simulink model "finalmodel1"  (R2024b)
(part 3 of 9)

Industry ET-P672305WB | ET Solar Industry ET-P672305WBG | ET Solar Industry ET-P672305WW | ET Solar Industry ET-P672305WWG | ET Solar Industry ET-P672310WB | ET Solar Industry ET-P672310WW | ET Solar Industry ET-P672315WB | ET Solar Industry ET-P672315WW | ET Solar Industry ET-M672320WB | ET Solar Industry ET-M672320WW | ET Solar Industry ET-P672320WB | ET Solar Industry ET-P672320WW | ET Solar Industry ET-M672325WB | ET Solar Industry ET-M672325WW | ET Solar Industry ET-P672325WB | ET Solar Industry ET-P672325WW | ET Solar Industry ET-M672330WB | ET Solar Industry ET-M672330WW | ET Solar Industry ET-P672330WB | ET Solar Industry ET-P672330WW | ET Solar Industry ET-M672335WB | ET Solar Industry ET-M672335WW | ET Solar Industry ET-P672335WB | ET Solar Industry ET-P672335WW | ET Solar Industry ET-M672340WB | ET Solar Industry ET-M672340WW | ET Solar Industry ET-M672345WB | ET Solar Industry ET-M672345WW | ET Solar Industry ET-M672350WB | ET Solar Industry ET-M672350WW | ET Solar New Energy ET-M572165WW | ET Solar New Energy ET-M572165WWZ | ET Solar New Energy ET-M572170WW | ET Solar New Energy ET-M572170WWZ | ET Solar New Energy ET-M572175BB | ET Solar New Energy ET-M572175BBZ | ET Solar New Energy ET-M572175WW | ET Solar New Energy ET-M572175WWZ | ET Solar New Energy ET-M572180BB | ET Solar New Energy ET-M572180BBZ | ET Solar New Energy ET-M572180WW | ET Solar New Energy ET-M572180WWZ | ET Solar New Energy ET-M572185BB | ET Solar New Energy ET-M572185BBZ | ET Solar New Energy ET-M572185WW | ET Solar New Energy ET-M572185WWZ | ET Solar New Energy ET-M572190BBZ | ET Solar New Energy ET-M572190WB | ET Solar New Energy ET-M572190WW | ET Solar New Energy ET-M572190WWZ | ET Solar New Energy ET-P654190WB | ET Solar New Energy ET-P654190WW | ET Solar New Energy ET-P654195WB | ET Solar New Energy ET-P654195WW | ET Solar New Energy ET-P654200WB | ET Solar New Energy ET-P654200WW | ET Solar New Energy ET-P654205WB | ET Solar New Energy ET-P654205WW | ET Solar New Energy ET-P654210WB | ET Solar New Energy ET-P654210WW | ET Solar New Energy ET-P660220WB | ET Solar New Energy ET-P660220WBZ | ET Solar New Energy ET-P660220WW | ET Solar New Energy ET-P660220WWZ | ET Solar New Energy ET-A-P660225 | ET Solar New Energy ET-A-P660225B | ET Solar New Energy ET-P660225WB | ET Solar New Energy ET-P660225WBZ | ET Solar New Energy ET-P660225WW | ET Solar New Energy ET-P660225WWZ | ET Solar New Energy ET-A-P660230 | ET Solar New Energy ET-A-P660230B | ET Solar New Energy ET-P660230B | ET Solar New Energy ET-P660230WB | ET Solar New Energy ET-P660230WBZ | ET Solar New Energy ET-P660230WW | ET Solar New Energy ET-P660230WWZ | ET Solar New Energy ET-A-M660235 | ET Solar New Energy ET-A-M660235B | ET Solar New Energy ET-A-P660235 | ET Solar New Energy ET-A-P660235B | ET Solar New Energy ET-P660235B | ET Solar New Energy ET-P660235BB | ET Solar New Energy ET-P660235BBZ | ET Solar New Energy ET-P660235WB | ET Solar New Energy ET-P660235WBZ | ET Solar New Energy ET-P660235WW | ET Solar New Energy ET-P660235WWZ | ET Solar New Energy ET-A-M660240 | ET Solar New Energy ET-A-M660240B | ET Solar New Energy ET-A-P660240 | ET Solar New Energy ET-A-P660240B | ET Solar New Energy ET-M660240BB | ET Solar New Energy ET-M660240WW | ET Solar New Energy ET-P660240B | ET Solar New Energy ET-P660240BB | ET Solar New Energy ET-P660240BBZ | ET Solar New Energy ET-P660240WB | ET Solar New Energy ET-P660240WBZ | ET Solar New Energy ET-P660240WW | ET Solar New Energy ET-P660240WWZ | ET Solar New Energy ET-A-M660245 | ET Solar New Energy ET-A-M660245B | ET Solar New Energy ET-A-P660245 | ET Solar New Energy ET-A-P660245B | ET Solar New Energy ET-M660245BB | ET Solar New Energy ET-M660245WW | ET Solar New Energy ET-P660245B | ET Solar New Energy ET-P660245BAC | ET Solar New Energy ET-P660245BB | ET Solar New Energy ET-P660245BBAC | ET Solar New Energy ET-P660245BBZ | ET Solar New Energy ET-P660245BBZAC | ET Solar New Energy ET-P660245WB | ET Solar New Energy ET-P660245WBZ | ET Solar New Energy ET-P660245WBZAC | ET Solar New Energy ET-P660245WW | ET Solar New Energy ET-P660245WWZ | ET Solar New Energy ET-A-M660250 | ET Solar New Energy ET-A-M660250B | ET Solar New Energy ET-M660250BB | ET Solar New Energy ET-M660250WW | ET Solar New Energy ET-P660250BAC | ET Solar New Energy ET-P660250BB | ET Solar New Energy ET-P660250BBAC | ET Solar New Energy ET-P660250BBZ | ET Solar New Energy ET-P660250BBZAC | ET Solar New Energy ET-P660250WB | ET Solar New Energy ET-P660250WBAC | ET Solar New Energy ET-P660250WBZ | ET Solar New Energy ET-P660250WBZAC | ET Solar New Energy ET-P660250WW | ET Solar New Energy ET-P660250WWZ | ET Solar New Energy ET-P672250 | ET Solar New Energy ET-A-M660255 | ET Solar New Energy ET-A-M660255B | ET Solar New Energy ET-M660255BB | ET Solar New Energy ET-M660255WW | ET Solar New Energy ET-P660255BB | ET Solar New Energy ET-P660255BBAC | ET Solar New Energy ET-P660255BBZ | ET Solar New Energy ET-P660255BBZAC | ET Solar New Energy ET-P660255WB | ET Solar New Energy ET-P660255WBAC | ET Solar New Energy ET-P660255WBZ | ET Solar New Energy ET-P660255WBZAC | ET Solar New Energy ET-P660255WW | ET Solar New Energy ET-P660255WWAC | ET Solar New Energy ET-P660255WWZ | ET Solar New Energy ET-P660255WWZAC | ET Solar New Energy ET-P672255 | ET Solar New Energy ET-A-M660260 | ET Solar New Energy ET-A-M660260B | ET Solar New Energy ET-M660260BB | ET Solar New Energy ET-M660260WW | ET Solar New Energy ET-P660260WB | ET Solar New Energy ET-P660260WBAC | ET Solar New Energy ET-P660260WBZ | ET Solar New Energy ET-P660260WBZAC | ET Solar New Energy ET-P660260WW | ET Solar New Energy ET-P660260WWAC | ET Solar New Energy ET-P660260WWZ | ET Solar New Energy ET-P660260WWZAC | ET Solar New Energy ET-P672260WB | ET Solar New Energy ET-P672260WW | ET Solar New Energy ET-A-M660265 | ET Solar New Energy ET-A-M660265B | ET Solar New Energy ET-M660265BB | ET Solar New Energy ET-M660265WB | ET Solar New Energy ET-M660265WW | ET Solar New Energy ET-P660265WB | ET Solar New Energy ET-P660265WW | ET Solar New Energy ET-P672265WB | ET Solar New Energy ET-P672265WW | ET Solar New Energy ET-M660270BB | ET Solar New Energy ET-M660270WB | ET Solar New Energy ET-M660270WW | ET Solar New Energy ET-P660270WB | ET Solar New Energy ET-P660270WW | ET Solar New Energy ET-P672270WB | ET Solar New Energy ET-P672270WW | ET Solar New Energy ET-A-P672275 | ET Solar New Energy ET-A-P672275B | ET Solar New Energy ET-M660275BB | ET Solar New Energy ET-M660275WB | ET Solar New Energy ET-M660275WW | ET Solar New Energy ET-P660275WB | ET Solar New Energy ET-P660275WW | ET Solar New Energy ET-P672275WB | ET Solar New Energy ET-P672275WW | ET Solar New Energy ET-A-P672280 | ET Solar New Energy ET-A-P672280B | ET Solar New Energy ET-M660280BB | ET Solar New Energy ET-M660280WB | ET Solar New Energy ET-M660280WW | ET Solar New Energy ET-P660280WB | ET Solar New Energy ET-P660280WW | ET Solar New Energy ET-P672280WB | ET Solar New Energy ET-P672280WBG | ET Solar New Energy ET-P672280WW | ET Solar New Energy ET-P672280WWG | ET Solar New Energy ET-A-M672285 | ET Solar New Energy ET-A-M672285B | ET Solar New Energy ET-A-P672285 | ET Solar New Energy ET-A-P672285B | ET Solar New Energy ET-M660285BB | ET Solar New Energy ET-M660285WB | ET Solar New Energy ET-M660285WW | ET Solar New Energy ET-P672285WB | ET Solar New Energy ET-P672285WBG | ET Solar New Energy ET-P672285WW | ET Solar New Energy ET-P672285WWG | ET Solar New Energy ET-A-M672290 | ET Solar New Energy ET-A-M672290B | ET Solar New Energy ET-A-P672290 | ET Solar New Energy ET-A-P672290B | ET Solar New Energy ET-M660290WB | ET Solar New Energy ET-M660290WW | ET Solar New Energy ET-P672290WB | ET Solar New Energy ET-P672290WBG | ET Solar New Energy ET-P672290WW | ET Solar New Energy ET-P672290WWG | ET Solar New Energy ET-A-M672295 | ET Solar New Energy ET-A-M672295B | ET Solar New Energy ET-A-P672295 | ET Solar New Energy ET-A-P672295B | ET Solar New Energy ET-P672295WB | ET Solar New Energy ET-P672295WBG | ET Solar New Energy ET-P672295WW | ET Solar New Energy ET-P672295WWG | ET Solar New Energy ET-A-M672300 | ET Solar New Energy ET-A-M672300B | ET Solar New Energy ET-P672300WB | ET Solar New Energy ET-P672300WBG | ET Solar New Energy ET-P672300WW | ET Solar New Energy ET-P672300WWG | ET Solar New Energy ET-A-M672305 | ET Solar New Energy ET-A-M672305B | ET Solar New Energy ET-P672305WB | ET Solar New Energy ET-P672305WBG | ET Solar New Energy ET-P672305WW | ET Solar New Energy ET-P672305WWG | ET Solar New Energy ET-P672310WB | ET Solar New Energy ET-P672310WW | ET Solar New Energy ET-P672315WB | ET Solar New Energy ET-P672315WW | ET Solar New Energy ET-M672320WB | ET Solar New Energy ET-M672320WW | ET Solar New Energy ET-P672320WB | ET Solar New Energy ET-P672320WW | ET Solar New Energy ET-M672325WB | ET Solar New Energy ET-M672325WW | ET Solar New Energy ET-P672325WB | ET Solar New Energy ET-P672325WW | ET Solar New Energy ET-M672330WB | ET Solar New Energy ET-M672330WW | ET Solar New Energy ET-P672330WB | ET Solar New Energy ET-P672330WW | ET Solar New Energy ET-M672335WB | ET Solar New Energy ET-M672335WW | ET Solar New Energy ET-P672335WB | ET Solar New Energy ET-P672335WW | ET Solar New Energy ET-M672340WB | ET Solar New Energy ET-M672340WW | ET Solar New Energy ET-M672345WB | ET Solar New Energy ET-M672345WW | ET Solar New Energy ET-M672350WB | ET Solar New Energy ET-M672350WW | Eterbright Solar Corp. Cigs-3050E1 | Eterbright Solar Corp. Cigs-3100A1 | Eterbright Solar Corp. Cigs-3100E1 | Eterbright Solar Corp. Cigs-3150A1 | Eterbright Solar Corp. Cigs-3150E1 | Eterbright Solar Corp. Cigs-3200A1 | Eterbright Solar Corp. Cigs-3200E1 | Eterbright Solar Corp. Cigs-3250A1 | Exeltech AM24-1-B-6-0-00 | Exiom Solution EX-175M | Exiom Solution EX-175MB | Exiom Solution EX-180M | Exiom Solution EX-180MB | Exiom Solution EX-185M | Exiom Solution EX-185MB | Exiom Solution EX-185W | Exiom Solution EX-190M | Exiom Solution EX-195M | Exiom Solution EX-220P | Exiom Solution EX-220PB | Exiom Solution EX-225P | Exiom Solution EX-225PB | Exiom Solution EX-230P | Exiom Solution EX-230PB | Exiom Solution EX-230W | Exiom Solution EX-235P | Exiom Solution EX-235PB | Exiom Solution EX-235W | Exiom Solution EX-240P | Exiom Solution EX-240PB | Exiom Solution EX-240W | Exiom Solution EX-270P | Exiom Solution EX-270PB | Exiom Solution EX-275P | Exiom Solution EX-275PB | Exiom Solution EX-280P | Exiom Solution EX-280PB | Exiom Solution EX-285P | Exiom Solution EX-285PB | Exiom Solution EX-290P | Exiom Solution EX-290PB | Fire Energy FE5A-160M | Fire Energy FE6A-160P | Fire Energy FE6A-160PE | Fire Energy FE5A-170M | Fire Energy FE6A-170P | Fire Energy FE6P-170PE | Fire Energy FE5A-180M | Fire Energy FE6A-180P | Fire Energy FE6P-180PE | Fire Energy FE5A-190M | Fire Energy FE6P-190PE | Fire Energy FE6P-200PE | Fire Energy FE6P-210P | Fire Energy FE5P-220M | Fire Energy FE6P-220P | Fire Energy FE5P-230M | Fire Energy FE6P-230P | Fire Energy FE5P-240M | First Solar FS-267 | First Solar FS-367 | First Solar FS-270 | First Solar FS-370 | First Solar FS-272 | First Solar FS-372 | First Solar FS-275 | First Solar FS-375 | First Solar FS-377 | First Solar FS-277 | First Solar FS-280 | First Solar FS-380 | First Solar FS-382 | First Solar FS-385 | First Solar FS-387 | First Solar FS-387-Plus | First Solar FS-390 | First Solar FS-390-Plus | First Solar FS-490 | First Solar FS-490A | First Solar FS-392 | First Solar FS-392-Plus | First Solar FS-492 | First Solar Fs-492A | First Solar FS-395 | First Solar FS-395-Plus | First Solar FS-495 | First Solar FS-495A | First Solar FS-397-Plus | First Solar FS-497 | First Solar FS-497A | First Solar FS-3100-Plus | First Solar FS-4100 | First Solar FS-4100-2 | First Solar FS-4100A | First Solar FS-4100A-2 | First Solar FS-4102 | First Solar FS-4102-2 | First Solar FS-4102A | First Solar FS-4102A-2 | First Solar FS-4105 | First Solar FS-4105-2 | First Solar FS-4105-3 | First Solar FS-4105A | First Solar FS-4105A-2 | First Solar FS-4105A-3 | First Solar FS-4107-2 | First Solar FS-4107-3 | First Solar FS-4107A-2 | First Solar FS-4107A-3 | First Solar FS-4110-2 | First Solar FS-4110-3 | First Solar FS-4110A-2 | First Solar FS-4110A-3 | First Solar FS-4112-2 | First Solar FS-4112-3 | First Solar FS-4112A-2 | First Solar FS-4112A-3 | First Solar FS-4115-2 | First Solar FS-4115-3 | First Solar FS-4115A-2 | First Solar FS-4115A-3 | First Solar FS-4117-2 | First Solar FS-4117-3 | First Solar FS-4117A-2 | First Solar FS-4117A-3 | First Solar FS-4120-3 | First Solar FS-4120A-3 | First Solar FS-4122-3 | First Solar FS-4122A-3 | First Solar TS-295-R11-02 | First Solar TS-295-R12-02 | First Solar TS-295-R13-02 | First Solar TS-300-R11-02 | First Solar TS-300-R12-02 | First Solar TS-300-R13-02 | First Solar TS-305-R11-02 | First Solar TS-305-R12-02 | First Solar TS-305-R13-02 | First Solar TS-310-R11-02 | First Solar TS-310-R12-02 | First Solar TS-310-R13-02 | First Solar TS-315-R11-02 | First Solar TS-315-R12-02 | First Solar TS-315-R13-02 | First Solar TS-355-R11-02 | First Solar TS-355-R12-02 | First Solar TS-355-R13-02 | First Solar TS-360-R11-02 | First Solar TS-360-R12-02 | First Solar TS-360-R13-02 | First Solar TS-365-R11-02 | First Solar TS-365-R12-02 | First Solar TS-365-R13-02 | First Solar TS-370-R11-02 | First Solar TS-370-R12-02 | First Solar TS-370-R13-02 | First Solar TS-375-R11-02 | First Solar TS-375-R12-02 | First Solar TS-375-R13-02 | Flextronics FXS-260BB-MAA1B | Flextronics FXS-260BB-MAA1W | Flextronics FLV-MA-265M60AK | Flextronics FLV-MA-265M60AW | Flextronics FLV-MA-270M60AK | Flextronics FLV-MA-270M60AW | Flextronics FXS-270BB-SAC1B | Flextronics FLV-MA-275M60AK | Flextronics FLV-MA-275M60AW | Flextronics FXS-275BB-SAC1B | Flextronics FXS-285BB-SBC1B | Flextronics FXS-285BB-SBC1W | Flextronics FLV-MA-280M60AK | Flextronics FLV-MA-280M60AW | Flextronics FLV-MA-280P60AB | Flextronics FLV-MA-280P60AK | Flextronics FLV-MA-280P60AW | Flextronics FLV-MA-285M60AK | Flextronics FLV-MA-285M60AW | Flextronics FLV-MA-285P60AB | Flextronics FLV-MA-285P60AK | Flextronics FLV-MA-285P60AW | Flextronics FLV-MA-290P60AB | Flextronics FLV-MA-290P60AK | Flextronics FLV-MA-290P60AW | Flextronics FLV-MA-295P60AB | Flextronics FLV-MA-295P60AK | Flextronics FLV-MA-295P60AW | Flextronics FLV-MA-300P60AB | Flextronics FLV-MA-320M72AK | Flextronics FLV-MA-320M72AW | Flextronics FLV-MA-325M72AK | Flextronics FLV-MA-325M72AW | Flextronics FXS-325BB-MAB1W | Flextronics FXS-325BC-MAB1W | Flextronics FLV-MA-330M72AK | Flextronics FLV-MA-330M72AW | Flextronics FLV-MA-330P72AK | Flextronics FLV-MA-330P72AW | Flextronics FXS-330BB-SAD1W | Flextronics FLV-MA-335M72AK | Flextronics FLV-MA-335M72AW | Flextronics FLV-MA-335P72AK | Flextronics FLV-MA-335P72AW | Flextronics FXS-335BB-SAD1W | Flextronics FLV-MA-340M72AK | Flextronics FLV-MA-340M72AW | Flextronics FLV-MA-340P72AK | Flextronics FLV-MA-340P72AW | Flextronics FXS-350BB-SBD1W | Flextronics FXS-350BC-SBD1W | Flextronics FLV-MA-345P72AK | Flextronics FLV-MA-345P72AW | Fluitecnik FTS210P | Fluitecnik FTS215P | Fluitecnik FTS220P | Fluitecnik FTS225P | Fluitecnik FTS230M | Fluitecnik FTS230P | Fluitecnik FTS235M | Fluitecnik FTS240M | Fluitecnik FTS245M | Fluitecnik FTS250P | Fluitecnik FTS260P | Fluitecnik FTS270P | Fluitecnik FTS280P | Foxconn International FSM185-D4C0 | Foxconn International FSM190-D4C0 | Foxconn International FSM195-D4C0 | Foxconn International FSM205-D3C0 | Foxconn International FSM210-D3C0 | Foxconn International FSM215-D3C0 | Foxconn International FSM220-D3C0 | Foxconn International FSM225-D3C0 | Foxconn International FSM230-D2C0 | Foxconn International FSM235-D2C0 | Foxconn International FSM240-D2C0 | Foxconn International FSM245-D2C0 | Foxconn International FSM250-D2C0 | Foxconn International FSM275-D1E0 | Foxconn International FSM275-D1F0 | Foxconn International FSM280-D1E0 | Foxconn International FSM280-D1F0 | Foxconn International FSM285-D1E0 | Foxconn International FSM285-D1F0 | Foxconn International FSM290-D1E0 | Foxconn International FSM290-D1F0 | Foxconn International FSM295-D1E0 | Foxconn International FSM295-D1F0 | Freevolt SW Premium 275 | Freevolt SW Premium 285 | Freevolt SW Premium 300 | Future Solar Energy FSM572165 | Future Solar Energy FSM572170 | Future Solar Energy FSM572175 | Future Solar Energy FSM572180 | Future Solar Energy FSM572185 | Future Solar Energy FSP654195 | Future Solar Energy FSP654200 | Future Solar Energy FSP654205 | Future Solar Energy FSP654210 | Future Solar Energy FSP672260 | Future Solar Energy FSP672265 | Future Solar Energy FSP672270 | Future Solar Energy FSP672275 | Future Solar Energy FSP672280 | GAF RIAC 1000 | GCL System Integration Technology Co._ Ltd. GCL-P6-36-130 | GCL System Integration Technology Co._ Ltd. GCL-P6-36-135 | GCL System Integration Technology Co._ Ltd. GCL-P6-36-140 | GCL System Integration Technology Co._ Ltd. GCL-P6-42-150 | GCL System Integration Technology Co._ Ltd. GCL-P6-42-155 | GCL System Integration Technology Co._ Ltd. GCL-P6-42-160 | GCL System Integration Technology Co._ Ltd. GCL-P6-42-165 | GCL System Integration Technology Co._ Ltd. GCL-P6-48-170 | GCL System Integration Technology Co._ Ltd. GCL-P6-48-175 | GCL System Integration Technology Co._ Ltd. GCL-M5(L)-72-180 | GCL System Integration Technology Co._ Ltd. GCL-P6-48-180 | GCL System Integration Technology Co._ Ltd. GCL-M5(L)-72-185 | GCL System Integration Technology Co._ Ltd. GCL-P6-48-185 | GCL System Integration Technology Co._ Ltd. GCL-M5(L)-72-190 | GCL System Integration Technology Co._ Ltd. GCL-P6-48-190 | GCL System Integration Technology Co._ Ltd. GCL-M5(L)-72-195 | GCL System Integration Technology Co._ Ltd. GCL-M5(L)-72-200 | GCL System Integration Technology Co._ Ltd. GCL-M6-60-200 | GCL System Integration Technology Co._ Ltd. GCL-P6-54-200 | GCL System Integration Technology Co._ Ltd. GCL-M5(L)-72-205 | GCL System Integration Technology Co._ Ltd. GCL-M6-60-205 | GCL System Integration Technology Co._ Ltd. GCL-P6-54-205 | GCL System Integration Technology Co._ Ltd. GCL-M5(L)-72-210 | GCL System Integration Technology Co._ Ltd. GCL-M6-60-210 | GCL System Integration Technology Co._ Ltd. GCL-P6-54-210 | GCL System Integration Technology Co._ Ltd. GCL-M6-60-215 | GCL System Integration Technology Co._ Ltd. GCL-P6-54-215 | GCL System Integration Technology Co._ Ltd. GCL-P6-60-215 | GCL System Integration Technology Co._ Ltd. GCL-M6-60-220 | GCL System Integration Technology Co._ Ltd. GCL-P6-54-220 | GCL System Integration Technology Co._ Ltd. GCL-P6-60-220 | GCL System Integration Technology Co._ Ltd. GCL-M6-60-225 | GCL System Integration Technology Co._ Ltd. GCL-P6-60-225 | GCL System Integration Technology Co._ Ltd. GCL-M6-60-230 | GCL System Integration Technology Co._ Ltd. GCL-P6-60-230 | GCL System Integration Technology Co._ Ltd. GCL-M6-60-235 | GCL System Integration Technology Co._ Ltd. GCL-P6-60-235 | GCL System Integration Technology Co._ Ltd. GCL-M6-60-240 | GCL System Integration Technology Co._ Ltd. GCL-P6-60-240 | GCL System Integration Technology Co._ Ltd. GCL-P6-60-245 | GCL System Integration Technology Co._ Ltd. GCL-P6-60-250 | GCL System Integration Technology Co._ Ltd. GCL-P6-72-250 | GCL System Integration Technology Co._ Ltd. GCL-P6/60255 | GCL System Integration Technology Co._ Ltd. GCL-P6-72-255 | GCL System Integration Technology Co._ Ltd. GCL-P6/60260 | GCL System Integration Technology Co._ Ltd. GCL-P6-72-260 | GCL System Integration Technology Co._ Ltd. GCL-P6/60265 | GCL System Integration Technology Co._ Ltd. GCL-P6-72-265 | GCL System Integration Technology Co._ Ltd. GCL-P6/60270 | GCL System Integration Technology Co._ Ltd. GCL-P6-72-270 | GCL System Integration Technology Co._ Ltd. GCL-M6/60275 | GCL System Integration Technology Co._ Ltd. GCL-P6/60275 | GCL System Integration Technology Co._ Ltd. GCL-P6-72-275 | GCL System Integration Technology Co._ Ltd. GCL-M6/60280 | GCL System Integration Technology Co._ Ltd. GCL-P6/60280 | GCL System Integration Technology Co._ Ltd. GCL-P6-72-280 | GCL System Integration Technology Co._ Ltd. GCL-M6/60285 | GCL System Integration Technology Co._ Ltd. GCL-P6/60285 | GCL System Integration Technology Co._ Ltd. GCL-P6-72-285 | GCL System Integration Technology Co._ Ltd. GCL-M6/60290 | GCL System Integration Technology Co._ Ltd. GCL-P6/60290 | GCL System Integration Technology Co._ Ltd. GCL-P6-72-290 | GCL System Integration Technology Co._ Ltd. GCL-M6/60295 | GCL System Integration Technology Co._ Ltd. GCL-P6-72-295 | GCL System Integration Technology Co._ Ltd. GCL-M6/60300 | GCL System Integration Technology Co._ Ltd. GCL-P6/72300 | GCL System Integration Technology Co._ Ltd. GCL-M6/60305 | GCL System Integration Technology Co._ Ltd. GCL-P6/72305 | GCL System Integration Technology Co._ Ltd. GCL-M6/60310 | GCL System Integration Technology Co._ Ltd. GCL-P6/72310 | GCL System Integration Technology Co._ Ltd. GCL-M6/60315 | GCL System Integration Technology Co._ Ltd. GCL-P6/72315 | GCL System Integration Technology Co._ Ltd. GCL-M6/60320 | GCL System Integration Technology Co._ Ltd. GCL-P6/72320 | GCL System Integration Technology Co._ Ltd. GCL-M6/72325 | GCL System Integration Technology Co._ Ltd. GCL-P6/72325 | GCL System Integration Technology Co._ Ltd. GCL-M6/72330 | GCL System Integration Technology Co._ Ltd. GCL-M6/72H330 | GCL System Integration Technology Co._ Ltd. GCL-P6/72330 | GCL System Integration Technology Co._ Ltd. GCL-P6/72H330 | GCL System Integration Technology Co._ Ltd. GCL-M6/72335 | GCL System Integration Technology Co._ Ltd. GCL-M6/72H335 | GCL System Integration Technology Co._ Ltd. GCL-P6/72335 | GCL System Integration Technology Co._ Ltd. GCL-P6/72H335 | GCL System Integration Technology Co._ Ltd. GCL-M6/72340 | GCL System Integration Technology Co._ Ltd. GCL-M6/72H340 | GCL System Integration Technology Co._ Ltd. GCL-P6/72340 | GCL System Integration Technology Co._ Ltd. GCL-P6/72H340 | GCL System Integration Technology Co._ Ltd. GCL-M6/72345 | GCL System Integration Technology Co._ Ltd. GCL-M6/72H345 | GCL System Integration Technology Co._ Ltd. GCL-P6/72345 | GCL System Integration Technology Co._ Ltd. GCL-P6/72H345 | GCL System Integration Technology Co._ Ltd. GCL-M6/72350 | GCL System Integration Technology Co._ Ltd. GCL-M6/72H350 | GCL System Integration Technology Co._ Ltd. GCL-P6/72350 | GCL System Integration Technology Co._ Ltd. GCL-P6/72H350 | GCL System Integration Technology Co._ Ltd. GCL-M6/72355 | GCL System Integration Technology Co._ Ltd. GCL-M6/72H355 | GCL System Integration Technology Co._ Ltd. GCL-P6/72355 | GCL System Integration Technology Co._ Ltd. GCL-P6/72H355 | GCL System Integration Technology Co._ Ltd. GCL-M6/72H360 | GCL System Integration Technology Co._ Ltd. GCL-P6/72H360 | GE Energy GEPVp-066-G | GE Energy GE80-NA-B | GE Energy GE85-NA-B | GE Energy GE-CIGS130 | GE Energy GE-CIGS140 | GE Energy GE-CIGS145 | GE Energy GE-CIGS150 | GE Energy GE-CIGS155 | GE Energy GEPVp-200-M | GE Energy GEPVp-205-M | General Energy Solutions 7C00-6A225 | General Energy Solutions 7C00-6A230 | General Energy Solutions 7C00-6A235 | General Energy Solutions 7E00-6A235 | General Energy Solutions 7C00-6A240 | General Energy Solutions 7E00-6A240 | General Energy Solutions 7C00-6A245 | General Energy Solutions 7E00-6A245 | General Energy Solutions 7E00-6A250 | General Energy Solutions BVM6610P-250 | General Energy Solutions 7E00-6A255 | General Energy Solutions BVM6610P-255 | General Energy Solutions 7E00-6A260 | General Energy Solutions BVM6610M-260 | General Energy Solutions BVM6610P-260 | General Energy Solutions 7E00-6A265 | General Energy Solutions BVM6610M-265 | General Energy Solutions BVM6610P-265 | General Energy Solutions BVM6610M-270 | General Energy Solutions BVM6610P-270 | General Energy Solutions 7C00-6C275 | General Energy Solutions BVM6610M-275 | General Energy Solutions 7C00-6C280 | General Energy Solutions BVM6610M-280 | General Energy Solutions 7C00-6C285 | General Energy Solutions 7E00-6C285 | General Energy Solutions 7C00-6C290 | General Energy Solutions 7E00-6C290 | General Energy Solutions 7C00-6C295 | General Energy Solutions 7E00-6C295 | General Energy Solutions 7C00-6C300 | General Energy Solutions 7E00-6C300 | General Energy Solutions BVM6612P-300 | General Energy Solutions 7C00-6C305 | General Energy Solutions 7E00-6C305 | General Energy Solutions BVM6612P-305 | General Energy Solutions 7C00-6C310 | General Energy Solutions 7E00-6C310 | General Energy Solutions BVM6612M-310 | General Energy Solutions BVM6612P-310 | General Energy Solutions 7E00-6C315 | General Energy Solutions BVM6612M-315 | General Energy Solutions BVM6612P-315 | General Energy Solutions BVM6612M-320 | General Energy Solutions BVM6612P-320 | General Energy Solutions BVM6612M-325 | General Energy Solutions BVM6612P-325 | General Energy Solutions BVM6612M-330 | General Energy Solutions BVM6612M-335 | General Solar Power (Yantai) GSC90UR33Y | General Solar Power (Yantai) GSC93UR33Y | General Solar Power (Yantai) GSB94UR33 | General Solar Power (Yantai) GSB97UR33 | General Solar Power (Yantai) GSB100UR33 | GermanSolar USA GSP6-60-245W | GermanSolar USA GSP6-60-250W | GermanSolar USA GSP6-60-255W | GermanSolar USA GSM6-60-260W | GermanSolar USA GSP6-60-260W | GermanSolar USA GSM6-60-265W | GermanSolar USA GSP6-60-265W | GermanSolar USA GSM6-60-270W | GermanSolar USA GSP6-60-270W | GermanSolar USA GSM6-60-275W | GermanSolar USA GSM6-60-280W | GermanSolar USA GSM6-60-285W | GermanSolar USA GSM6-60-290W | GermanSolar USA GSM6-60-295W | GermanSolar USA GSM6-60-300W | GermanSolar USA GSP6-72-300W | GermanSolar USA GSP6-72-305W | GermanSolar USA GSM6-72-310W | GermanSolar USA GSP6-72-310W | GermanSolar USA GSM6-72-315W | GermanSolar USA GSP6-72-315W | GermanSolar USA GSM6-72-320W | GermanSolar USA GSP6-72-320W | GermanSolar USA GSM6-72-325W | GermanSolar USA GSP6-72-325W | GermanSolar USA GSM6-72-330W | GermanSolar USA GSM6-72-335W | GESOLAR GES-M165 | GESOLAR GES-M170 | GESOLAR GES-M175 | GESOLAR GES-M180 | GESOLAR GES-P200 | GESOLAR GES-P210 | GESOLAR GES-P220 | GESOLAR GES-P230 | GESOLAR GES-P250 | GESOLAR GES-P260 | GESOLAR GES-P270 | GESOLAR GES-P280 | Gigawatt GW250PB | Gigawatt GW255PB | Gigawatt GW260PB | Gigawatt GW265PB | Gigawatt GW270MB | Gigawatt GW270MB-M2 | Gigawatt GW270PB | Gigawatt GW275MB | Gigawatt GW275MB-M2 | Gigawatt GW-275MB-USA | Gigawatt GW275PB | Gigawatt GW280MB | Gigawatt GW280MB-M2 | Gigawatt GW-280MB-USA | Gigawatt GW280PB | Gigawatt GW285MB | Gigawatt GW285MB-M2 | Gigawatt GW-285MB-USA | Gigawatt GW290MB | Gigawatt GW290MB-M2 | Gigawatt GW-290MB-USA | Gigawatt GW295MB | Gigawatt GW295MB-M2 | Gigawatt GW-295MB-USA | Gigawatt GW-300MB-USA | Gintech Energy GIN P6-48-200 | Gintech Energy GTE 200M | Gintech Energy GIN P6-48-205 | Gintech Energy GTE 205M | Gintech Energy GIN M6-48-210 | Gintech Energy GIN P6-48-210 | Gintech Energy GTE 210M | Gintech Energy GIN M6-48-215 | Gintech Energy GIN P6-48-215 | Gintech Energy GTE 215M | Gintech Energy GIN M6-48-220 | Gintech Energy GIN P6-48-220 | Gintech Energy GTE 220M | Gintech Energy GIN M6-48-225 | Gintech Energy GTE 225M | Gintech Energy GIN M6-48-230 | Gintech Energy GTE 230M | Gintech Energy GTE 235M | Gintech Energy GTE 240M | Gintech Energy GIN P6-60-250 | Gintech Energy GIN P6-60-255 | Gintech Energy GIN P6-60-260 | Gintech Energy GIN M6-60-265 | Gintech Energy GIN P6-60-265 | Gintech Energy GIN M6-60-270 | Gintech Energy GIN P6-60-270 | Gintech Energy GIN M6-60-275 | Gintech Energy GIN M6-60-280 | Gintech Energy GIN M6-60-285 | Gintech Energy GIN P6-72-290 | Gintech Energy GIN P6-72-295 | Gintech Energy GIN P6-72-300 | Gintech Energy GIN M6-72-305 | Gintech Energy GIN P6-72-305 | Gintech Energy GIN P6F-72-305 | Gintech Energy GIN M6-72-310 | Gintech Energy GIN P6-72-310 | Gintech Energy GIN P6F-72-310 | Gintech Energy GIN M6-72-315 | Gintech Energy GIN P6-72-315 | Gintech Energy GIN P6F-72-315 | Gintech Energy GIN M6-72-320 | Gintech Energy GIN P6-72-320 | Gintech Energy GIN P6F-72-320 | Gintech Energy GIN M6-72-325 | Gintech Energy GIN P6F-72-325 | Gintech Energy GIN M6-72-330 | Gintech Energy GIN P6F-72-330 | Gintech Energy GIN M6-72-335 | Gintung Energy ASEC-120G6M | Gintung Energy ASEC-125G6M | Gintung Energy ASEC-125G6S | Gintung Energy ASEC-130G6M | Gintung Energy ASEC-130G6S | Gintung Energy ASEC-135G6M | Gintung Energy ASEC-135G6S | Gintung Energy ASEC-140G6M | Gintung Energy ASEC-140G6S | Gintung Energy ASEC-145G6M49 | Gintung Energy ASEC-145G6S49 | Gintung Energy ASEC-150G6M49 | Gintung Energy ASEC-150G6S49 | Gintung Energy ASEC-155G6M49 | Gintung Energy ASEC-155G6S49 | Gintung Energy ASEC-175G6M | Gintung Energy ASEC-175G6S | Gintung Energy ASEC-180G6M | Gintung Energy ASEC-180G6S | Gintung Energy ASEC-185G6M | Gintung Energy ASEC-185G6S | Gintung Energy ASEC-190G6M | Gintung Energy ASEC-190G6M68 | Gintung Energy ASEC-190G6S | Gintung Energy ASEC-190G6S68 | Gintung Energy GTEC-190G6M68 | Gintung Energy GTEC-190G6S68 | Gintung Energy ASEC-195G6M | Gintung Energy ASEC-195G6M68 | Gintung Energy ASEC-195G6S | Gintung Energy ASEC-195G6S68 | Gintung Energy GTEC-195G6M68 | Gintung Energy GTEC-195G6S68 | Gintung Energy ASEC-200G6M | Gintung Energy ASEC-200G6M68 | Gintung Energy ASEC-200G6S | Gintung Energy ASEC-200G6S68 | Gintung Energy GTEC-200G6M68 | Gintung Energy GTEC-200G6S68 | Gintung Energy ASEC-205G6M | Gintung Energy ASEC-205G6M68 | Gintung Energy ASEC-205G6S | Gintung Energy ASEC-205G6S68 | Gintung Energy GTEC-205G6M68 | Gintung Energy GTEC-205G6S68 | Gintung Energy ASEC-210G6M | Gintung Energy ASEC-210G6M68 | Gintung Energy ASEC-210G6S | Gintung Energy ASEC-210G6S68 | Gintung Energy GTEC-210G6M68 | Gintung Energy GTEC-210G6S68 | Gintung Energy ASEC-215G6M | Gintung Energy ASEC-215G6M68 | Gintung Energy ASEC-215G6M69 | Gintung Energy ASEC-215G6S | Gintung Energy ASEC-215G6S68 | Gintung Energy ASEC-215G6S69 | Gintung Energy GTEC-215G6M68 | Gintung Energy GTEC-215G6M69 | Gintung Energy GTEC-215G6S68 | Gintung Energy GTEC-215G6S69 | Gintung Energy ASEC-220G6M | Gintung Energy ASEC-220G6M68 | Gintung Energy ASEC-220G6M69 | Gintung Energy ASEC-220G6S | Gintung Energy ASEC-220G6S68 | Gintung Energy ASEC-220G6S69 | Gintung Energy GTEC-220G6M68 | Gintung Energy GTEC-220G6M69 | Gintung Energy GTEC-220G6S68 | Gintung Energy GTEC-220G6S69 | Gintung Energy ASEC-225G6M | Gintung Energy ASEC-225G6M69 | Gintung Energy ASEC-225G6S | Gintung Energy ASEC-225G6S69 | Gintung Energy GTEC-225G6M69 | Gintung Energy GTEC-225G6S69 | Gintung Energy ASEC-230G6M | Gintung Energy ASEC-230G6M69 | Gintung Energy ASEC-230G6S | Gintung Energy ASEC-230G6S69 | Gintung Energy GTEC-230G6M69 | Gintung Energy GTEC-230G6S69 | Gintung Energy ASEC-235G6M | Gintung Energy ASEC-235G6M69 | Gintung Energy ASEC-235G6S | Gintung Energy ASEC-235G6S69 | Gintung Energy GTEC-235G6M69 | Gintung Energy GTEC-235G6S69 | Gintung Energy ASEC-240G6M69 | Gintung Energy ASEC-240G6M6A | Gintung Energy ASEC-240G6S69 | Gintung Energy ASEC-240G6S6A | Gintung Energy GTEC-240G6M69 | Gintung Energy GTEC-240G6M6A | Gintung Energy GTEC-240G6S69 | Gintung Energy GTEC-240G6S6A | Gintung Energy ASEC-245G6M | Gintung Energy ASEC-245G6M69 | Gintung Energy ASEC-245G6M6A | Gintung Energy ASEC-245G6S69 | Gintung Energy ASEC-245G6S6A | Gintung Energy GTEC-245G6M69 | Gintung Energy GTEC-245G6M6A | Gintung Energy GTEC-245G6S69 | Gintung Energy GTEC-245G6S6A | Gintung Energy ASEC-250G6M | Gintung Energy ASEC-250G6M6A | Gintung Energy ASEC-250G6M6B | Gintung Energy ASEC-250G6S6A | Gintung Energy ASEC-250G6S6B | Gintung Energy GTEC-250G6M6A | Gintung Energy GTEC-250G6S6A | Gintung Energy ASEC-255G6M | Gintung Energy ASEC-255G6M6A | Gintung Energy ASEC-255G6M6B | Gintung Energy ASEC-255G6S | Gintung Energy ASEC-255G6S6A | Gintung Energy ASEC-255G6S6B | Gintung Energy GTEC-255G6M6A | Gintung Energy GTEC-255G6S6A | Gintung Energy ASEC-260G6M | Gintung Energy ASEC-260G6M6A | Gintung Energy ASEC-260G6M6B | Gintung Energy ASEC-260G6S | Gintung Energy ASEC-260G6S6A | Gintung Energy ASEC-260G6S6B | Gintung Energy GTEC-260G6M6A | Gintung Energy GTEC-260G6M6B | Gintung Energy GTEC-260G6S6A | Gintung Energy GTEC-260G6S6B | Gintung Energy ASEC-265G6M | Gintung Energy ASEC-265G6M6A | Gintung Energy ASEC-265G6M6B | Gintung Energy ASEC-265G6S | Gintung Energy ASEC-265G6S6A | Gintung Energy ASEC-265G6S6B | Gintung Energy GTEC-265G6M6A | Gintung Energy GTEC-265G6M6B | Gintung Energy GTEC-265G6S6A | Gintung Energy GTEC-265G6S6B | Gintung Energy ASEC-270G6M | Gintung Energy ASEC-270G6M6A | Gintung Energy ASEC-270G6M6B | Gintung Energy ASEC-270G6S | Gintung Energy ASEC-270G6S6A | Gintung Energy ASEC-270G6S6B | Gintung Energy GTEC-270G6M6A | Gintung Energy GTEC-270G6M6B | Gintung Energy GTEC-270G6S6A | Gintung Energy GTEC-270G6S6B | Gintung Energy ASEC-275G6M | Gintung Energy ASEC-275G6M6B | Gintung Energy ASEC-275G6S | Gintung Energy ASEC-275G6S6B | Gintung Energy GTEC-275G6M6B | Gintung Energy GTEC-275G6S6B | Gintung Energy ASEC-280G6M | Gintung Energy ASEC-280G6M6B | Gintung Energy ASEC-280G6S | Gintung Energy ASEC-280G6S6B | Gintung Energy GTEC-280G6M | Gintung Energy GTEC-280G6M6B | Gintung Energy GTEC-280G6S | Gintung Energy GTEC-280G6S6B | Gintung Energy ASEC-285G6M | Gintung Energy ASEC-285G6M6B | Gintung Energy ASEC-285G6S | Gintung Energy ASEC-285G6S6B | Gintung Energy GTEC-285G6M | Gintung Energy GTEC-285G6M6B | Gintung Energy GTEC-285G6S | Gintung Energy GTEC-285G6S6B | Gintung Energy ASEC-290G6M | Gintung Energy ASEC-290G6M6B | Gintung Energy ASEC-290G6S | Gintung Energy ASEC-290G6S6B | Gintung Energy GTEC-290G6M | Gintung Energy GTEC-290G6M6B | Gintung Energy GTEC-290G6S | Gintung Energy GTEC-290G6S6B | Gintung Energy ASEC-295G6M | Gintung Energy ASEC-295G6M6B | Gintung Energy ASEC-295G6S | Gintung Energy ASEC-295G6S6B | Gintung Energy GTEC-295G6M | Gintung Energy GTEC-295G6M6B | Gintung Energy GTEC-295G6S | Gintung Energy GTEC-295G6S6B | Gintung Energy ASEC-300G6M | Gintung Energy ASEC-300G6S | Gintung Energy GTEC-300G6M | Gintung Energy GTEC-300G6S | Gintung Energy ASEC-305G6M | Gintung Energy ASEC-305G6S | Gintung Energy GTEC-305G6M | Gintung Energy GTEC-305G6S | Gintung Energy ASEC-310G6M | Gintung Energy ASEC-310G6S | Gintung Energy GTEC-310G6M | Gintung Energy GTEC-310G6S | Gintung Energy ASEC-315G6M | Gintung Energy ASEC-315G6S | Gintung Energy GTEC-315G6M | Gintung Energy GTEC-315G6S | Gintung Energy ASEC-320G6M | Gintung Energy ASEC-320G6S | Gintung Energy GTEC-320G6M | Gintung Energy GTEC-320G6S | Gintung Energy ASEC-325G6M | Gintung Energy ASEC-325G6S | Gintung Energy GTEC-325G6M | Gintung Energy GTEC-325G6S | Global Solar Energy FG-2BTM-82 | Global Solar Energy FG-2BTN-82 | Global Solar Energy FG-2BTM-90 | Global Solar Energy FG-2BTN-90 | Global Solar Energy FG-2BTM-100 | Global Solar Energy FG-2BTN-100 | Global Solar Energy FG-4BTM-185 | Global Solar Energy FG-4BTN-185 | Global Solar Energy FG-1BTM-225 | Global Solar Energy FG-1BTN-225 | Global Solar Energy FG-1BTM-250 | Global Solar Energy FG-1BTN-250 | Global Solar Energy FG-1BTM-275 | Global Solar Energy FG-1BTN-275 | Global Solar Energy FG-1BTM-300 | Global Solar Energy FG-1BTN-300 | Global Sun P-220GS | Global Sun P-225GS | Global Sun P-230GS | Global Sun P-235GS | Global Sun P-240GS | Gloria Solar GSS5-160A-E1 | Gloria Solar GSS5-165A-E1 | Gloria Solar GSS5-170A-E1 | Gloria Solar GSS5-175A-E1 | Gloria Solar GSS5-180A-E1 | Gloria Solar GSM6-200D-E1 | Gloria Solar GSM6-205D-E1 | Gloria Solar GSM6-210D-E1 | Gloria Solar GSM6-215D-E1 | Gloria Solar GSM6-220D-E1 | Gloria Solar GSM6-225D-E1 | Gloria Solar GSM6-230D-E1 | Gloria Solar GSM6-235D-E1 | Gloria Solar GSM6-240D-E1 | Grape Solar GS-P-120-PDX | Grape Solar GS-P-125-PDX | Grape Solar GS-P-130-PDX | Grape Solar GS-P-135-PDX | Grape Solar GS-P-140-PDX | Grape Solar GS-S-150-SF | Grape Solar GS-S-155-SF | Grape Solar GS-P-160-EUG | Grape Solar GS-S-160-Fab8 | Grape Solar GS-S-160-SF | Grape Solar CS-S-165-DJ | Grape Solar GS-P-165-EUG | Grape Solar GS-S-165-Fab8 | Grape Solar GS-S-165-SF | Grape Solar CS-S-170-DJ | Grape Solar GS-P-170-EUG | Grape Solar GS-S-170-Fab3 | Grape Solar GS-S-170-SF | Grape Solar GS-S-175-Fab8 | Grape Solar CS-S-175-DJ | Grape Solar GS-P-175-EUG | Grape Solar GS-S-175-EUG | Grape Solar GS-S-175-Fab3 | Grape Solar GS-S-175-SF | Grape Solar CS-S-180-DJ | Grape Solar GS-P-180-EUG | Grape Solar GS-S-180-EUG | Grape Solar GS-S-180-Fab3 | Grape Solar GS-S-180-Fab8 | Grape Solar GS-S-180-SF | Grape Solar GS-S-185-Fab3 | Grape Solar GS-S-185-Fab8 | Grape Solar GS-S-185-SF | Grape Solar GS-P-190-EUG | Grape Solar GS-S-190-Fab3 | Grape Solar GS-P-190-SL6-18 | Grape Solar GS-P-195-EUG | Grape Solar GS-S-195-Fab3 | Grape Solar CS-P-200-DJ | Grape Solar GS-P-200-CSPE | Grape Solar GS-P-200-EUG | Grape Solar GS-P-200-Fab1 | Grape Solar GS-P-200-OR | Grape Solar GS-P-200-PDX | Grape Solar GS-P-200-SL6-18 | Grape Solar GS-S-200-Fab1 | Grape Solar GS-P-205-EUG | Grape Solar GS-P-205-Fab1 | Grape Solar GS-P-205-OR | Grape Solar GS-P-205-PDX | Grape Solar GS-P-205-SL6-18 | Grape Solar GS-S-205-Fab1 | Grape Solar CS-P-210-DJ | Grape Solar GS-P-210-Fab1 | Grape Solar GS-P-210-Fab5 | Grape Solar GS-P-210-OR | Grape Solar GS-P-210-PDX | Grape Solar GS-S-210-Fab1 | Grape Solar GS-P-215-Fab1 | Grape Solar GS-P-215-Fab5 | Grape Solar GS-P-215-OR | Grape Solar GS-P-215-PDX | Grape Solar GS-S-215-Fab1 | Grape Solar CS-P-220-DJ | Grape Solar GS-P-220-CS | Grape Solar GS-P-220-EUG | Grape Solar GS-P-220-Fab1 | Grape Solar GS-P-220-Fab5 | Grape Solar GS-P-220-OR | Grape Solar GS-P-220-PDX | Grape Solar GS-P-220-SL6-20 | Grape Solar GS-S-220-CS | Grape Solar GS-S-220-Fab1 | Grape Solar GS-S-220-Fab3 | Grape Solar GS-S-220-Fab8 | Grape Solar GS-P-225-EUG | Grape Solar GS-P-225-Fab1 | Grape Solar GS-P-225-Fab5 | Grape Solar GS-P-225-PDX | Grape Solar GS-P-225-SL6-20 | Grape Solar GS-S-225-Fab1 | Grape Solar GS-S-225-Fab3 | Grape Solar GS-S-225-Fab8 | Grape Solar CS-P-230-DJ | Grape Solar GS-P-230-CS | Grape Solar GS-P-230-EUG | Grape Solar GS-P-230-Fab1 | Grape Solar GS-P-230-Fab5 | Grape Solar GS-P-230-PDX | Grape Solar GS-P-230-SL6-20 | Grape Solar GS-S-230-CS | Grape Solar GS-S-230-Fab1 | Grape Solar GS-S-230-Fab3 | Grape Solar GS-S-230-Fab8 | Grape Solar GS-P-235-Fab1 | Grape Solar GS-P-235-Fab5 | Grape Solar GS-P-235-PDX | Grape Solar GS-S-235-Fab1 | Grape Solar GS-S-235-Fab3 | Grape Solar GS-S-235-Fab8 | Grape Solar GS-P-240-Fab1 | Grape Solar GS-P-240-KR2 | Grape Solar GS-P-240-KR2K | Grape Solar GS-P-240-PDX | Grape Solar GS-S-240-CS | Grape Solar GS-S-240-Fab1 | Grape Solar GS-S-240-Fab3 | Grape Solar GS-S-240-Fab8 | Grape Solar GS-P-245-Fab1 | Grape Solar GS-P-245-KR2 | Grape Solar GS-P-245-KR2K | Grape Solar GS-P-245-PDX | Grape Solar GS-S-245-Fab3 | Grape Solar GS-S-245-Fab8 | Grape Solar CS-P-250-DJ | Grape Solar GS-P-250-EUG | Grape Solar GS-P-250-Fab1 | Grape Solar GS-P-250-KR2 | Grape Solar GS-P-250-KR2K | Grape Solar GS-P-250-PDX | Grape Solar GS-S-250-Fab3 | Grape Solar GS-S-250-Fab5 | Grape Solar GS-S-250-Fab8 | Grape Solar GS-S-250-KR1 | Grape Solar GS-S-250-KR1K | Grape Solar GS-S-250-KR3 | Grape Solar GS-S-250-KR3K | Grape Solar GS-P-255-EUG | Grape Solar GS-P-255-Fab1 | Grape Solar GS-P-255-PDX | Grape Solar GS-P60-255-Fab2 | Grape Solar GS-S-255-Fab3 | Grape Solar GS-S-255-Fab5 | Grape Solar GS-S-255-KR1 | Grape Solar GS-S-255-KR1K | Grape Solar GS-S-255-KR3 | Grape Solar GS-S-255-KR3K | Grape Solar CS-P-260-DJ | Grape Solar GS-P-260-EUG | Grape Solar GS-P-260-Fab1 | Grape Solar GS-P-260-PDX | Grape Solar GS-P60-260-Fab2 | Grape Solar GS-P72-260-Fab2 | Grape Solar GS-S-260-Fab1 | Grape Solar GS-S-260-Fab5 | Grape Solar GS-S-260-KR1 | Grape Solar GS-S-260-KR1K | Grape Solar GS-S-260-KR3 | Grape Solar GS-S-260-KR3K | Grape Solar GS-S60-260-SI | Grape Solar GS-P-265-Fab1 | Grape Solar GS-P-265-PDX | Grape Solar GS-P60-265-Fab2 | Grape Solar GS-P72-265-Fab2 | Grape Solar GS-S-265-Fab1 | Grape Solar GS-S-265-Fab5 | Grape Solar GS-S60-265-SI | Grape Solar CS-P-270-DJ | Grape Solar GS-P-270-EUG | Grape Solar GS-P-270-Fab1 | Grape Solar GS-P-270-PDX | Grape Solar GS-P60-270-Fab2 | Grape Solar GS-P72-270-Fab2 | Grape Solar GS-S-270-Fab1 | Grape Solar GS-S-270-Fab5 | Grape Solar GS-S60-270-SI | Grape Solar GS-P-275-EUG | Grape Solar GS-P-275-Fab1 | Grape Solar GS-P-275-PDX | Grape Solar GS-P60-275-Fab2 | Grape Solar GS-P72-275-Fab2 | Grape Solar GS-S-275-Fab1 | Grape Solar GS-S-275-Fab5 | Grape Solar GS-S60-275-SI | Grape Solar CS-P-280-DJ | Grape Solar GS-P-280-EUG | Grape Solar GS-P-280-Fab1 | Grape Solar GS-P-280-PDX | Grape Solar GS-P72-280-Fab2 | Grape Solar GS-S-280-Fab1 | Grape Solar GS-S-280-Fab5 | Grape Solar GS-S60-280-SI | Grape Solar GS-M60-285-Fab1-USA | Grape Solar GS-P-285-Fab1 | Grape Solar GS-P-285-FAB36 | Grape Solar GS-P-285-PDX | Grape Solar GS-P72-285-Fab2 | Grape Solar GS-S-285-Fab1 | Grape Solar GS-S60LSQ-285-PR | Grape Solar GS-M60-290-Fab1-USA | Grape Solar GS-P-290-Fab1 | Grape Solar GS-P-290-FAB36 | Grape Solar GS-P72-290-Fab2 | Grape Solar GS-S-290-Fab1 | Grape Solar GS-S-290-FAB36 | Grape Solar GS-M60-295-Fab1-USA | Grape Solar GS-P-295-Fab1 | Grape Solar GS-P-295-FAB36 | Grape Solar GS-P72-295-Fab2 | Grape Solar GS-S-295-Fab1 | Grape Solar GS-S-295-FAB36 | Grape Solar GS-M60-300-Fab1-USA | Grape Solar GS-P-300-FAB36 | Grape Solar GS-P72-300-Fab2 | Grape Solar GS-S-300-FAB36 | Grape Solar GS-S-300-KR1 | Grape Solar GS-S-300-KR1K | Grape Solar GS-P72-305-Fab2 | Grape Solar GS-S-305-FAB36 | Grape Solar GS-S-305-KR1 | Grape Solar GS-S-305-KR1K | Grape Solar GS-S72-305-SI | Grape Solar GS-P72-310-Fab2 | Grape Solar GS-S-310-FAB36 | Grape Solar GS-S-310-KR1 | Grape Solar GS-S-310-KR1K | Grape Solar GS-S72-310-SI | Grape Solar GS-P72-315-Fab2 | Grape Solar GS-S72-315-SI | Grape Solar GS-P72-320-Fab2 | Grape Solar GS-S72-320-SI | Grape Solar GS-P72-325-Fab2 | Grape Solar GS-S72-325-SI | Grape Solar GS-P72-330-Fab2 | Grape Solar GS-S72-330-SI | Grape Solar GS-S72-335-SI | Grape Solar GS-M72-340-Fab1-USA | Grape Solar GS-M72-345-Fab1-USA | Grape Solar GS-M72-350-Fab1-USA | Grape Solar GS-M72-355-Fab1-USA | Grape Solar GS-M72-360-Fab1-USA | Grape Solar GS-P-375-KR2 | Grape Solar GS-P-380-KR2 | Grape Solar GS-P-385-KR2 | Grape Solar GS-S-385-TS | Grape Solar GS-P-390-KR2 | Grape Solar GS-S-390-TS | Grape Solar GS-P-395-KR2 | Grape Solar GS-S-395-Platinum | Grape Solar GS-S-400-Platinum | Grape Solar GS-S-405-KR1 | Grape Solar GS-S-405-KR3 | Grape Solar GS-S-405-Platinum | Grape Solar GS-S-410-KR1 | Grape Solar GS-S-410-KR3 | Grape Solar GS-S-410-Platinum | Grape Solar GS-S-415-KR1 | Grape Solar GS-S-415-KR3 | Grape Solar GS-S-420-KR1 | Grape Solar GS-S-420-KR3 | Green Energy Solar & Wind GESW1750 USA-170W | Green Energy Solar & Wind GESW1750 USA-175W | Green Energy Solar & Wind GESW1750 USA-180W | Green Energy Solar & Wind GESW2100 USA-210W | Green Energy Solar & Wind GESW2100 USA-215W | Green Energy Solar & Wind GESW2100 USA-220W | Green Energy Technology GET-085A | Green Energy Technology GET-090A | Green Energy Technology GET-095A-1 | Green Energy Technology GET-095-AT | Green Energy Technology GET-100A-1 | Green Energy Technology GET-100-AT | Green Energy Technology GET-105-AT | Green Energy Technology GET-170A | Green Energy Technology GET-170B | Green Energy Technology GET-180A | Green Energy Technology GET-180B | Green Energy Technology GET-340A | Green Energy Technology GET-360A | Green Power ET-M572165 | Green Power ET-M572170 | Green Power ET-M572175 | Green Power ET-M572175B | Green Power ET-M572180 | Green Power ET-M572180B | Green Power ET-M572185 | Green Power ET-M572185B | Green Power ET-P654190B | Green Power ET-P654195 | Green Power ET-P654195B | Green Power ET-P654200 | Green Power ET-P654200B | Green Power ET-P654205 | Green Power ET-P654205B | Green Power ET-P654210 | Green Power ET-P654210B | Green Power ET-P660220 | Green Power ET-P660220B | Green Power ET-P660225 | Green Power ET-P660225B | Green Power ET-P660230 | Green Power ET-P660230B | Green Power ET-P660235 | Green Power ET-P660235B | Green Power ET-P672260 | Green Power ET-P672260B | Green Power ET-P672265 | Green Power ET-P672265B | Green Power ET-P672270 | Green Power ET-P672270B | Green Power ET-P672275 | Green Power ET-P672275B | Green Power ET-P672280 | Green Power ET-P672280B | Greenbrilliance Energy GB54P6-200 | Greenbrilliance Energy GB60P6-210 | Greenbrilliance Energy GB60P6-215 | Greenbrilliance Energy GB60P6-220 | Greenbrilliance Energy GB60P6-225 | Greenbrilliance Energy GB60P6-230 | Greenbrilliance Energy GB72P6-270 | Greenbrilliance Energy GB72P6-275 | Greenbrilliance Energy GB72P6-280 | Greenlite Solar Canada GLS-200 | Greenlite Solar Canada GLS-220 | Greenlite Solar Canada GLS-270 | GS-Solar (Fujian) GS-46SU | GS-Solar (Fujian) GS-58 | GS-Solar (Fujian) GS-60 | GS-Solar (Fujian) GS-63 | Guangdong Fivestar Solar Energy FS-M125-175W | Guangdong Fivestar Solar Energy FS-P156-210W | Guangdong Fivestar Solar Energy FS-P156-220W | Guangdong Golden Glass Technologies GG160M2-24/1324x992 | Guangdong Golden Glass Technologies GG165M2-24/1324x992 | Guangdong Golden Glass Technologies GG170M2-24/1324x992 | Guangdong Golden Glass Technologies GG175M2-24/1324x992 | Guangdong Golden Glass Technologies GG175S1-36/1589x807 | Guangdong Golden Glass Technologies GG180M2-24/1324x992 | Guangdong Golden Glass Technologies GG180S1-36/1589x807 | Guangdong Golden Glass Technologies GG190M2-27/1482x992 | Guangdong Golden Glass Technologies GG195M2-27/1482x992 | Guangdong Golden Glass Technologies GG200M2-27/1482x992 | Guangdong Golden Glass Technologies GG205M2-27/1482x992 | Guangdong Golden Glass Technologies GG220M2-30/1640x992 | Guangdong Golden Glass Technologies GG225M2-30/1640x992 | Guangdong Golden Glass Technologies GG230M2-30/1640x992 | Guangdong Golden Glass Technologies GG250M2-35/1956x992 | Guangdong Golden Glass Technologies GG255M2-35/1956x992 | Guangdong Golden Glass Technologies GG260M2-35/1956x992 | Guangdong Golden Glass Technologies GG270M2-36/1956x992 | Guangdong Golden Glass Technologies GG275M2-36/1956x992 | Guangdong Golden Glass Technologies GG280M2-36/1956x992 | Guodian Jintech Solar Energy JT5M-175/E | Guodian Jintech Solar Energy JT5M-180/E | Guodian Jintech Solar Energy JT5M-185/E | Guodian Jintech Solar Energy JT6P-215/D | Guodian Jintech Solar Energy JT6P-220/D | Guodian Jintech Solar Energy JT6P-225/D | Guodian Jintech Solar Energy JT6P-230/D | Guodian Jintech Solar Energy JT6P-235/D | Guodian Jintech Solar Energy JT6P-255/E | Guodian Jintech Solar Energy JT6P-260/E | Guodian Jintech Solar Energy JT6P-265/E | Guodian Jintech Solar Energy JT6P-270/E | Guodian Jintech Solar Energy JT6P-275/E | Guodian Jintech Solar Energy JT6P-280/E | Hangzhou AmpleSun Solar Technology ASF100 | Hangzhou Zhejiang University Sunny Energy Science & Technology ZDNY-180C | Hangzhou Zhejiang University Sunny Energy Science & Technology ZDNY-185C | Hangzhou Zhejiang University Sunny Energy Science & Technology ZDNY-190C | Hangzhou Zhejiang University Sunny Energy Science & Technology ZDNY-200P54 | Hangzhou Zhejiang University Sunny Energy Science & Technology ZDNY-210C54 | Hangzhou Zhejiang University Sunny Energy Science & Technology ZDNY-210P54 | Hangzhou Zhejiang University Sunny Energy Science & Technology ZDNY-220C54 | Hangzhou Zhejiang University Sunny Energy Science & Technology ZDNY-220P54 | Hangzhou Zhejiang University Sunny Energy Science & Technology ZDNY-220P60 | Hangzhou Zhejiang University Sunny Energy Science & Technology ZDNY-230C54 | Hangzhou Zhejiang University Sunny Energy Science & Technology ZDNY-230C60 | Hangzhou Zhejiang University Sunny Energy Science & Technology ZDNY-230P60 | Hangzhou Zhejiang University Sunny Energy Science & Technology ZDNY-240C60 | Hangzhou Zhejiang University Sunny Energy Science & Technology ZDNY-240P60 | Hangzhou Zhejiang University Sunny Energy Science & Technology ZDNY-245P60 | Hangzhou Zhejiang University Sunny Energy Science & Technology ZDNY-250C60 | Hangzhou Zhejiang University Sunny Energy Science & Technology ZDNY-250P60 | Hangzhou Zhejiang University Sunny Energy Science & Technology ZDNY-255C60 | Hangzhou Zhejiang University Sunny Energy Science & Technology ZDNY-255P60 | Hangzhou Zhejiang University Sunny Energy Science & Technology ZDNY-260C60 | Hangzhou Zhejiang University Sunny Energy Science & Technology ZDNY-260P60 | Hangzhou Zhejiang University Sunny Energy Science & Technology ZDNY-265C60 | Hangzhou Zhejiang University Sunny Energy Science & Technology ZDNY-265P60 | Hangzhou Zhejiang University Sunny Energy Science & Technology ZDNY-270C60 | Hangzhou Zhejiang University Sunny Energy Science & Technology ZDNY-270P72 | Hangzhou Zhejiang University Sunny Energy Science & Technology ZDNY-275C60 | Hangzhou Zhejiang University Sunny Energy Science & Technology ZDNY-280C72 | Hangzhou Zhejiang University Sunny Energy Science & Technology ZDNY-280P72 | Hangzhou Zhejiang University Sunny Energy Science & Technology ZDNY-290C72 | Hangzhou Zhejiang University Sunny Energy Science & Technology ZDNY-290P72 | Hangzhou Zhejiang University Sunny Energy Science & Technology ZDNY-295P72 | Hangzhou Zhejiang University Sunny Energy Science & Technology ZDNY-300C72 | Hangzhou Zhejiang University Sunny Energy Science & Technology ZDNY-300P72 | Hangzhou Zhejiang University Sunny Energy Science & Technology ZDNY-305C72 | Hangzhou Zhejiang University Sunny Energy Science & Technology ZDNY-305P72 | Hangzhou Zhejiang University Sunny Energy Science & Technology ZDNY-310C72 | Hangzhou Zhejiang University Sunny Energy Science & Technology ZDNY-310P72 | Hangzhou Zhejiang University Sunny Energy Science & Technology ZDNY-315C72 | Hangzhou Zhejiang University Sunny Energy Science & Technology ZDNY-315P72 | Hangzhou Zhejiang University Sunny Energy Science & Technology ZDNY-320C72 | Hangzhou Zhejiang University Sunny Energy Science & Technology ZDNY-320P72 | Hangzhou Zhejiang University Sunny Energy Science & Technology ZDNY-325C72 | Hangzhou Zhejiang University Sunny Energy Science & Technology ZDNY-330C72 | Hangzhou Zhejiang University Sunny Energy Science & Technology ZDNY-335C72 | Hansol Technics Co._ Ltd HS238SB-A | Hansol Technics Co._ Ltd HS238SB-A06 | Hansol Technics Co._ Ltd HS240ME-V01 | Hansol Technics Co._ Ltd HS240SB-A | Hansol Technics Co._ Ltd HS240SB-A06 | Hansol Technics Co._ Ltd HS243SB-A | Hansol Technics Co._ Ltd HS243SB-A06 | Hansol Technics Co._ Ltd HS245ME-V01 | Hansol Technics Co._ Ltd HS245SB-A | Hansol Technics Co._ Ltd HS245SB-A06 | Hansol Technics Co._ Ltd HS248SB-A | Hansol Technics Co._ Ltd HS248SB-A06 | Hansol Technics Co._ Ltd HS250MB-AN3 | Hansol Technics Co._ Ltd HS250ME-V01 | Hansol Technics Co._ Ltd HS250NB-AN3 | Hansol Technics Co._ Ltd HS250SB-A | Hansol Technics Co._ Ltd HS250SB-A06 | Hansol Technics Co._ Ltd HS253SB-A | Hansol Technics Co._ Ltd HS253SB-A06 | Hansol Technics Co._ Ltd HS255MB-AN3 | Hansol Technics Co._ Ltd HS255ME-V01 | Hansol Technics Co._ Ltd HS255NB-AN3 | Hansol Technics Co._ Ltd HS255NB-AN4 | Hansol Technics Co._ Ltd HS255SB-A | Hansol Technics Co._ Ltd HS255SB-A06 | Hansol Technics Co._ Ltd HS255SE-V01 | Hansol Technics Co._ Ltd HS258SB-A | Hansol Technics Co._ Ltd HS258SB-A06 | Hansol Technics Co._ Ltd HS260MB-AN3 | Hansol Technics Co._ Ltd HS260ME-V01 | Hansol Technics Co._ Ltd HS260NB-AN3 | Hansol Technics Co._ Ltd HS260NB-AN4 | Hansol Technics Co._ Ltd HS260PB-AN1 | Hansol Technics Co._ Ltd HS260SB-A | Hansol Technics Co._ Ltd HS260SB-A06 | Hansol Technics Co._ Ltd HS260SE-V01 | Hansol Technics Co._ Ltd HS265MB-AN3 | Hansol Technics Co._ Ltd HS265ME-V01 | Hansol Technics Co._ Ltd HS265NB-AN3 | Hansol Technics Co._ Ltd HS265NB-AN4 | Hansol Technics Co._ Ltd HS265PB-AN1 | Hansol Technics Co._ Ltd HS265SE-V01 | Hansol Technics Co._ Ltd HS270MB-AN3 | Hansol Technics Co._ Ltd HS270ME-V01 | Hansol Technics Co._ Ltd HS270NB-AN3 | Hansol Technics Co._ Ltd HS270NB-AN4 | Hansol Technics Co._ Ltd HS270PB-AN1 | Hansol Technics Co._ Ltd HS270SE-V01 | Hansol Technics Co._ Ltd HS275NB-AN4 | Hansol Technics Co._ Ltd HS275PB-AN1 | Hansol Technics Co._ Ltd HS275SE-V01 | Hansol Technics Co._ Ltd HS275TB-AN3 | Hansol Technics Co._ Ltd HS280PB-AN1 | Hansol Technics Co._ Ltd HS280SE-V01 | Hansol Technics Co._ Ltd HS280TB-AN3 | Hansol Technics Co._ Ltd HS280TB-AN4 | Hansol Technics Co._ Ltd HS285TB-AN3 | Hansol Technics Co._ Ltd HS285TB-AN4 | Hansol Technics Co._ Ltd HS285UB-AN1 [Wht] | Hansol Technics Co._ Ltd HS290TB-AN3 | Hansol Technics Co._ Ltd HS290TB-AN4 | Hansol Technics Co._ Ltd HS290UB-AN1 [Blk] | Hansol Technics Co._ Ltd HS290UB-AN1 [Wht] | Hansol Technics Co._ Ltd HS295ME-V01 | Hansol Technics Co._ Ltd HS295TB-AN3 | Hansol Technics Co._ Ltd HS295TB-AN4 | Hansol Technics Co._ Ltd HS295UB-AN1 [Blk] | Hansol Technics Co._ Ltd HS295UB-AN1 [Wht] | Hansol Technics Co._ Ltd HS300MD-AN3 | Hansol Technics Co._ Ltd HS300ME-V01 | Hansol Technics Co._ Ltd HS300ND-AN3 | Hansol Technics Co._ Ltd HS300TB-AN3 | Hansol Technics Co._ Ltd HS300TB-AN4 | Hansol Technics Co._ Ltd HS300UB-AN1 [Blk] | Hansol Technics Co._ Ltd HS300UB-AN1 [Wht] | Hansol Technics Co._ Ltd HS305MD-AN3 | Hansol Technics Co._ Ltd HS305ME-V01 | Hansol Technics Co._ Ltd HS305ND-AN3 | Hansol Technics Co._ Ltd HS305ND-AN4 | Hansol Technics Co._ Ltd HS305SE-V01 | Hansol Technics Co._ Ltd HS305UB-AN1 [Blk] | Hansol Technics Co._ Ltd HS305UB-AN1 [Wht] | Hansol Technics Co._ Ltd HS310MD-AN3 | Hansol Technics Co._ Ltd HS310ME-V01 | Hansol Technics Co._ Ltd HS310ND-AN3 | Hansol Technics Co._ Ltd HS310ND-AN4 | Hansol Technics Co._ Ltd HS310SE-V01 | Hansol Technics Co._ Ltd HS310UB-AN1 [Blk] | Hansol Technics Co._ Ltd HS310UB-AN1 [Wht] | Hansol Technics Co._ Ltd HS315MD-AN3 | Hansol Technics Co._ Ltd HS315ME-V01 | Hansol Technics Co._ Ltd HS315ND-AN3 | Hansol Technics Co._ Ltd HS315ND-AN4 | Hansol Technics Co._ Ltd HS315PD-AN1 | Hansol Technics Co._ Ltd HS315SE-V01 | Hansol Technics Co._ Ltd HS315UB-AN1 [Blk] | Hansol Technics Co._ Ltd HS315UB-AN1 [Wht] | Hansol Technics Co._ Ltd HS320MD-AN3 | Hansol Technics Co._ Ltd HS320ME-V01 | Hansol Technics Co._ Ltd HS320ND-AN3 | Hansol Technics Co._ Ltd HS320ND-AN4 | Hansol Technics Co._ Ltd HS320PD-AN1 | Hansol Technics Co._ Ltd HS320SE-V01 | Hansol Technics Co._ Ltd HS320UB-AN1 [Blk] | Hansol Technics Co._ Ltd HS320UB-AN1 [Wht] | Hansol Technics Co._ Ltd HS325MD-AN3 | Hansol Technics Co._ Ltd HS325ME-V01 | Hansol Technics Co._ Ltd HS325ND-AN3 | Hansol Technics Co._ Ltd HS325ND-AN4 | Hansol Technics Co._ Ltd HS325PD-AN1 | Hansol Technics Co._ Ltd HS325SE-V01 | Hansol Technics Co._ Ltd HS325TD-AN3 | Hansol Technics Co._ Ltd HS330ND-AN4 | Hansol Technics Co._ Ltd HS330PD-AN1 | Hansol Technics Co._ Ltd HS330SE-V01 | Hansol Technics Co._ Ltd HS330TD-AN3 | Hansol Technics Co._ Ltd HS330TD-AN4 | Hansol Technics Co._ Ltd HS335ND-AN4 | Hansol Technics Co._ Ltd HS335PD-AN1 | Hansol Technics Co._ Ltd HS335SE-V01 | Hansol Technics Co._ Ltd HS335TD-AN3 | Hansol Technics Co._ Ltd HS335TD-AN4 | Hansol Technics Co._ Ltd HS340PD-AN1 | Hansol Technics Co._ Ltd HS340TD-AN3 | Hansol Technics Co._ Ltd HS340TD-AN4 | Hansol Technics Co._ Ltd HS340UD-AN1 [Wht] | Hansol Technics Co._ Ltd HS345PD-AN1 | Hansol Technics Co._ Ltd HS345TD-AN3 | Hansol Technics Co._ Ltd HS345TD-AN4 | Hansol Technics Co._ Ltd HS345UD-AN1 [Blk] | Hansol Technics Co._ Ltd HS345UD-AN1 [Wht] | Hansol Technics Co._ Ltd HS350TD-AN3 | Hansol Technics Co._ Ltd HS350TD-AN4 | Hansol Technics Co._ Ltd HS350UD-AN1 [Blk] | Hansol Technics Co._ Ltd HS350UD-AN1 [Wht] | Hansol Technics Co._ Ltd HS355TD-AN3 | Hansol Technics Co._ Ltd HS355TD-AN4 | Hansol Technics Co._ Ltd HS355UD-AN1 [Blk] | Hansol Technics Co._ Ltd HS355UD-AN1 [Wht] | Hansol Technics Co._ Ltd HS360TD-AN4 | Hansol Technics Co._ Ltd HS360UD-AN1 [Blk] | Hansol Technics Co._ Ltd HS360UD-AN1 [Wht] | Hansol Technics Co._ Ltd HS365UD-AN1 [Blk] | Hansol Technics Co._ Ltd HS365UD-AN1 [Wht] | Hansol Technics Co._ Ltd HS370UD-AN1 [Blk] | Hansol Technics Co._ Ltd HS370UD-AN1 [Wht] | Hansol Technics Co._ Ltd HS380UE-AN1 | Hansol Technics Co._ Ltd HS385UE-AN1 | Hansol Technics Co._ Ltd HS390UE-AN1 | Hansol Technics Co._ Ltd HS395UE-AN1 | Hansol Technics Co._ Ltd HS400UE-AN1 | Hansol Technics Co._ Ltd HS405UE-AN1 | Hansol Technics Co._ Ltd HS410UE-AN1 | Hansol Technics Co._ Ltd HS415UE-AN1 | Hansol Technics Co._ Ltd HS420UE-AN1 | Hanwha Q CELLS Q.PRO-G3 240 | Hanwha Q CELLS Q.PRO BFR - G3 245 | Hanwha Q CELLS Q.PRO-G3 245 | Hanwha Q CELLS Q.PRO BFR - G3 250 | Hanwha Q CELLS Q.PRO-G3 250 | Hanwha Q CELLS Q.PRO BFR - G3 255 | Hanwha Q CELLS Q.PRO BFR G4 255 | Hanwha Q CELLS Q.PRO BFR-G4.1 255 | Hanwha Q CELLS Q.PRO G4.1/SC 255 | Hanwha Q CELLS Q.PRO-G3 255 | Hanwha Q CELLS Q.PRO-G4 255 | Hanwha Q CELLS Q.PRO-G4/SC 255 | Hanwha Q CELLS Q.PRO BFR - G3 260 | Hanwha Q CELLS Q.PRO BFR G4 260 | Hanwha Q CELLS Q.PRO BFR-G4.1 260 | Hanwha Q CELLS Q.PRO BFR-G4.3 260 | Hanwha Q CELLS Q.PRO G4.1/SC 260 | Hanwha Q CELLS Q.PRO-G3 260 | Hanwha Q CELLS Q.PRO-G4 260 | Hanwha Q CELLS Q.PRO-G4/SC 260 | Hanwha Q CELLS Q.PEAK BLK-G3 265 | Hanwha Q CELLS Q.PEAK-G3 265 | Hanwha Q CELLS Q.PRO BFR - G3 265 | Hanwha Q CELLS Q.PRO BFR G4 265 | Hanwha Q CELLS Q.PRO BFR-G4.1 265 | Hanwha Q CELLS Q.PRO BFR-G4.3 265 | Hanwha Q CELLS Q.PRO G4.1/SC 265 | Hanwha Q CELLS Q.PRO-G3 265 | Hanwha Q CELLS Q.PRO-G4 265 | Hanwha Q CELLS Q.PRO-G4/SC 265 | Hanwha Q CELLS Q.PEAK BLK-G3 270 | Hanwha Q CELLS Q.PEAK-G3 270 | Hanwha Q CELLS Q.PLUS BFR G3.1 270 | Hanwha Q CELLS Q.PLUS BFR G4.1 270 | Hanwha Q CELLS Q.PLUS G4 270 | Hanwha Q CELLS Q.PLUS-G3 270 | Hanwha Q CELLS Q.PLUS-G4.1/SC 270 | Hanwha Q CELLS Q.PEAK BLK-G3 275 | Hanwha Q CELLS Q.PEAK-G3 275 | Hanwha Q CELLS Q.PLUS BFR G3.1 275 | Hanwha Q CELLS Q.PLUS BFR G4.1 275 | Hanwha Q CELLS Q.PLUS G4 275 | Hanwha Q CELLS Q.PLUS-G3 275 | Hanwha Q CELLS Q.PLUS-G4.1/SC 275 | Hanwha Q CELLS B.LINE PEAK BLK-G4.1 280 | Hanwha Q CELLS Q.PEAK-G3 280 | Hanwha Q CELLS Q.PLUS BFR G3.1 280 | Hanwha Q CELLS Q.PLUS BFR G4.1 280 | Hanwha Q CELLS Q.PLUS BFR-G4.1/TAA 280 | Hanwha Q CELLS Q.PLUS G4 280 | Hanwha Q CELLS Q.PLUS-G3 280 | Hanwha Q CELLS Q.PLUS-G4.1/SC 280 | Hanwha Q CELLS B.LINE PEAK BLK-G4.1 285 | Hanwha Q CELLS B.LINE PEAK BLK-G4.1/SC 285 | Hanwha Q CELLS Q.PEAK BLK-G4.1 285 | Hanwha Q CELLS Q.PEAK BLK-G4.1/SC 285 | Hanwha Q CELLS Q.PEAK BLK-G4.1/TAA 285 | Hanwha Q CELLS Q.PLUS BFR-G4.1/TAA 285 | Hanwha Q CELLS Q.PLUS-G4.1/SC 285 | Hanwha Q CELLS Q.PEAK BLK-G3.1 290 | Hanwha Q CELLS Q.PEAK BLK-G4.1 290 | Hanwha Q CELLS Q.PEAK BLK-G4.1/SC 290 | Hanwha Q CELLS Q.PEAK BLK-G4.1/TAA 290 | Hanwha Q Cells Q.PEAK-G4.1 290 | Hanwha Q CELLS Q.PLUS-BFR G4.1/TAA 290 | Hanwha Q CELLS Q.PRO L 290 | Hanwha Q CELLS Q.PEAK BLK-G3.1 295 | Hanwha Q CELLS Q.PEAK BLK-G4.1 295 | Hanwha Q CELLS Q.PEAK BLK-G4.1/SC 295 | Hanwha Q CELLS Q.PEAK BLK-G4.1/TAA 295 | Hanwha Q CELLS Q.PEAK G3.1 295 | Hanwha Q CELLS Q.PEAK G4.1/SC 295 | Hanwha Q Cells Q.PEAK-G4.1 295 | Hanwha Q CELLS Q.PRO L 295 | Hanwha Q CELLS Q.PEAK BLK-G4.1 300 | Hanwha Q CELLS Q.PEAK BLK-G4.1 300W | Hanwha Q CELLS Q.PEAK BLK-G4.1/TAA 300 | Hanwha Q CELLS Q.PEAK DUO BLK-G5 300 | Hanwha Q CELLS Q.PEAK G3.1 300 | Hanwha Q CELLS Q.PEAK G4.1/SC 300 | Hanwha Q CELLS Q.PEAK G4.1/TAA 300 | Hanwha Q Cells Q.PEAK-G4.1 300 | Hanwha Q CELLS Q.PRO L 300 | Hanwha Q CELLS Q.PRO L-G3 300 | Hanwha Q CELLS Q.Peak Duo-G5 305 | Hanwha Q CELLS Q.PEAK G3.1 305 | Hanwha Q CELLS Q.PEAK G4.1/SC 305 | Hanwha Q CELLS Q.PEAK G4.1/TAA 305 | Hanwha Q Cells Q.PEAK-G4.1 305 | Hanwha Q CELLS Q.PRO L 305 | Hanwha Q CELLS Q.PRO L-G2 305 | Hanwha Q CELLS Q.PRO L-G2.3 305 | Hanwha Q CELLS Q.PRO L-G3 305 | Hanwha Q CELLS B.LINE PRO L-G4.1 307 | Hanwha Q CELLS Q.PEAK DUO BLK-G5 310 | Hanwha Q CELLS Q.Peak Duo-G5 310 | Hanwha Q CELLS Q.PRO L 310 | Hanwha Q CELLS Q.PRO L G4 310 | Hanwha Q CELLS Q.PRO L G4.1 310 | Hanwha Q CELLS Q.PRO L-G2 310 | Hanwha Q CELLS Q.PRO L-G2.3 310 | Hanwha Q CELLS Q.PRO L-G3 310 | Hanwha Q CELLS Q.PRO L-G3.1 310 | Hanwha Q CELLS Q.PEAK DUO BLK-G5 315 | Hanwha Q CELLS Q.Peak Duo-G5 315 | Hanwha Q CELLS Q.PRO L G2 315 | Hanwha Q CELLS Q.PRO L G4 315 | Hanwha Q CELLS Q.PRO L G4.1 315 | Hanwha Q CELLS Q.PRO L-G2.3 315 | Hanwha Q CELLS Q.PRO L-G3 315 | Hanwha Q CELLS Q.PRO L-G3.1 315 | Hanwha Q CELLS B.LINE PLUS L-G4.2 317 | Hanwha Q CELLS Q.PEAK DUO BLK-G5 320 | Hanwha Q CELLS Q.Peak Duo-G5 320 | Hanwha Q CELLS Q.PLUS L-G4 320 | Hanwha Q CELLS Q.PLUS L-G4.1 320 | Hanwha Q CELLS Q.PLUS L-G4.2 320 | Hanwha Q CELLS Q.PRO L G4 320 | Hanwha Q CELLS Q.PRO L G4.1 320 | Hanwha Q CELLS Q.PRO L-G3.1 320 | Hanwha Q CELLS B.LINE PLUS L-G4.1 322 | Hanwha Q CELLS B.LINE PRO L-G4.1 322 | Hanwha Q CELLS B.LINE PLUS L-G4.2 325 | Hanwha Q CELLS Q.Peak Duo-G5 325 | Hanwha Q CELLS Q.PLUS L-G4 325 | Hanwha Q CELLS Q.PLUS L-G4.1 325 | Hanwha Q CELLS Q.PLUS L-G4.2 325 | Hanwha Q CELLS B.LINE PLUS L-G4.2 330 | Hanwha Q CELLS Q.PLUS L-G4 330 | Hanwha Q CELLS Q.PLUS L-G4.1 330 | Hanwha Q CELLS Q.PLUS L-G4.2 330 | Hanwha Q CELLS B.LINE PLUS L-G4.2 332 | Hanwha Q CELLS B.LINE PLUS L-G4.2 335 | Hanwha Q CELLS Q.PLUS L-G4 335 | Hanwha Q CELLS Q.PLUS L-G4.1 335 | Hanwha Q CELLS Q.PLUS L-G4.2 335 | Hanwha Q CELLS Q.PLUS L-G4.2/TAA 335 | Hanwha Q CELLS Q.PLUS L-G4.2 340W | Hanwha Q CELLS Q.PLUS L-G4.2/TAA 340 | Hanwha Q CELLS Q.PEAK L-G4.1 345 | Hanwha Q CELLS Q.PLUS L-G4.2 345W | Hanwha Q CELLS Q.PLUS L-G4.2/TAA 345 | Hanwha Q CELLS Q.PEAK L-G4.1 350 | Hanwha Q CELLS Q.PLUS L-G4.2/TAA 350 | Hanwha Q CELLS Q.PEAK L-G4.1 355 | Hanwha Q CELLS Q.PEAK L-G4.1 360 | Hanwha Q CELLS Q.PEAK L-G4.2 360W | Hanwha Q CELLS Q.PEAK L-G4.2 365 | Hanwha Q CELLS Q.PEAK L-G4.2 370 | Hanwha Q Cells Q.PEAK DUO L-G5.2 380 | Hanwha Q Cells Q.PEAK DUO L-G5.2 385 | Hanwha Q Cells Q.PEAK DUO L-G5.2 390 | Hanwha Q CELLS (Qidong) HSL60P6-PA-3-230Q | Hanwha Q CELLS (Qidong) HSL60P6-PA-3-230QB | Hanwha Q CELLS (Qidong) HSL60P6-PA-3-230QW | Hanwha Q CELLS (Qidong) HSL60P6-PB-3-230Q | Hanwha Q CELLS (Qidong) HSL60P6-PB-3-230QB | Hanwha Q CELLS (Qidong) HSL60P6-PB-3-230QW | Hanwha Q CELLS (Qidong) HSL60P6-PA-0-235T | Hanwha Q CELLS (Qidong) HSL60P6-PA-0-235TB | Hanwha Q CELLS (Qidong) HSL60P6-PA-0-235TW | Hanwha Q CELLS (Qidong) HSL60P6-PA-2-235Q | Hanwha Q CELLS (Qidong) HSL60P6-PA-2-235QB | Hanwha Q CELLS (Qidong) HSL60P6-PA-2-235QW | Hanwha Q CELLS (Qidong) HSL60P6-PA-3-235Q | Hanwha Q CELLS (Qidong) HSL60P6-PA-3-235QB | Hanwha Q CELLS (Qidong) HSL60P6-PA-3-235QW | Hanwha Q CELLS (Qidong) HSL60P6-PA-4-235Q | Hanwha Q CELLS (Qidong) HSL60P6-PA-4-235QB | Hanwha Q CELLS (Qidong) HSL60P6-PA-4-235QW | Hanwha Q CELLS (Qidong) HSL60P6-PA-4-235T | Hanwha Q CELLS (Qidong) HSL60P6-PA-4-235TB | Hanwha Q CELLS (Qidong) HSL60P6-PA-4-235TW | Hanwha Q CELLS (Qidong) HSL60P6-PB-2-235Q | Hanwha Q CELLS (Qidong) HSL60P6-PB-2-235QB | Hanwha Q CELLS (Qidong) HSL60P6-PB-2-235QW | Hanwha Q CELLS (Qidong) HSL60P6-PB-3-235Q | Hanwha Q CELLS (Qidong) HSL60P6-PB-3-235QB | Hanwha Q CELLS (Qidong) HSL60P6-PB-3-235QW | Hanwha Q CELLS (Qidong) HSL60P6-PB-4-235Q | Hanwha Q CELLS (Qidong) HSL60P6-PB-4-235QB | Hanwha Q CELLS (Qidong) HSL60P6-PB-4-235QW | Hanwha Q CELLS (Qidong) HSL60M6-HA-0-240T | Hanwha Q CELLS (Qidong) HSL60M6-HB-0-240T | Hanwha Q CELLS (Qidong) HSL60M6-HB-4-240T | Hanwha Q CELLS (Qidong) HSL60M6-HB-4-240TB | Hanwha Q CELLS (Qidong) HSL60M6-HB-4-240TW | Hanwha Q CELLS (Qidong) HSL60P6-PA-0-240T | Hanwha Q CELLS (Qidong) HSL60P6-PA-0-240TB | Hanwha Q CELLS (Qidong) HSL60P6-PA-0-240TW | Hanwha Q CELLS (Qidong) HSL60P6-PA-2-240Q | Hanwha Q CELLS (Qidong) HSL60P6-PA-2-240QB | Hanwha Q CELLS (Qidong) HSL60P6-PA-2-240QW | Hanwha Q CELLS (Qidong) HSL60P6-PA-3-240Q | Hanwha Q CELLS (Qidong) HSL60P6-PA-3-240QB | Hanwha Q CELLS (Qidong) HSL60P6-PA-3-240QW | Hanwha Q CELLS (Qidong) HSL60P6-PA-4-240Q | Hanwha Q CELLS (Qidong) HSL60P6-PA-4-240QB | Hanwha Q CELLS (Qidong) HSL60P6-PA-4-240QW | Hanwha Q CELLS (Qidong) HSL60P6-PA-4-240T | Hanwha Q CELLS (Qidong) HSL60P6-PA-4-240TB | Hanwha Q CELLS (Qidong) HSL60P6-PA-4-240TW | Hanwha Q CELLS (Qidong) HSL60P6-PB-0-240T | Hanwha Q CELLS (Qidong) HSL60P6-PB-0-240TB | Hanwha Q CELLS (Qidong) HSL60P6-PB-0-240TW | Hanwha Q CELLS (Qidong) HSL60P6-PB-2-240Q | Hanwha Q CELLS (Qidong) HSL60P6-PB-2-240QB | Hanwha Q CELLS (Qidong) HSL60P6-PB-2-240QW | Hanwha Q CELLS (Qidong) HSL60P6-PB-3-240QB | Hanwha Q CELLS (Qidong) HSL60P6-PB-4-240Q | Hanwha Q CELLS (Qidong) HSL60P6-PB-4-240QW | Hanwha Q CELLS (Qidong) HSL60P6-PB-4-240T | Hanwha Q CELLS (Qidong) HSL60P6-PB-4-240TB | Hanwha Q CELLS (Qidong) HSL60P6-PB-4-240TW | Hanwha Q CELLS (Qidong) HSL60M6-HB-0-245TW | Hanwha Q CELLS (Qidong) HSL60M6-HB-4-245T | Hanwha Q CELLS (Qidong) HSL60M6-HB-4-245TB | Hanwha Q CELLS (Qidong) HSL60M6-HB-4-245TW | Hanwha Q CELLS (Qidong) HSL60P6-PA-0-245T | Hanwha Q CELLS (Qidong) HSL60P6-PA-0-245TB | Hanwha Q CELLS (Qidong) HSL60P6-PA-0-245TW | Hanwha Q CELLS (Qidong) HSL60P6-PA-2-245Q | Hanwha Q CELLS (Qidong) HSL60P6-PA-2-245QB | Hanwha Q CELLS (Qidong) HSL60P6-PA-2-245QW | Hanwha Q CELLS (Qidong) HSL60P6-PA-3-245Q | Hanwha Q CELLS (Qidong) HSL60P6-PA-3-245QB | Hanwha Q CELLS (Qidong) HSL60P6-PA-3-245QW | Hanwha Q CELLS (Qidong) HSL60P6-PA-4-245Q | Hanwha Q CELLS (Qidong) HSL60P6-PA-4-245QB | Hanwha Q CELLS (Qidong) HSL60P6-PA-4-245QW | Hanwha Q CELLS (Qidong) HSL60P6-PA-4-245T | Hanwha Q CELLS (Qidong) HSL60P6-PA-4-245TB | Hanwha Q CELLS (Qidong) HSL60P6-PA-4-245TW | Hanwha Q CELLS (Qidong) HSL60P6-PB-0-245T | Hanwha Q CELLS (Qidong) HSL60P6-PB-0-245TB | Hanwha Q CELLS (Qidong) HSL60P6-PB-0-245TW | Hanwha Q CELLS (Qidong) HSL60P6-PB-2-245Q | Hanwha Q CELLS (Qidong) HSL60P6-PB-2-245QB | Hanwha Q CELLS (Qidong) HSL60P6-PB-2-245QW | Hanwha Q CELLS (Qidong) HSL60P6-PB-3-245Q | Hanwha Q CELLS (Qidong) HSL60P6-PB-3-245QB | Hanwha Q CELLS (Qidong) HSL60P6-PB-3-245QW | Hanwha Q CELLS (Qidong) HSL60P6-PB-4-245 | Hanwha Q CELLS (Qidong) HSL60P6-PB-4-245Q | Hanwha Q CELLS (Qidong) HSL60P6-PB-4-245QB | Hanwha Q CELLS (Qidong) HSL60P6-PB-4-245QW | Hanwha Q CELLS (Qidong) HSL60P6-PB-4-245T | Hanwha Q CELLS (Qidong) HSL60P6-PB-4-245TB | Hanwha Q CELLS (Qidong) HSL60P6-PB-4-245TW | Hanwha Q CELLS (Qidong) HSL60P6-PB-4-245W | Hanwha Q CELLS (Qidong) HSL60M6-HA-0-250T | Hanwha Q CELLS (Qidong) HSL60P6-PA-2-250QB | Hanwha Q CELLS (Qidong) HSL60P6-PA-2-250QW | Hanwha Q CELLS (Qidong) HSL60P6-PA-3-250Q | Hanwha Q CELLS (Qidong) HSL60P6-PA-3-250QB | Hanwha Q CELLS (Qidong) HSL60P6-PA-3-250QW | Hanwha Q CELLS (Qidong) HSL60P6-PA-4-250Q | Hanwha Q CELLS (Qidong) HSL60P6-PA-4-250QB | Hanwha Q CELLS (Qidong) HSL60P6-PA-4-250QW | Hanwha Q CELLS (Qidong) HSL60P6-PA-4-250T | Hanwha Q CELLS (Qidong) HSL60P6-PA-4-250TB | Hanwha Q CELLS (Qidong) HSL60P6-PA-4-250TW | Hanwha Q CELLS (Qidong) HSL60P6-PB-0-250T | Hanwha Q CELLS (Qidong) HSL60P6-PB-0-250TB | Hanwha Q CELLS (Qidong) HSL60P6-PB-0-250TW | Hanwha Q CELLS (Qidong) HSL60P6-PB-2-250Q | Hanwha Q CELLS (Qidong) HSL60P6-PB-2-250QB | Hanwha Q CELLS (Qidong) HSL60P6-PB-2-250QW | Hanwha Q CELLS (Qidong) HSL60P6-PB-3-250Q | Hanwha Q CELLS (Qidong) HSL60P6-PB-3-250QB | Hanwha Q CELLS (Qidong) HSL60P6-PB-3-250QW | Hanwha Q CELLS (Qidong) HSL60P6-PB-4-250 | Hanwha Q CELLS (Qidong) HSL60P6-PB-4-250Q | Hanwha Q CELLS (Qidong) HSL60P6-PB-4-250QB | Hanwha Q CELLS (Qidong) HSL60P6-PB-4-250QW | Hanwha Q CELLS (Qidong) HSL60P6-PB-4-250T | Hanwha Q CELLS (Qidong) HSL60P6-PB-4-250TB | Hanwha Q CELLS (Qidong) HSL60P6-PB-4-250TW | Hanwha Q CELLS (Qidong) HSL60P6-PB-4-250W | Hanwha Q CELLS (Qidong) HSL60P6-PC-3-250 | Hanwha Q CELLS (Qidong) HSL60P6-PC-3-250W | Hanwha Q CELLS (Qidong) HSL60M6-HA-4-255T | Hanwha Q CELLS (Qidong) HSL60M6-HA-4-255TB | Hanwha Q CELLS (Qidong) HSL60M6-HA-4-255TW | Hanwha Q CELLS (Qidong) HSL60M6-HB-4-255T | Hanwha Q CELLS (Qidong) HSL60M6-HB-4-255TB | Hanwha Q CELLS (Qidong) HSL60M6-HB-4-255TW | Hanwha Q CELLS (Qidong) HSL60P6-PA-0-255T | Hanwha Q CELLS (Qidong) HSL60P6-PA-0-255TB | Hanwha Q CELLS (Qidong) HSL60P6-PA-0-255TW | Hanwha Q CELLS (Qidong) HSL60P6-PA-2-255Q | Hanwha Q CELLS (Qidong) HSL60P6-PA-2-255QB | Hanwha Q CELLS (Qidong) HSL60P6-PA-2-255QW | Hanwha Q CELLS (Qidong) HSL60P6-PA-3-255Q | Hanwha Q CELLS (Qidong) HSL60P6-PA-3-255QB | Hanwha Q CELLS (Qidong) HSL60P6-PA-3-255QW | Hanwha Q CELLS (Qidong) HSL60P6-PA-4-255Q | Hanwha Q CELLS (Qidong) HSL60P6-PA-4-255QB | Hanwha Q CELLS (Qidong) HSL60P6-PA-4-255QW | Hanwha Q CELLS (Qidong) HSL60P6-PA-4-255T | Hanwha Q CELLS (Qidong) HSL60P6-PA-4-255TB | Hanwha Q CELLS (Qidong) HSL60P6-PA-4-255TW | Hanwha Q CELLS (Qidong) HSL60P6-PB-0-255T | Hanwha Q CELLS (Qidong) HSL60P6-PB-0-255TB | Hanwha Q CELLS (Qidong) HSL60P6-PB-0-255TW | Hanwha Q CELLS (Qidong) HSL60P6-PB-2-255Q | Hanwha Q CELLS (Qidong) HSL60P6-PB-2-255QB | Hanwha Q CELLS (Qidong) HSL60P6-PB-2-255QW | Hanwha Q CELLS (Qidong) HSL60P6-PB-3-255Q | Hanwha Q CELLS (Qidong) HSL60P6-PB-3-255QB | Hanwha Q CELLS (Qidong) HSL60P6-PB-3-255QW | Hanwha Q CELLS (Qidong) HSL60P6-PB-4-255 | Hanwha Q CELLS (Qidong) HSL60P6-PB-4-255Q | Hanwha Q CELLS (Qidong) HSL60P6-PB-4-255QB | Hanwha Q CELLS (Qidong) HSL60P6-PB-4-255QW | Hanwha Q CELLS (Qidong) HSL60P6-PB-4-255T | Hanwha Q CELLS (Qidong) HSL60P6-PB-4-255TB | Hanwha Q CELLS (Qidong) HSL60P6-PB-4-255TW | Hanwha Q CELLS (Qidong) HSL60P6-PB-4-255W | Hanwha Q CELLS (Qidong) HSL60P6-PC-3-255 | Hanwha Q CELLS (Qidong) HSL60P6-PC-3-255W | Hanwha Q CELLS (Qidong) HSL60M6-HA-4-260T | Hanwha Q CELLS (Qidong) HSL60M6-HA-4-260TB | Hanwha Q CELLS (Qidong) HSL60M6-HA-4-260TW | Hanwha Q CELLS (Qidong) HSL60M6-HB-0-260T | Hanwha Q CELLS (Qidong) HSL60M6-HB-4-260T | Hanwha Q CELLS (Qidong) HSL60M6-HB-4-260TB | Hanwha Q CELLS (Qidong) HSL60M6-HB-4-260TW | Hanwha Q CELLS (Qidong) HSL60P6-PB-0-260T | Hanwha Q CELLS (Qidong) HSL60P6-PB-0-260TW | Hanwha Q CELLS (Qidong) HSL60P6-PB-4-260 | Hanwha Q CELLS (Qidong) HSL60P6-PB-4-260T | Hanwha Q CELLS (Qidong) HSL60P6-PB-4-260TW | Hanwha Q CELLS (Qidong) HSL60P6-PB-4-260W | Hanwha Q CELLS (Qidong) HSL60P6-PC-3-260 | Hanwha Q CELLS (Qidong) HSL60P6-PC-3-260W | Hanwha Q CELLS (Qidong) HSL60P6-PB-0-265T | Hanwha Q CELLS (Qidong) HSL60P6-PB-0-265TW | Hanwha Q CELLS (Qidong) HSL60P6-PB-4-265T | Hanwha Q CELLS (Qidong) HSL60P6-PB-4-265TW | Hanwha Q CELLS (Qidong) HSL60P6-PC-3-265 | Hanwha Q CELLS (Qidong) HSL60P6-PC-3-265W | Hanwha Q CELLS (Qidong) HSL60P6-PB-0-270T | Hanwha Q CELLS (Qidong) HSL60P6-PB-0-270TW | Hanwha Q CELLS (Qidong) HSL60P6-PB-4-270T | Hanwha Q CELLS (Qidong) HSL60P6-PB-4-270TW | Hanwha Q CELLS (Qidong) HSL60P6-PC-3-270 | Hanwha Q CELLS (Qidong) HSL60P6-PC-3-275 | Hanwha Q CELLS (Qidong) HSL72P6-PA-0-275T | Hanwha Q CELLS (Qidong) HSL72P6-PA-0-275TB | Hanwha Q CELLS (Qidong) HSL72P6-PA-0-275TW | Hanwha Q CELLS (Qidong) HSL72P6-PA-4-275T | Hanwha Q CELLS (Qidong) HSL72P6-PA-4-275TB | Hanwha Q CELLS (Qidong) HSL72P6-PA-4-275TW | Hanwha Q CELLS (Qidong) HSL72P6-PA-0-280T | Hanwha Q CELLS (Qidong) HSL72P6-PA-0-280TB | Hanwha Q CELLS (Qidong) HSL72P6-PA-0-280TW | Hanwha Q CELLS (Qidong) HSL72P6-PA-2-280Q | Hanwha Q CELLS (Qidong) HSL72P6-PA-2-280QB | Hanwha Q CELLS (Qidong) HSL72P6-PA-2-280QW | Hanwha Q CELLS (Qidong) HSL72P6-PA-3-280Q | Hanwha Q CELLS (Qidong) HSL72P6-PA-3-280QB | Hanwha Q CELLS (Qidong) HSL72P6-PA-3-280QW | Hanwha Q CELLS (Qidong) HSL72P6-PA-4-280Q | Hanwha Q CELLS (Qidong) HSL72P6-PA-4-280QB | Hanwha Q CELLS (Qidong) HSL72P6-PA-4-280QW | Hanwha Q CELLS (Qidong) HSL72P6-PA-4-280T | Hanwha Q CELLS (Qidong) HSL72P6-PA-4-280TB | Hanwha Q CELLS (Qidong) HSL72P6-PA-4-280TW | Hanwha Q CELLS (Qidong) HSL72P6-PB-2-280Q | Hanwha Q CELLS (Qidong) HSL72P6-PB-2-280QB | Hanwha Q CELLS (Qidong) HSL72P6-PB-2-280QW | Hanwha Q CELLS (Qidong) HSL72P6-PB-3-280Q | Hanwha Q CELLS (Qidong) HSL72P6-PB-3-280QB | Hanwha Q CELLS (Qidong) HSL72P6-PB-3-280QW | Hanwha Q CELLS (Qidong) HSL72P6-PB-4-280Q | Hanwha Q CELLS (Qidong) HSL72P6-PB-4-280QB | Hanwha Q CELLS (Qidong) HSL72P6-PB-4-280QW | Hanwha Q CELLS (Qidong) HSL72M6-HA-0-285T | Hanwha Q CELLS (Qidong) HSL72M6-HA-0-285TB | Hanwha Q CELLS (Qidong) HSL72M6-HA-0-285TW | Hanwha Q CELLS (Qidong) HSL72M6-HA-4-285T | Hanwha Q CELLS (Qidong) HSL72M6-HA-4-285TB | Hanwha Q CELLS (Qidong) HSL72M6-HA-4-285TW | Hanwha Q CELLS (Qidong) HSL72M6-HB-0-285T | Hanwha Q CELLS (Qidong) HSL72M6-HB-0-285TB | Hanwha Q CELLS (Qidong) HSL72M6-HB-0-285TW | Hanwha Q CELLS (Qidong) HSL72M6-HB-4-285T | Hanwha Q CELLS (Qidong) HSL72M6-HB-4-285TB | Hanwha Q CELLS (Qidong) HSL72M6-HB-4-285TW | Hanwha Q CELLS (Qidong) HSL72P6-PA-0-285T | Hanwha Q CELLS (Qidong) HSL72P6-PA-0-285TB | Hanwha Q CELLS (Qidong) HSL72P6-PA-0-285TW | Hanwha Q CELLS (Qidong) HSL72P6-PA-2-285Q | Hanwha Q CELLS (Qidong) HSL72P6-PA-2-285QB | Hanwha Q CELLS (Qidong) HSL72P6-PA-2-285QW | Hanwha Q CELLS (Qidong) HSL72P6-PA-3-285Q | Hanwha Q CELLS (Qidong) HSL72P6-PA-3-285QB | Hanwha Q CELLS (Qidong) HSL72P6-PA-3-285QW | Hanwha Q CELLS (Qidong) HSL72P6-PA-4-285Q | Hanwha Q CELLS (Qidong) HSL72P6-PA-4-285QB | Hanwha Q CELLS (Qidong) HSL72P6-PA-4-285QW | Hanwha Q CELLS (Qidong) HSL72P6-PA-4-285T | Hanwha Q CELLS (Qidong) HSL72P6-PA-4-285TB | Hanwha Q CELLS (Qidong) HSL72P6-PA-4-285TW | Hanwha Q CELLS (Qidong) HSL72P6-PB-0-285T | Hanwha Q CELLS (Qidong) HSL72P6-PB-0-285TB | Hanwha Q CELLS (Qidong) HSL72P6-PB-0-285TW | Hanwha Q CELLS (Qidong) HSL72P6-PB-2-285Q | Hanwha Q CELLS (Qidong) HSL72P6-PB-2-285QB | Hanwha Q CELLS (Qidong) HSL72P6-PB-2-285QW | Hanwha Q CELLS (Qidong) HSL72P6-PB-3-285Q | Hanwha Q CELLS (Qidong) HSL72P6-PB-3-285QB | Hanwha Q CELLS (Qidong) HSL72P6-PB-3-285QW | Hanwha Q CELLS (Qidong) HSL72P6-PB-4-285Q | Hanwha Q CELLS (Qidong) HSL72P6-PB-4-285QB | Hanwha Q CELLS (Qidong) HSL72P6-PB-4-285QW | Hanwha Q CELLS (Qidong) HSL72P6-PB-4-285T | Hanwha Q CELLS (Qidong) HSL72P6-PB-4-285TB | Hanwha Q CELLS (Qidong) HSL72P6-PB-4-285TW | Hanwha Q CELLS (Qidong) HSL72M6-HA-0-290T | Hanwha Q CELLS (Qidong) HSL72M6-HA-0-290TB | Hanwha Q CELLS (Qidong) HSL72M6-HA-0-290TW | Hanwha Q CELLS (Qidong) HSL72M6-HA-4-290T | Hanwha Q CELLS (Qidong) HSL72M6-HA-4-290TB | Hanwha Q CELLS (Qidong) HSL72M6-HA-4-290TW | Hanwha Q CELLS (Qidong) HSL72M6-HB-0-290T | Hanwha Q CELLS (Qidong) HSL72M6-HB-0-290TB | Hanwha Q CELLS (Qidong) HSL72M6-HB-0-290TW | Hanwha Q CELLS (Qidong) HSL72M6-HB-4-290T | Hanwha Q CELLS (Qidong) HSL72M6-HB-4-290TB | Hanwha Q CELLS (Qidong) HSL72M6-HB-4-290TW | Hanwha Q CELLS (Qidong) HSL72P6-PA-0-290T | Hanwha Q CELLS (Qidong) HSL72P6-PA-0-290TB | Hanwha Q CELLS (Qidong) HSL72P6-PA-0-290TW | Hanwha Q CELLS (Qidong) HSL72P6-PA-2-290QB | Hanwha Q CELLS (Qidong) HSL72P6-PA-3-290Q | Hanwha Q CELLS (Qidong) HSL72P6-PA-3-290QW | Hanwha Q CELLS (Qidong) HSL72P6-PA-4-290Q | Hanwha Q CELLS (Qidong) HSL72P6-PA-4-290QB | Hanwha Q CELLS (Qidong) HSL72P6-PA-4-290QW | Hanwha Q CELLS (Qidong) HSL72P6-PA-4-290T | Hanwha Q CELLS (Qidong) HSL72P6-PA-4-290TB | Hanwha Q CELLS (Qidong) HSL72P6-PA-4-290TW | Hanwha Q CELLS (Qidong) HSL72P6-PB-0-290T | Hanwha Q CELLS (Qidong) HSL72P6-PB-0-290TB | Hanwha Q CELLS (Qidong) HSL72P6-PB-0-290TW | Hanwha Q CELLS (Qidong) HSL72P6-PB-2-290Q | Hanwha Q CELLS (Qidong) HSL72P6-PB-2-290QB | Hanwha Q CELLS (Qidong) HSL72P6-PB-2-290QW | Hanwha Q CELLS (Qidong) HSL72P6-PB-3-290Q | Hanwha Q CELLS (Qidong) HSL72P6-PB-3-290QB | Hanwha Q CELLS (Qidong) HSL72P6-PB-3-290QW | Hanwha Q CELLS (Qidong) HSL72P6-PB-4-290Q | Hanwha Q CELLS (Qidong) HSL72P6-PB-4-290QB | Hanwha Q CELLS (Qidong) HSL72P6-PB-4-290QW | Hanwha Q CELLS (Qidong) HSL72P6-PB-4-290T | Hanwha Q CELLS (Qidong) HSL72P6-PB-4-290TB | Hanwha Q CELLS (Qidong) HSL72P6-PB-4-290TW | Hanwha Q CELLS (Qidong) HSL72P6-PC-3-290 | Hanwha Q CELLS (Qidong) HSL72P6-PC-3-290W | Hanwha Q CELLS (Qidong) HSL72M6-HA-0-295T | Hanwha Q CELLS (Qidong) HSL72M6-HA-0-295TB | Hanwha Q CELLS (Qidong) HSL72M6-HA-0-295TW | Hanwha Q CELLS (Qidong) HSL72M6-HA-4-295T | Hanwha Q CELLS (Qidong) HSL72M6-HA-4-295TB | Hanwha Q CELLS (Qidong) HSL72M6-HA-4-295TW | Hanwha Q CELLS (Qidong) HSL72M6-HB-0-295T | Hanwha Q CELLS (Qidong) HSL72M6-HB-0-295TB | Hanwha Q CELLS (Qidong) HSL72M6-HB-0-295TW | Hanwha Q CELLS (Qidong) HSL72M6-HB-4-295T | Hanwha Q CELLS (Qidong) HSL72M6-HB-4-295TB | Hanwha Q CELLS (Qidong) HSL72M6-HB-4-295TW | Hanwha Q CELLS (Qidong) HSL72P6-PA-0-295T | Hanwha Q CELLS (Qidong) HSL72P6-PA-0-295TB | Hanwha Q CELLS (Qidong) HSL72P6-PA-0-295TW | Hanwha Q CELLS (Qidong) HSL72P6-PA-2-295Q | Hanwha Q CELLS (Qidong) HSL72P6-PA-2-295QB | Hanwha Q CELLS (Qidong) HSL72P6-PA-2-295QW | Hanwha Q CELLS (Qidong) HSL72P6-PA-3-295Q | Hanwha Q CELLS (Qidong) HSL72P6-PA-3-295QB | Hanwha Q CELLS (Qidong) HSL72P6-PA-3-295QW | Hanwha Q CELLS (Qidong) HSL72P6-PA-4-295Q | Hanwha Q CELLS (Qidong) HSL72P6-PA-4-295QB | Hanwha Q CELLS (Qidong) HSL72P6-PA-4-295QW | Hanwha Q CELLS (Qidong) HSL72P6-PA-4-295T | Hanwha Q CELLS (Qidong) HSL72P6-PA-4-295TB | Hanwha Q CELLS (Qidong) HSL72P6-PA-4-295TW | Hanwha Q CELLS (Qidong) HSL72P6-PB-0-295T | Hanwha Q CELLS (Qidong) HSL72P6-PB-0-295TB | Hanwha Q CELLS (Qidong) HSL72P6-PB-0-295TW | Hanwha Q CELLS (Qidong) HSL72P6-PB-2-295Q | Hanwha Q CELLS (Qidong) HSL72P6-PB-2-295QB | Hanwha Q CELLS (Qidong) HSL72P6-PB-2-295QW | Hanwha Q CELLS (Qidong) HSL72P6-PB-3-295Q | Hanwha Q CELLS (Qidong) HSL72P6-PB-3-295QB | Hanwha Q CELLS (Qidong) HSL72P6-PB-3-295QW | Hanwha Q CELLS (Qidong) HSL72P6-PB-4-295 | Hanwha Q CELLS (Qidong) HSL72P6-PB-4-295Q | Hanwha Q CELLS (Qidong) HSL72P6-PB-4-295QB | Hanwha Q CELLS (Qidong) HSL72P6-PB-4-295QW | Hanwha Q CELLS (Qidong) HSL72P6-PB-4-295T | Hanwha Q CELLS (Qidong) HSL72P6-PB-4-295TB | Hanwha Q CELLS (Qidong) HSL72P6-PB-4-295TW | Hanwha Q CELLS (Qidong) HSL72P6-PB-4-295W | Hanwha Q CELLS (Qidong) HSL72P6-PC-3-295 | Hanwha Q CELLS (Qidong) HSL72P6-PC-3-295Q | Hanwha Q CELLS (Qidong) HSL72P6-PC-3-295QW | Hanwha Q CELLS (Qidong) HSL72P6-PC-3-295W | Hanwha Q CELLS (Qidong) HSL72M6-HA-0-300T | Hanwha Q CELLS (Qidong) HSL72M6-HA-0-300TB | Hanwha Q CELLS (Qidong) HSL72M6-HA-0-300TW | Hanwha Q CELLS (Qidong) HSL72M6-HA-4-300T | Hanwha Q CELLS (Qidong) HSL72M6-HA-4-300TB | Hanwha Q CELLS (Qidong) HSL72M6-HA-4-300TW | Hanwha Q CELLS (Qidong) HSL72M6-HB-0-300T | Hanwha Q CELLS (Qidong) HSL72M6-HB-0-300TB | Hanwha Q CELLS (Qidong) HSL72M6-HB-0-300TW | Hanwha Q CELLS (Qidong) HSL72M6-HB-4-300T | Hanwha Q CELLS (Qidong) HSL72M6-HB-4-300TB | Hanwha Q CELLS (Qidong) HSL72M6-HB-4-300TW | Hanwha Q CELLS (Qidong) HSL72P6-PA-0-300T | Hanwha Q CELLS (Qidong) HSL72P6-PA-0-300TW | Hanwha Q CELLS (Qidong) HSL72P6-PA-2-300Q | Hanwha Q CELLS (Qidong) HSL72P6-PA-2-300QB | Hanwha Q CELLS (Qidong) HSL72P6-PA-2-300QW | Hanwha Q CELLS (Qidong) HSL72P6-PA-3-300Q | Hanwha Q CELLS (Qidong) HSL72P6-PA-3-300QB | Hanwha Q CELLS (Qidong) HSL72P6-PA-3-300QW | Hanwha Q CELLS (Qidong) HSL72P6-PA-4-300Q | Hanwha Q CELLS (Qidong) HSL72P6-PA-4-300QB | Hanwha Q CELLS (Qidong) HSL72P6-PA-4-300QW | Hanwha Q CELLS (Qidong) HSL72P6-PA-4-300T | Hanwha Q CELLS (Qidong) HSL72P6-PA-4-300TW | Hanwha Q CELLS (Qidong) HSL72P6-PB-0-300T | Hanwha Q CELLS (Qidong) HSL72P6-PB-0-300TW | Hanwha Q CELLS (Qidong) HSL72P6-PB-2-300Q | Hanwha Q CELLS (Qidong) HSL72P6-PB-2-300QB | Hanwha Q CELLS (Qidong) HSL72P6-PB-2-300QW | Hanwha Q CELLS (Qidong) HSL72P6-PB-3-300Q | Hanwha Q CELLS (Qidong) HSL72P6-PB-3-300QB | Hanwha Q CELLS (Qidong) HSL72P6-PB-3-300QW | Hanwha Q CELLS (Qidong) HSL72P6-PB-4-300 | Hanwha Q CELLS (Qidong) HSL72P6-PB-4-300Q | Hanwha Q CELLS (Qidong) HSL72P6-PB-4-300QB | Hanwha Q CELLS (Qidong) HSL72P6-PB-4-300QW | Hanwha Q CELLS (Qidong) HSL72P6-PB-4-300T | Hanwha Q CELLS (Qidong) HSL72P6-PB-4-300TW | Hanwha Q CELLS (Qidong) HSL72P6-PB-4-300W | Hanwha Q CELLS (Qidong) HSL72P6-PC-3-300 | Hanwha Q CELLS (Qidong) HSL72P6-PC-3-300Q | Hanwha Q CELLS (Qidong) HSL72P6-PC-3-300QW | Hanwha Q CELLS (Qidong) HSL72P6-PC-3-300W | Hanwha Q CELLS (Qidong) HSL72M6-HA-0-305T | Hanwha Q CELLS (Qidong) HSL72M6-HA-0-305TB | Hanwha Q CELLS (Qidong) HSL72M6-HA-0-305TW | Hanwha Q CELLS (Qidong) HSL72M6-HA-4-305T | Hanwha Q CELLS (Qidong) HSL72M6-HA-4-305TB | Hanwha Q CELLS (Qidong) HSL72M6-HA-4-305TW | Hanwha Q CELLS (Qidong) HSL72M6-HB-0-305T | Hanwha Q CELLS (Qidong) HSL72M6-HB-0-305TB | Hanwha Q CELLS (Qidong) HSL72M6-HB-0-305TW | Hanwha Q CELLS (Qidong) HSL72M6-HB-4-305T | Hanwha Q CELLS (Qidong) HSL72M6-HB-4-305TB | Hanwha Q CELLS (Qidong) HSL72M6-HB-4-305TW | Hanwha Q CELLS (Qidong) HSL72P6-PA-0-305T | Hanwha Q CELLS (Qidong) HSL72P6-PA-0-305TB | Hanwha Q CELLS (Qidong) HSL72P6-PA-0-305TW | Hanwha Q CELLS (Qidong) HSL72P6-PA-2-305Q | Hanwha Q CELLS (Qidong) HSL72P6-PA-2-305QB | Hanwha Q CELLS (Qidong) HSL72P6-PA-2-305QW | Hanwha Q CELLS (Qidong) HSL72P6-PA-3-305Q | Hanwha Q CELLS (Qidong) HSL72P6-PA-3-305QB | Hanwha Q CELLS (Qidong) HSL72P6-PA-3-305QW | Hanwha Q CELLS (Qidong) HSL72P6-PA-4-305Q | Hanwha Q CELLS (Qidong) HSL72P6-PA-4-305QB | Hanwha Q CELLS (Qidong) HSL72P6-PA-4-305QW | Hanwha Q CELLS (Qidong) HSL72P6-PA-4-305T | Hanwha Q CELLS (Qidong) HSL72P6-PA-4-305TB | Hanwha Q CELLS (Qidong) HSL72P6-PA-4-305TW | Hanwha Q CELLS (Qidong) HSL72P6-PB-0-305T | Hanwha Q CELLS (Qidong) HSL72P6-PB-0-305TB | Hanwha Q CELLS (Qidong) HSL72P6-PB-0-305TW | Hanwha Q CELLS (Qidong) HSL72P6-PB-2-305Q | Hanwha Q CELLS (Qidong) HSL72P6-PB-2-305QB | Hanwha Q CELLS (Qidong) HSL72P6-PB-2-305QW | Hanwha Q CELLS (Qidong) HSL72P6-PB-3-305Q | Hanwha Q CELLS (Qidong) HSL72P6-PB-3-305QB | Hanwha Q CELLS (Qidong) HSL72P6-PB-3-305QW | Hanwha Q CELLS (Qidong) HSL72P6-PB-4-305 | Hanwha Q CELLS (Qidong) HSL72P6-PB-4-305Q | Hanwha Q CELLS (Qidong) HSL72P6-PB-4-305QB | Hanwha Q CELLS (Qidong) HSL72P6-PB-4-305QW | Hanwha Q CELLS (Qidong) HSL72P6-PB-4-305T | Hanwha Q CELLS (Qidong) HSL72P6-PB-4-305TB | Hanwha Q CELLS (Qidong) HSL72P6-PB-4-305TW | Hanwha Q CELLS (Qidong) HSL72P6-PB-4-305W | Hanwha Q CELLS (Qidong) HSL72P6-PC-3-305 | Hanwha Q CELLS (Qidong) HSL72P6-PC-3-305Q | Hanwha Q CELLS (Qidong) HSL72P6-PC-3-305QW | Hanwha Q CELLS (Qidong) HSL72P6-PC-3-305W | Hanwha Q CELLS (Qidong) HSL72M6-HA-0-310T | Hanwha Q CELLS (Qidong) HSL72M6-HA-0-310TB | Hanwha Q CELLS (Qidong) HSL72M6-HA-0-310TW | Hanwha Q CELLS (Qidong) HSL72M6-HA-4-310T | Hanwha Q CELLS (Qidong) HSL72M6-HA-4-310TB | Hanwha Q CELLS (Qidong) HSL72M6-HA-4-310TW | Hanwha Q CELLS (Qidong) HSL72M6-HB-0-310T | Hanwha Q CELLS (Qidong) HSL72M6-HB-0-310TB | Hanwha Q CELLS (Qidong) HSL72M6-HB-0-310TW | Hanwha Q CELLS (Qidong) HSL72M6-HB-4-310T | Hanwha Q CELLS (Qidong) HSL72M6-HB-4-310TB | Hanwha Q CELLS (Qidong) HSL72M6-HB-4-310TW | Hanwha Q CELLS (Qidong) HSL72P6-PB-0-310T | Hanwha Q CELLS (Qidong) HSL72P6-PB-0-310TW | Hanwha Q CELLS (Qidong) HSL72P6-PB-4-310 | Hanwha Q CELLS (Qidong) HSL72P6-PB-4-310T | Hanwha Q CELLS (Qidong) HSL72P6-PB-4-310TW | Hanwha Q CELLS (Qidong) HSL72P6-PB-4-310W | Hanwha Q CELLS (Qidong) HSL72P6-PC-3-310 | Hanwha Q CELLS (Qidong) HSL72P6-PC-3-310Q | Hanwha Q CELLS (Qidong) HSL72P6-PC-3-310QW | Hanwha Q CELLS (Qidong) HSL72P6-PC-3-310W | Hanwha Q CELLS (Qidong) HSL72P6-PB-0-315T | Hanwha Q CELLS (Qidong) HSL72P6-PB-0-315TW | Hanwha Q CELLS (Qidong) HSL72P6-PB-4-315T | Hanwha Q CELLS (Qidong) HSL72P6-PB-4-315TW | Hanwha Q CELLS (Qidong) HSL72P6-PC-3-315 | Hanwha Q CELLS (Qidong) HSL72P6-PC-3-315Q | Hanwha Q CELLS (Qidong) HSL72P6-PC-3-315QW | Hanwha Q CELLS (Qidong) HSL72P6-PC-3-320 | Hanwha Q CELLS (Qidong) HSL72P6-PC-3-325 | Hanwha Q CELLS (Qidong) HSL72P6-PC-3-330 | Hanwha Q CELLS (Qidong) Co._ Ltd. Q.PRIME L-G5.1.G 330 | Hanwha Q CELLS (Qidong) Co._ Ltd. Q.PRIME L-G5.2.G 330 | Hanwha Q CELLS (Qidong) Co._ Ltd. Q.PRIME L-G5.1.G 335 | Hanwha Q CELLS (Qidong) Co._ Ltd. Q.PRIME L-G5.2.G 335 | Hanwha Q CELLS (Qidong) Co._ Ltd. Q.PRIME L-G5.1.G 340 | Hanwha Q CELLS (Qidong) Co._ Ltd. Q.PRIME L-G5.2.G 340 | Hanwha Q CELLS (Qidong) Co._ Ltd. Q.PRIME L-G5.1.G 345 | Hanwha Q CELLS (Qidong) Co._ Ltd. Q.PRIME L-G5.2.G 345 | Hanwha Solar Canada HSC60PA-D-S-240 | Hanwha Solar Canada HSC60PA-x-S-245 | Hanwha Solar Canada HSC60PA-x-S-250 | Hanwha Solar Canada HSC60PA-x-S-255 | Hanwha Solar Canada HSC60MA-G-S-260 | Hanwha Solar Canada HSC60MA-S-S-260 | Hanwha Solar Canada HSC60PA-x-S-260 | Hanwha Solar Canada HSC60MA-G-S-265 | Hanwha Solar Canada HSC60MA-S-S-265 | Hanwha Solar Canada HSC60PA-x-S-265 | Hanwha Solar Canada HSC60MA-G-S-270 | Hanwha Solar Canada HSC60MA-S-S-270 | Hanwha Solar Canada HSC60MA-G-S-275 | Hanwha Solar Canada HSC60MA-S-S-275 | Hanwha Solar Canada HSC60MA-G-S-280 | Hanwha Solar Canada HSC60MA-S-S-280 | Hanwha Solar Canada HSC60MA-G-S-285 | Hanwha Solar Canada HSC60MA-S-S-285 | Hanwha Solar Canada HSC72PA-x-S-290 | Hanwha Solar Canada HSC72PA-x-S-295 | Hanwha Solar Canada HSC72PA-x-S-300 | Hanwha Solar Canada HSC72PA-x-S-305 | Hanwha Solar Canada HSC72PA-x-S-310 | Hanwha Solar Canada HSC72MA-G-S-315 | Hanwha Solar Canada HSC72MA-S-S-315 | Hanwha Solar Canada HSC72PA-x-S-315 | Hanwha Solar Canada HSC72MA-G-S-320 | Hanwha Solar Canada HSC72MA-S-S-320 | Hanwha Solar Canada HSC72PA-x-S-320 | Hanwha Solar Canada HSC72MA-G-S-325 | Hanwha Solar Canada HSC72MA-S-S-325 | Hanwha Solar Canada HSC72MA-G-S-330 | Hanwha Solar Canada HSC72MA-S-S-330 | Hanwha Solar Canada HSC72MA-G-S-335 | Hanwha Solar Canada HSC72MA-S-S-335 | Hanwha SolarOne (Qidong) SF160-24-M150 | Hanwha SolarOne (Qidong) SF160-24-M155 | Hanwha SolarOne (Qidong) SF160-24-M160 | Hanwha SolarOne (Qidong) SF160-24-M160B | Hanwha SolarOne (Qidong) SF160-24-M165 | Hanwha SolarOne (Qidong) SF160-24-M165B | Hanwha SolarOne (Qidong) SF160-24-P165 | Hanwha SolarOne (Qidong) SF160-24-M170 | Hanwha SolarOne (Qidong) SF160-24-M170B | Hanwha SolarOne (Qidong) SF160-24-P170 | Hanwha SolarOne (Qidong) SF190-27-P170 | Hanwha SolarOne (Qidong) SF160-24-M175 | Hanwha SolarOne (Qidong) SF160-24-M175B | Hanwha SolarOne (Qidong) SF160-24-M175L | Hanwha SolarOne (Qidong) SF160-24-M175L-B | Hanwha SolarOne (Qidong) SF160-24-P175 | Hanwha SolarOne (Qidong) SF190-27-P175 | Hanwha SolarOne (Qidong) SF160-24-M180 | Hanwha SolarOne (Qidong) SF160-24-M180B | Hanwha SolarOne (Qidong) SF160-24-M180L | Hanwha SolarOne (Qidong) SF160-24-M180L-B | Hanwha SolarOne (Qidong) SF190-27-M180 | Hanwha SolarOne (Qidong) SF190-27-M180B | Hanwha SolarOne (Qidong) SF190-27-P180 | Hanwha SolarOne (Qidong) SF160-24-M185 | Hanwha SolarOne (Qidong) SF160-24-M185B | Hanwha SolarOne (Qidong) SF160-24-M185L | Hanwha SolarOne (Qidong) SF160-24-M185L-B | Hanwha SolarOne (Qidong) SF190-27-M185 | Hanwha SolarOne (Qidong) SF190-27-M185B | Hanwha SolarOne (Qidong) SF190-27-P185 | Hanwha SolarOne (Qidong) SF160-24-M190 | Hanwha SolarOne (Qidong) SF160-24-M190B | Hanwha SolarOne (Qidong) SF160-24-M190L | Hanwha SolarOne (Qidong) SF160-24-M190L-B | Hanwha SolarOne (Qidong) SF190-27-M190 | Hanwha SolarOne (Qidong) SF190-27-M190B | Hanwha SolarOne (Qidong) SF190-27-P190 | Hanwha SolarOne (Qidong) SF190-27-M195 | Hanwha SolarOne (Qidong) SF190-27-M195B | Hanwha SolarOne (Qidong) SF190-27-P195 | Hanwha SolarOne (Qidong) SF190-27-M200 | Hanwha SolarOne (Qidong) SF190-27-M200B | Hanwha SolarOne (Qidong) SF190-27-P200 | Hanwha SolarOne (Qidong) SF220-30-M200 | Hanwha SolarOne (Qidong) SF220-30-M200B | Hanwha SolarOne (Qidong) SF220-30-P200 | Hanwha SolarOne (Qidong) SF220-30-P200B | Hanwha SolarOne (Qidong) SF190-27-M205 | Hanwha SolarOne (Qidong) SF190-27-M205B | Hanwha SolarOne (Qidong) SF190-27-P205 | Hanwha SolarOne (Qidong) SF220-30-M205 | Hanwha SolarOne (Qidong) SF220-30-M205B | Hanwha SolarOne (Qidong) SF220-30-P205 | Hanwha SolarOne (Qidong) SF220-30-P205B | Hanwha SolarOne (Qidong) SF190-27-M210 | Hanwha SolarOne (Qidong) SF190-27-M210B | Hanwha SolarOne (Qidong) SF190-27-P210 | Hanwha SolarOne (Qidong) SF220-30-M210 | Hanwha SolarOne (Qidong) SF220-30-M210B | Hanwha SolarOne (Qidong) SF220-30-P210 | Hanwha SolarOne (Qidong) SF220-30-P210B | Hanwha SolarOne (Qidong) SF220-30-M215 | Hanwha SolarOne (Qidong) SF220-30-M215B | Hanwha SolarOne (Qidong) SF220-30-P215 | Hanwha SolarOne (Qidong) SF220-30-P215B | Hanwha SolarOne (Qidong) SF220-30-M220 | Hanwha SolarOne (Qidong) SF220-30-M220B | Hanwha SolarOne (Qidong) SF220-30-P220 | Hanwha SolarOne (Qidong) SF220-30-P220B | Hanwha SolarOne (Qidong) SF220-30-M225 | Hanwha SolarOne (Qidong) SF220-30-M225B | Hanwha SolarOne (Qidong) SF220-30-P225 | Hanwha SolarOne (Qidong) SF220-30-P225B | Hanwha SolarOne (Qidong) HSL60P6-PA-3-230Q | Hanwha SolarOne (Qidong) HSL60P6-PA-3-230QB | Hanwha SolarOne (Qidong) HSL60P6-PA-3-230QW | Hanwha SolarOne (Qidong) HSL60P6-PB-3-230Q | Hanwha SolarOne (Qidong) HSL60P6-PB-3-230QB | Hanwha SolarOne (Qidong) HSL60P6-PB-3-230QW | Hanwha SolarOne (Qidong) SF220-30-M230 | Hanwha SolarOne (Qidong) SF220-30-M230B | Hanwha SolarOne (Qidong) SF220-30-M230L | Hanwha SolarOne (Qidong) SF220-30-P230 | Hanwha SolarOne (Qidong) SF220-30-P230B | Hanwha SolarOne (Qidong) SF220-30-P230L | Hanwha SolarOne (Qidong) SF220-30-P230L-B | Hanwha SolarOne (Qidong) HSL60P6-PA-0-235T | Hanwha SolarOne (Qidong) HSL60P6-PA-0-235TB | Hanwha SolarOne (Qidong) HSL60P6-PA-0-235TW | Hanwha SolarOne (Qidong) HSL60P6-PA-2-235Q | Hanwha SolarOne (Qidong) HSL60P6-PA-2-235QB | Hanwha SolarOne (Qidong) HSL60P6-PA-2-235QW | Hanwha SolarOne (Qidong) HSL60P6-PA-3-235Q | Hanwha SolarOne (Qidong) HSL60P6-PA-3-235QB | Hanwha SolarOne (Qidong) HSL60P6-PA-3-235QW | Hanwha SolarOne (Qidong) HSL60P6-PA-4-235Q | Hanwha SolarOne (Qidong) HSL60P6-PA-4-235QB | Hanwha SolarOne (Qidong) HSL60P6-PA-4-235QW | Hanwha SolarOne (Qidong) HSL60P6-PA-4-235T | Hanwha SolarOne (Qidong) HSL60P6-PA-4-235TB | Hanwha SolarOne (Qidong) HSL60P6-PA-4-235TW | Hanwha SolarOne (Qidong) HSL60P6-PB-2-235Q | Hanwha SolarOne (Qidong) HSL60P6-PB-2-235QB | Hanwha SolarOne (Qidong) HSL60P6-PB-2-235QW | Hanwha SolarOne (Qidong) HSL60P6-PB-3-235Q | Hanwha SolarOne (Qidong) HSL60P6-PB-3-235QB | Hanwha SolarOne (Qidong) HSL60P6-PB-3-235QW | Hanwha SolarOne (Qidong) HSL60P6-PB-4-235Q | Hanwha SolarOne (Qidong) HSL60P6-PB-4-235QB | Hanwha SolarOne (Qidong) HSL60P6-PB-4-235QW | Hanwha SolarOne (Qidong) SF220-30-M235 | Hanwha SolarOne (Qidong) SF220-30-M235B | Hanwha SolarOne (Qidong) SF220-30-M235L | Hanwha SolarOne (Qidong) SF220-30-P235 | Hanwha SolarOne (Qidong) SF220-30-P235B | Hanwha SolarOne (Qidong) SF220-30-P235L | Hanwha SolarOne (Qidong) SF220-30-P235L-B | Hanwha SolarOne (Qidong) HSL60M6-HA-0-240T | Hanwha SolarOne (Qidong) HSL60M6-HA-0-240TW | Hanwha SolarOne (Qidong) HSL60M6-HA-4-240T | Hanwha SolarOne (Qidong) HSL60M6-HA-4-240TB | Hanwha SolarOne (Qidong) HSL60M6-HA-4-240TW | Hanwha SolarOne (Qidong) HSL60M6-HB-0-240T | Hanwha SolarOne (Qidong) HSL60M6-HB-0-240TB | Hanwha SolarOne (Qidong) HSL60M6-HB-0-240TW | Hanwha SolarOne (Qidong) HSL60M6-HB-4-240T | Hanwha SolarOne (Qidong) HSL60M6-HB-4-240TB | Hanwha SolarOne (Qidong) HSL60M6-HB-4-240TW | Hanwha SolarOne (Qidong) HSL60P6-PA-0-240T | Hanwha SolarOne (Qidong) HSL60P6-PA-0-240TB | Hanwha SolarOne (Qidong) HSL60P6-PA-0-240TW | Hanwha SolarOne (Qidong) HSL60P6-PA-2-240Q | Hanwha SolarOne (Qidong) HSL60P6-PA-2-240QB | Hanwha SolarOne (Qidong) HSL60P6-PA-2-240QW | Hanwha SolarOne (Qidong) HSL60P6-PA-3-240Q | Hanwha SolarOne (Qidong) HSL60P6-PA-3-240QB | Hanwha SolarOne (Qidong) HSL60P6-PA-3-240QW | Hanwha SolarOne (Qidong) HSL60P6-PA-4-240Q | Hanwha SolarOne (Qidong) HSL60P6-PA-4-240QB | Hanwha SolarOne (Qidong) HSL60P6-PA-4-240QW | Hanwha SolarOne (Qidong) HSL60P6-PA-4-240T | Hanwha SolarOne (Qidong) HSL60P6-PA-4-240TB | Hanwha SolarOne (Qidong) HSL60P6-PA-4-240TW | Hanwha SolarOne (Qidong) HSL60P6-PB-0-240T | Hanwha SolarOne (Qidong) HSL60P6-PB-0-240TB | Hanwha SolarOne (Qidong) HSL60P6-PB-0-240TW | Hanwha SolarOne (Qidong) HSL60P6-PB-2-240Q | Hanwha SolarOne (Qidong) HSL60P6-PB-2-240QB | Hanwha SolarOne (Qidong) HSL60P6-PB-2-240QW | Hanwha SolarOne (Qidong) HSL60P6-PB-3-240QB | Hanwha SolarOne (Qidong) HSL60P6-PB-4-240Q | Hanwha SolarOne (Qidong) HSL60P6-PB-4-240QW | Hanwha SolarOne (Qidong) HSL60P6-PB-4-240T | Hanwha SolarOne (Qidong) HSL60P6-PB-4-240TB | Hanwha SolarOne (Qidong) HSL60P6-PB-4-240TW | Hanwha SolarOne (Qidong) SF220-30-M240 | Hanwha SolarOne (Qidong) SF220-30-M240B | Hanwha SolarOne (Qidong) SF220-30-M240L | Hanwha SolarOne (Qidong) SF220-30-P240 | Hanwha SolarOne (Qidong) SF220-30-P240B | Hanwha SolarOne (Qidong) SF220-30-P240L | Hanwha SolarOne (Qidong) SF220-30-P240L-B | Hanwha SolarOne (Qidong) HSL60M6-HA-0-245T | Hanwha SolarOne (Qidong) HSL60M6-HA-0-245TW | Hanwha SolarOne (Qidong) HSL60M6-HA-4-245T | Hanwha SolarOne (Qidong) HSL60M6-HA-4-245TB | Hanwha SolarOne (Qidong) HSL60M6-HA-4-245TW | Hanwha SolarOne (Qidong) HSL60M6-HB-0-245T | Hanwha SolarOne (Qidong) HSL60M6-HB-0-245TB | Hanwha SolarOne (Qidong) HSL60M6-HB-0-245TW | Hanwha SolarOne (Qidong) HSL60M6-HB-4-245T | Hanwha SolarOne (Qidong) HSL60M6-HB-4-245TB | Hanwha SolarOne (Qidong) HSL60M6-HB-4-245TW | Hanwha SolarOne (Qidong) HSL60P6-PA-0-245T | Hanwha SolarOne (Qidong) HSL60P6-PA-0-245TB | Hanwha SolarOne (Qidong) HSL60P6-PA-0-245TW | Hanwha SolarOne (Qidong) HSL60P6-PA-2-245Q | Hanwha SolarOne (Qidong) HSL60P6-PA-2-245QB | Hanwha SolarOne (Qidong) HSL60P6-PA-2-245QW | Hanwha SolarOne (Qidong) HSL60P6-PA-3-245Q | Hanwha SolarOne (Qidong) HSL60P6-PA-3-245QB | Hanwha SolarOne (Qidong) HSL60P6-PA-3-245QW | Hanwha SolarOne (Qidong) HSL60P6-PA-4-245Q | Hanwha SolarOne (Qidong) HSL60P6-PA-4-245QB | Hanwha SolarOne (Qidong) HSL60P6-PA-4-245QW | Hanwha SolarOne (Qidong) HSL60P6-PA-4-245T | Hanwha SolarOne (Qidong) HSL60P6-PA-4-245TB | Hanwha SolarOne (Qidong) HSL60P6-PA-4-245TW | Hanwha SolarOne (Qidong) HSL60P6-PB-0-245T | Hanwha SolarOne (Qidong) HSL60P6-PB-0-245TB | Hanwha SolarOne (Qidong) HSL60P6-PB-0-245TW | Hanwha SolarOne (Qidong) HSL60P6-PB-2-245Q | Hanwha SolarOne (Qidong) HSL60P6-PB-2-245QB | Hanwha SolarOne (Qidong) HSL60P6-PB-2-245QW | Hanwha SolarOne (Qidong) HSL60P6-PB-3-245Q | Hanwha SolarOne (Qidong) HSL60P6-PB-3-245QB | Hanwha SolarOne (Qidong) HSL60P6-PB-3-245QW | Hanwha SolarOne (Qidong) HSL60P6-PB-4-245 | Hanwha SolarOne (Qidong) HSL60P6-PB-4-245Q | Hanwha SolarOne (Qidong) HSL60P6-PB-4-245QB | Hanwha SolarOne (Qidong) HSL60P6-PB-4-245QW | Hanwha SolarOne (Qidong) HSL60P6-PB-4-245T | Hanwha SolarOne (Qidong) HSL60P6-PB-4-245TB | Hanwha SolarOne (Qidong) HSL60P6-PB-4-245TW | Hanwha SolarOne (Qidong) HSL60P6-PB-4-245W | Hanwha SolarOne (Qidong) SF220-30-M245 | Hanwha SolarOne (Qidong) SF220-30-M245B | Hanwha SolarOne (Qidong) SF220-30-M245L | Hanwha SolarOne (Qidong) SF220-30-P245 | Hanwha SolarOne (Qidong) SF220-30-P245B | Hanwha SolarOne (Qidong) SF220-30-P245L | Hanwha SolarOne (Qidong) SF220-30-P245L-B | Hanwha SolarOne (Qidong) HSL60M6-HA-0-250T | Hanwha SolarOne (Qidong) HSL60M6-HA-0-250TW | Hanwha SolarOne (Qidong) HSL60M6-HA-4-250T | Hanwha SolarOne (Qidong) HSL60M6-HA-4-250TB | Hanwha SolarOne (Qidong) HSL60M6-HA-4-250TW | Hanwha SolarOne (Qidong) HSL60M6-HB-0-250T | Hanwha SolarOne (Qidong) HSL60M6-HB-0-250TB | Hanwha SolarOne (Qidong) HSL60M6-HB-0-250TW | Hanwha SolarOne (Qidong) HSL60M6-HB-4-250T | Hanwha SolarOne (Qidong) HSL60M6-HB-4-250TB | Hanwha SolarOne (Qidong) HSL60M6-HB-4-250TW | Hanwha SolarOne (Qidong) HSL60P6-PA-0-250T | Hanwha SolarOne (Qidong) HSL60P6-PA-0-250TB | Hanwha SolarOne (Qidong) HSL60P6-PA-0-250TW | Hanwha SolarOne (Qidong) HSL60P6-PA-2-250Q | Hanwha SolarOne (Qidong) HSL60P6-PA-2-250QB | Hanwha SolarOne (Qidong) HSL60P6-PA-2-250QW | Hanwha SolarOne (Qidong) HSL60P6-PA-3-250Q | Hanwha SolarOne (Qidong) HSL60P6-PA-3-250QB | Hanwha SolarOne (Qidong) HSL60P6-PA-3-250QW | Hanwha SolarOne (Qidong) HSL60P6-PA-4-250Q | Hanwha SolarOne (Qidong) HSL60P6-PA-4-250QB | Hanwha SolarOne (Qidong) HSL60P6-PA-4-250QW | Hanwha SolarOne (Qidong) HSL60P6-PA-4-250T | Hanwha SolarOne (Qidong) HSL60P6-PA-4-250TB | Hanwha SolarOne (Qidong) HSL60P6-PA-4-250TW | Hanwha SolarOne (Qidong) HSL60P6-PB-0-250T | Hanwha SolarOne (Qidong) HSL60P6-PB-0-250TB | Hanwha SolarOne (Qidong) HSL60P6-PB-0-250TW | Hanwha SolarOne (Qidong) HSL60P6-PB-2-250Q | Hanwha SolarOne (Qidong) HSL60P6-PB-2-250QB | Hanwha SolarOne (Qidong) HSL60P6-PB-2-250QW | Hanwha SolarOne (Qidong) HSL60P6-PB-3-250Q | Hanwha SolarOne (Qidong) HSL60P6-PB-3-250QB | Hanwha SolarOne (Qidong) HSL60P6-PB-3-250QW | Hanwha SolarOne (Qidong) HSL60P6-PB-4-250 | Hanwha SolarOne (Qidong) HSL60P6-PB-4-250Q | Hanwha SolarOne (Qidong) HSL60P6-PB-4-250QB | Hanwha SolarOne (Qidong) HSL60P6-PB-4-250QW | Hanwha SolarOne (Qidong) HSL60P6-PB-4-250T | Hanwha SolarOne (Qidong) HSL60P6-PB-4-250TB | Hanwha SolarOne (Qidong) HSL60P6-PB-4-250TW | Hanwha SolarOne (Qidong) HSL60P6-PB-4-250W | Hanwha SolarOne (Qidong) HSL60P6-PC-3-250 | Hanwha SolarOne (Qidong) HSL60P6-PC-3-250W | Hanwha SolarOne (Qidong) HSL60M6-HA-0-255T | Hanwha SolarOne (Qidong) HSL60M6-HA-0-255TW | Hanwha SolarOne (Qidong) HSL60M6-HA-4-255T | Hanwha SolarOne (Qidong) HSL60M6-HA-4-255TB | Hanwha SolarOne (Qidong) HSL60M6-HA-4-255TW | Hanwha SolarOne (Qidong) HSL60M6-HB-0-255T | Hanwha SolarOne (Qidong) HSL60M6-HB-0-255TB | Hanwha SolarOne (Qidong) HSL60M6-HB-0-255TW | Hanwha SolarOne (Qidong) HSL60M6-HB-4-255T | Hanwha SolarOne (Qidong) HSL60M6-HB-4-255TB | Hanwha SolarOne (Qidong) HSL60M6-HB-4-255TW | Hanwha SolarOne (Qidong) HSL60P6-PA-0-255T | Hanwha SolarOne (Qidong) HSL60P6-PA-0-255TB | Hanwha SolarOne (Qidong) HSL60P6-PA-0-255TW | Hanwha SolarOne (Qidong) HSL60P6-PA-2-255Q | Hanwha SolarOne (Qidong) HSL60P6-PA-2-255QB | Hanwha SolarOne (Qidong) HSL60P6-PA-2-255QW | Hanwha SolarOne (Qidong) HSL60P6-PA-3-255Q | Hanwha SolarOne (Qidong) HSL60P6-PA-3-255QB | Hanwha SolarOne (Qidong) HSL60P6-PA-3-255QW | Hanwha SolarOne (Qidong) HSL60P6-PA-4-255Q | Hanwha SolarOne (Qidong) HSL60P6-PA-4-255QB | Hanwha SolarOne (Qidong) HSL60P6-PA-4-255QW | Hanwha SolarOne (Qidong) HSL60P6-PA-4-255T | Hanwha SolarOne (Qidong) HSL60P6-PA-4-255TB | Hanwha SolarOne (Qidong) HSL60P6-PA-4-255TW | Hanwha SolarOne (Qidong) HSL60P6-PB-0-255T | Hanwha SolarOne (Qidong) HSL60P6-PB-0-255TB | Hanwha SolarOne (Qidong) HSL60P6-PB-0-255TW | Hanwha SolarOne (Qidong) HSL60P6-PB-2-255Q | Hanwha SolarOne (Qidong) HSL60P6-PB-2-255QB | Hanwha SolarOne (Qidong) HSL60P6-PB-2-255QW | Hanwha SolarOne (Qidong) HSL60P6-PB-3-255Q | Hanwha SolarOne (Qidong) HSL60P6-PB-3-255QB | Hanwha SolarOne (Qidong) HSL60P6-PB-3-255QW | Hanwha SolarOne (Qidong) HSL60P6-PB-4-255 | Hanwha SolarOne (Qidong) HSL60P6-PB-4-255Q | Hanwha SolarOne (Qidong) HSL60P6-PB-4-255QB | Hanwha SolarOne (Qidong) HSL60P6-PB-4-255QW | Hanwha SolarOne (Qidong) HSL60P6-PB-4-255T | Hanwha SolarOne (Qidong) HSL60P6-PB-4-255TB | Hanwha SolarOne (Qidong) HSL60P6-PB-4-255TW | Hanwha SolarOne (Qidong) HSL60P6-PB-4-255W | Hanwha SolarOne (Qidong) HSL60P6-PC-3-255 | Hanwha SolarOne (Qidong) HSL60P6-PC-3-255W | Hanwha SolarOne (Qidong) SF260-36-P255 | Hanwha SolarOne (Qidong) SF260-36-P255B | Hanwha SolarOne (Qidong) HSL60M6-HA-0-260T | Hanwha SolarOne (Qidong) HSL60M6-HA-0-260TW | Hanwha SolarOne (Qidong) HSL60M6-HA-4-260T | Hanwha SolarOne (Qidong) HSL60M6-HA-4-260TB | Hanwha SolarOne (Qidong) HSL60M6-HA-4-260TW | Hanwha SolarOne (Qidong) HSL60M6-HB-0-260T | Hanwha SolarOne (Qidong) HSL60M6-HB-0-260TB | Hanwha SolarOne (Qidong) HSL60M6-HB-0-260TW | Hanwha SolarOne (Qidong) HSL60M6-HB-4-260T | Hanwha SolarOne (Qidong) HSL60M6-HB-4-260TB | Hanwha SolarOne (Qidong) HSL60M6-HB-4-260TW | Hanwha SolarOne (Qidong) HSL60P6-PB-0-260T | Hanwha SolarOne (Qidong) HSL60P6-PB-0-260TW | Hanwha SolarOne (Qidong) HSL60P6-PB-4-260 | Hanwha SolarOne (Qidong) HSL60P6-PB-4-260T | Hanwha SolarOne (Qidong) HSL60P6-PB-4-260TW | Hanwha SolarOne (Qidong) HSL60P6-PB-4-260W | Hanwha SolarOne (Qidong) HSL60P6-PC-3-260 | Hanwha SolarOne (Qidong) HSL60P6-PC-3-260W | Hanwha SolarOne (Qidong) SF260-36-P260 | Hanwha SolarOne (Qidong) SF260-36-P260B | Hanwha SolarOne (Qidong) HSL60P6-PB-0-265T | Hanwha SolarOne (Qidong) HSL60P6-PB-0-265TW | Hanwha SolarOne (Qidong) HSL60P6-PB-4-265T | Hanwha SolarOne (Qidong) HSL60P6-PB-4-265TW | Hanwha SolarOne (Qidong) HSL60P6-PC-3-265 | Hanwha SolarOne (Qidong) HSL60P6-PC-3-265W | Hanwha SolarOne (Qidong) SF260-36-P265 | Hanwha SolarOne (Qidong) SF260-36-P265B | Hanwha SolarOne (Qidong) HSL60P6-PB-0-270T | Hanwha SolarOne (Qidong) HSL60P6-PB-0-270TW | Hanwha SolarOne (Qidong) HSL60P6-PB-4-270T | Hanwha SolarOne (Qidong) HSL60P6-PB-4-270TW | Hanwha SolarOne (Qidong) SF260-36-P270 | Hanwha SolarOne (Qidong) SF260-36-P270B | Hanwha SolarOne (Qidong) SF260-36-P270L | Hanwha SolarOne (Qidong) SF260-36-P270L-B | Hanwha SolarOne (Qidong) HSL72P6-PA-0-275T | Hanwha SolarOne (Qidong) HSL72P6-PA-0-275TB | Hanwha SolarOne (Qidong) HSL72P6-PA-0-275TW | Hanwha SolarOne (Qidong) HSL72P6-PA-4-275T | Hanwha SolarOne (Qidong) HSL72P6-PA-4-275TB | Hanwha SolarOne (Qidong) HSL72P6-PA-4-275TW | Hanwha SolarOne (Qidong) SF260-36-P275 | Hanwha SolarOne (Qidong) SF260-36-P275B | Hanwha SolarOne (Qidong) SF260-36-P275L | Hanwha SolarOne (Qidong) SF260-36-P275L-B | Hanwha SolarOne (Qidong) HSL72P6-PA-0-280T | Hanwha SolarOne (Qidong) HSL72P6-PA-0-280TB | Hanwha SolarOne (Qidong) HSL72P6-PA-0-280TW | Hanwha SolarOne (Qidong) HSL72P6-PA-2-280Q | Hanwha SolarOne (Qidong) HSL72P6-PA-2-280QB | Hanwha SolarOne (Qidong) HSL72P6-PA-2-280QW | Hanwha SolarOne (Qidong) HSL72P6-PA-3-280Q | Hanwha SolarOne (Qidong) HSL72P6-PA-3-280QB | Hanwha SolarOne (Qidong) HSL72P6-PA-3-280QW | Hanwha SolarOne (Qidong) HSL72P6-PA-4-280Q | Hanwha SolarOne (Qidong) HSL72P6-PA-4-280QB | Hanwha SolarOne (Qidong) HSL72P6-PA-4-280QW | Hanwha SolarOne (Qidong) HSL72P6-PA-4-280T | Hanwha SolarOne (Qidong) HSL72P6-PA-4-280TB | Hanwha SolarOne (Qidong) HSL72P6-PA-4-280TW | Hanwha SolarOne (Qidong) HSL72P6-PB-2-280Q | Hanwha SolarOne (Qidong) HSL72P6-PB-2-280QB | Hanwha SolarOne (Qidong) HSL72P6-PB-2-280QW | Hanwha SolarOne (Qidong) HSL72P6-PB-3-280Q | Hanwha SolarOne (Qidong) HSL72P6-PB-3-280QB | Hanwha SolarOne (Qidong) HSL72P6-PB-3-280QW | Hanwha SolarOne (Qidong) HSL72P6-PB-4-280Q | Hanwha SolarOne (Qidong) HSL72P6-PB-4-280QB | Hanwha SolarOne (Qidong) HSL72P6-PB-4-280QW | Hanwha SolarOne (Qidong) SF260-36-P280 | Hanwha SolarOne (Qidong) SF260-36-P280B | Hanwha SolarOne (Qidong) SF260-36-P280L | Hanwha SolarOne (Qidong) SF260-36-P280L-B | Hanwha SolarOne (Qidong) HSL72M6-HA-0-285T | Hanwha SolarOne (Qidong) HSL72M6-HA-0-285TB | Hanwha SolarOne (Qidong) HSL72M6-HA-0-285TW | Hanwha SolarOne (Qidong) HSL72M6-HA-4-285T | Hanwha SolarOne (Qidong) HSL72M6-HA-4-285TB | Hanwha SolarOne (Qidong) HSL72M6-HA-4-285TW | Hanwha SolarOne (Qidong) HSL72M6-HB-0-285T | Hanwha SolarOne (Qidong) HSL72M6-HB-0-285TB | Hanwha SolarOne (Qidong) HSL72M6-HB-0-285TW | Hanwha SolarOne (Qidong) HSL72M6-HB-4-285T | Hanwha SolarOne (Qidong) HSL72M6-HB-4-285TB | Hanwha SolarOne (Qidong) HSL72M6-HB-4-285TW | Hanwha SolarOne (Qidong) HSL72P6-PA-0-285T | Hanwha SolarOne (Qidong) HSL72P6-PA-0-285TB | Hanwha SolarOne (Qidong) HSL72P6-PA-0-285TW | Hanwha SolarOne (Qidong) HSL72P6-PA-2-285Q | Hanwha SolarOne (Qidong) HSL72P6-PA-2-285QB | Hanwha SolarOne (Qidong) HSL72P6-PA-2-285QW | Hanwha SolarOne (Qidong) HSL72P6-PA-3-285Q | Hanwha SolarOne (Qidong) HSL72P6-PA-3-285QB | Hanwha SolarOne (Qidong) HSL72P6-PA-3-285QW | Hanwha SolarOne (Qidong) HSL72P6-PA-4-285Q | Hanwha SolarOne (Qidong) HSL72P6-PA-4-285QB | Hanwha SolarOne (Qidong) HSL72P6-PA-4-285QW | Hanwha SolarOne (Qidong) HSL72P6-PA-4-285T | Hanwha SolarOne (Qidong) HSL72P6-PA-4-285TB | Hanwha SolarOne (Qidong) HSL72P6-PA-4-285TW | Hanwha SolarOne (Qidong) HSL72P6-PB-0-285T | Hanwha SolarOne (Qidong) HSL72P6-PB-0-285TB | Hanwha SolarOne (Qidong) HSL72P6-PB-0-285TW | Hanwha SolarOne (Qidong) HSL72P6-PB-2-285Q | Hanwha SolarOne (Qidong) HSL72P6-PB-2-285QB | Hanwha SolarOne (Qidong) HSL72P6-PB-2-285QW | Hanwha SolarOne (Qidong) HSL72P6-PB-3-285Q | Hanwha SolarOne (Qidong) HSL72P6-PB-3-285QB | Hanwha SolarOne (Qidong) HSL72P6-PB-3-285QW | Hanwha SolarOne (Qidong) HSL72P6-PB-4-285Q | Hanwha SolarOne (Qidong) HSL72P6-PB-4-285QB | Hanwha SolarOne (Qidong) HSL72P6-PB-4-285QW | Hanwha SolarOne (Qidong) HSL72P6-PB-4-285T | Hanwha SolarOne (Qidong) HSL72P6-PB-4-285TB | Hanwha SolarOne (Qidong) HSL72P6-PB-4-285TW | Hanwha SolarOne (Qidong) SF260-36-P285 | Hanwha SolarOne (Qidong) SF260-36-P285B | Hanwha SolarOne (Qidong) SF260-36-P285L | Hanwha SolarOne (Qidong) SF260-36-P285L-B | Hanwha SolarOne (Qidong) HSL72M6-HA-0-290T | Hanwha SolarOne (Qidong) HSL72M6-HA-0-290TB | Hanwha SolarOne (Qidong) HSL72M6-HA-0-290TW | Hanwha SolarOne (Qidong) HSL72M6-HA-4-290T | Hanwha SolarOne (Qidong) HSL72M6-HA-4-290TB | Hanwha SolarOne (Qidong) HSL72M6-HA-4-290TW | Hanwha SolarOne (Qidong) HSL72M6-HB-0-290T | Hanwha SolarOne (Qidong) HSL72M6-HB-0-290TB | Hanwha SolarOne (Qidong) HSL72M6-HB-0-290TW | Hanwha SolarOne (Qidong) HSL72M6-HB-4-290T | Hanwha SolarOne (Qidong) HSL72M6-HB-4-290TB | Hanwha SolarOne (Qidong) HSL72M6-HB-4-290TW | Hanwha SolarOne (Qidong) HSL72P6-PA-0-290T | Hanwha SolarOne (Qidong) HSL72P6-PA-0-290TB | Hanwha SolarOne (Qidong) HSL72P6-PA-0-290TW | Hanwha SolarOne (Qidong) HSL72P6-PA-2-290QB | Hanwha SolarOne (Qidong) HSL72P6-PA-3-290Q | Hanwha SolarOne (Qidong) HSL72P6-PA-3-290QW | Hanwha SolarOne (Qidong) HSL72P6-PA-4-290Q | Hanwha SolarOne (Qidong) HSL72P6-PA-4-290QB | Hanwha SolarOne (Qidong) HSL72P6-PA-4-290QW | Hanwha SolarOne (Qidong) HSL72P6-PA-4-290T | Hanwha SolarOne (Qidong) HSL72P6-PA-4-290TB | Hanwha SolarOne (Qidong) HSL72P6-PA-4-290TW | Hanwha SolarOne (Qidong) HSL72P6-PB-0-290T | Hanwha SolarOne (Qidong) HSL72P6-PB-0-290TB | Hanwha SolarOne (Qidong) HSL72P6-PB-0-290TW | Hanwha SolarOne (Qidong) HSL72P6-PB-2-290Q | Hanwha SolarOne (Qidong) HSL72P6-PB-2-290QB | Hanwha SolarOne (Qidong) HSL72P6-PB-2-290QW | Hanwha SolarOne (Qidong) HSL72P6-PB-3-290Q | Hanwha SolarOne (Qidong) HSL72P6-PB-3-290QB | Hanwha SolarOne (Qidong) HSL72P6-PB-3-290QW | Hanwha SolarOne (Qidong) HSL72P6-PB-4-290Q | Hanwha SolarOne (Qidong) HSL72P6-PB-4-290QB | Hanwha SolarOne (Qidong) HSL72P6-PB-4-290QW | Hanwha SolarOne (Qidong) HSL72P6-PB-4-290T | Hanwha SolarOne (Qidong) HSL72P6-PB-4-290TB | Hanwha SolarOne (Qidong) HSL72P6-PB-4-290TW | Hanwha SolarOne (Qidong) HSL72P6-PC-3-290 | Hanwha SolarOne (Qidong) HSL72P6-PC-3-290W | Hanwha SolarOne (Qidong) SF260-36-P290 | Hanwha SolarOne (Qidong) SF260-36-P290B | Hanwha SolarOne (Qidong) SF260-36-P290L | Hanwha SolarOne (Qidong) SF260-36-P290L-B | Hanwha SolarOne (Qidong) HSL72M6-HA-0-295T | Hanwha SolarOne (Qidong) HSL72M6-HA-0-295TB | Hanwha SolarOne (Qidong) HSL72M6-HA-0-295TW | Hanwha SolarOne (Qidong) HSL72M6-HA-4-295T | Hanwha SolarOne (Qidong) HSL72M6-HA-4-295TB | Hanwha SolarOne (Qidong) HSL72M6-HA-4-295TW | Hanwha SolarOne (Qidong) HSL72M6-HB-0-295T | Hanwha SolarOne (Qidong) HSL72M6-HB-0-295TB | Hanwha SolarOne (Qidong) HSL72M6-HB-0-295TW | Hanwha SolarOne (Qidong) HSL72M6-HB-4-295T | Hanwha SolarOne (Qidong) HSL72M6-HB-4-295TB | Hanwha SolarOne (Qidong) HSL72M6-HB-4-295TW | Hanwha SolarOne (Qidong) HSL72P6-PA-0-295T | Hanwha SolarOne (Qidong) HSL72P6-PA-0-295TB | Hanwha SolarOne (Qidong) HSL72P6-PA-0-295TW | Hanwha SolarOne (Qidong) HSL72P6-PA-2-295Q | Hanwha SolarOne (Qidong) HSL72P6-PA-2-295QB | Hanwha SolarOne (Qidong) HSL72P6-PA-2-295QW | Hanwha SolarOne (Qidong) HSL72P6-PA-3-295Q | Hanwha SolarOne (Qidong) HSL72P6-PA-3-295QB | Hanwha SolarOne (Qidong) HSL72P6-PA-3-295QW | Hanwha SolarOne (Qidong) HSL72P6-PA-4-295Q | Hanwha SolarOne (Qidong) HSL72P6-PA-4-295QB | Hanwha SolarOne (Qidong) HSL72P6-PA-4-295QW | Hanwha SolarOne (Qidong) HSL72P6-PA-4-295T | Hanwha SolarOne (Qidong) HSL72P6-PA-4-295TB | Hanwha SolarOne (Qidong) HSL72P6-PA-4-295TW | Hanwha SolarOne (Qidong) HSL72P6-PB-0-295T | Hanwha SolarOne (Qidong) HSL72P6-PB-0-295TB | Hanwha SolarOne (Qidong) HSL72P6-PB-0-295TW | Hanwha SolarOne (Qidong) HSL72P6-PB-2-295Q | Hanwha SolarOne (Qidong) HSL72P6-PB-2-295QB | Hanwha SolarOne (Qidong) HSL72P6-PB-2-295QW | Hanwha SolarOne (Qidong) HSL72P6-PB-3-295Q | Hanwha SolarOne (Qidong) HSL72P6-PB-3-295QB | Hanwha SolarOne (Qidong) HSL72P6-PB-3-295QW | Hanwha SolarOne (Qidong) HSL72P6-PB-4-295 | Hanwha SolarOne (Qidong) HSL72P6-PB-4-295Q | Hanwha SolarOne (Qidong) HSL72P6-PB-4-295QB | Hanwha SolarOne (Qidong) HSL72P6-PB-4-295QW | Hanwha SolarOne (Qidong) HSL72P6-PB-4-295T | Hanwha SolarOne (Qidong) HSL72P6-PB-4-295TB | Hanwha SolarOne (Qidong) HSL72P6-PB-4-295TW | Hanwha SolarOne (Qidong) HSL72P6-PB-4-295W | Hanwha SolarOne (Qidong) HSL72P6-PC-3-295 | Hanwha SolarOne (Qidong) HSL72P6-PC-3-295Q | Hanwha SolarOne (Qidong) HSL72P6-PC-3-295QW | Hanwha SolarOne (Qidong) HSL72P6-PC-3-295W | Hanwha SolarOne (Qidong) SF260-36-P295 | Hanwha SolarOne (Qidong) SF260-36-P295B | Hanwha SolarOne (Qidong) SF260-36-P295L | Hanwha SolarOne (Qidong) SF260-36-P295L-B | Hanwha SolarOne (Qidong) HSL72M6-HA-0-300T | Hanwha SolarOne (Qidong) HSL72M6-HA-0-300TB | Hanwha SolarOne (Qidong) HSL72M6-HA-0-300TW | Hanwha SolarOne (Qidong) HSL72M6-HA-4-300T | Hanwha SolarOne (Qidong) HSL72M6-HA-4-300TB | Hanwha SolarOne (Qidong) HSL72M6-HA-4-300TW | Hanwha SolarOne (Qidong) HSL72M6-HB-0-300T | Hanwha SolarOne (Qidong) HSL72M6-HB-0-300TB | Hanwha SolarOne (Qidong) HSL72M6-HB-0-300TW | Hanwha SolarOne (Qidong) HSL72M6-HB-4-300T | Hanwha SolarOne (Qidong) HSL72M6-HB-4-300TB | Hanwha SolarOne (Qidong) HSL72M6-HB-4-300TW | Hanwha SolarOne (Qidong) HSL72P6-PA-0-300T | Hanwha SolarOne (Qidong) HSL72P6-PA-0-300TW | Hanwha SolarOne (Qidong) HSL72P6-PA-2-300Q | Hanwha SolarOne (Qidong) HSL72P6-PA-2-300QB | Hanwha SolarOne (Qidong) HSL72P6-PA-2-300QW | Hanwha SolarOne (Qidong) HSL72P6-PA-3-300Q | Hanwha SolarOne (Qidong) HSL72P6-PA-3-300QB | Hanwha SolarOne (Qidong) HSL72P6-PA-3-300QW | Hanwha SolarOne (Qidong) HSL72P6-PA-4-300Q | Hanwha SolarOne (Qidong) HSL72P6-PA-4-300QB | Hanwha SolarOne (Qidong) HSL72P6-PA-4-300QW | Hanwha SolarOne (Qidong) HSL72P6-PA-4-300T | Hanwha SolarOne (Qidong) HSL72P6-PA-4-300TW | Hanwha SolarOne (Qidong) HSL72P6-PB-0-300T | Hanwha SolarOne (Qidong) HSL72P6-PB-0-300TW | Hanwha SolarOne (Qidong) HSL72P6-PB-2-300Q | Hanwha SolarOne (Qidong) HSL72P6-PB-2-300QB | Hanwha SolarOne (Qidong) HSL72P6-PB-2-300QW | Hanwha SolarOne (Qidong) HSL72P6-PB-3-300Q | Hanwha SolarOne (Qidong) HSL72P6-PB-3-300QB | Hanwha SolarOne (Qidong) HSL72P6-PB-3-300QW | Hanwha SolarOne (Qidong) HSL72P6-PB-4-300 | Hanwha SolarOne (Qidong) HSL72P6-PB-4-300Q | Hanwha SolarOne (Qidong) HSL72P6-PB-4-300QB | Hanwha SolarOne (Qidong) HSL72P6-PB-4-300QW | Hanwha SolarOne (Qidong) HSL72P6-PB-4-300T | Hanwha SolarOne (Qidong) HSL72P6-PB-4-300TW | Hanwha SolarOne (Qidong) HSL72P6-PB-4-300W | Hanwha SolarOne (Qidong) HSL72P6-PC-3-300 | Hanwha SolarOne (Qidong) HSL72P6-PC-3-300Q | Hanwha SolarOne (Qidong) HSL72P6-PC-3-300QW | Hanwha SolarOne (Qidong) HSL72P6-PC-3-300W | Hanwha SolarOne (Qidong) HSL72M6-HA-0-305T | Hanwha SolarOne (Qidong) HSL72M6-HA-0-305TB | Hanwha SolarOne (Qidong) HSL72M6-HA-0-305TW | Hanwha SolarOne (Qidong) HSL72M6-HA-4-305T | Hanwha SolarOne (Qidong) HSL72M6-HA-4-305TB | Hanwha SolarOne (Qidong) HSL72M6-HA-4-305TW | Hanwha SolarOne (Qidong) HSL72M6-HB-0-305T | Hanwha SolarOne (Qidong) HSL72M6-HB-0-305TB | Hanwha SolarOne (Qidong) HSL72M6-HB-0-305TW | Hanwha SolarOne (Qidong) HSL72M6-HB-4-305T | Hanwha SolarOne (Qidong) HSL72M6-HB-4-305TB | Hanwha SolarOne (Qidong) HSL72M6-HB-4-305TW | Hanwha SolarOne (Qidong) HSL72P6-PA-0-305T | Hanwha SolarOne (Qidong) HSL72P6-PA-0-305TB | Hanwha SolarOne (Qidong) HSL72P6-PA-0-305TW | Hanwha SolarOne (Qidong) HSL72P6-PA-2-305Q | Hanwha SolarOne (Qidong) HSL72P6-PA-2-305QB | Hanwha SolarOne (Qidong) HSL72P6-PA-2-305QW | Hanwha SolarOne (Qidong) HSL72P6-PA-3-305Q | Hanwha SolarOne (Qidong) HSL72P6-PA-3-305QB | Hanwha SolarOne (Qidong) HSL72P6-PA-3-305QW | Hanwha SolarOne (Qidong) HSL72P6-PA-4-305Q | Hanwha SolarOne (Qidong) HSL72P6-PA-4-305QB | Hanwha SolarOne (Qidong) HSL72P6-PA-4-305QW | Hanwha SolarOne (Qidong) HSL72P6-PA-4-305T | Hanwha SolarOne (Qidong) HSL72P6-PA-4-305TB | Hanwha SolarOne (Qidong) HSL72P6-PA-4-305TW | Hanwha SolarOne (Qidong) HSL72P6-PB-0-305T | Hanwha SolarOne (Qidong) HSL72P6-PB-0-305TB | Hanwha SolarOne (Qidong) HSL72P6-PB-0-305TW | Hanwha SolarOne (Qidong) HSL72P6-PB-2-305Q | Hanwha SolarOne (Qidong) HSL72P6-PB-2-305QB | Hanwha SolarOne (Qidong) HSL72P6-PB-2-305QW | Hanwha SolarOne (Qidong) HSL72P6-PB-3-305Q | Hanwha SolarOne (Qidong) HSL72P6-PB-3-305QB | Hanwha SolarOne (Qidong) HSL72P6-PB-3-305QW | Hanwha SolarOne (Qidong) HSL72P6-PB-4-305 | Hanwha SolarOne (Qidong) HSL72P6-PB-4-305Q | Hanwha SolarOne (Qidong) HSL72P6-PB-4-305QB | Hanwha SolarOne (Qidong) HSL72P6-PB-4-305QW | Hanwha SolarOne (Qidong) HSL72P6-PB-4-305T | Hanwha SolarOne (Qidong) HSL72P6-PB-4-305TB | Hanwha SolarOne (Qidong) HSL72P6-PB-4-305TW | Hanwha SolarOne (Qidong) HSL72P6-PB-4-305W | Hanwha SolarOne (Qidong) HSL72P6-PC-3-305 | Hanwha SolarOne (Qidong) HSL72P6-PC-3-305Q | Hanwha SolarOne (Qidong) HSL72P6-PC-3-305QW | Hanwha SolarOne (Qidong) HSL72P6-PC-3-305W | Hanwha SolarOne (Qidong) HSL72M6-HA-0-310T | Hanwha SolarOne (Qidong) HSL72M6-HA-0-310TB | Hanwha SolarOne (Qidong) HSL72M6-HA-0-310TW | Hanwha SolarOne (Qidong) HSL72M6-HA-4-310T | Hanwha SolarOne (Qidong) HSL72M6-HA-4-310TB | Hanwha SolarOne (Qidong) HSL72M6-HA-4-310TW | Hanwha SolarOne (Qidong) HSL72M6-HB-0-310T | Hanwha SolarOne (Qidong) HSL72M6-HB-0-310TB | Hanwha SolarOne (Qidong) HSL72M6-HB-0-310TW | Hanwha SolarOne (Qidong) HSL72M6-HB-4-310T | Hanwha SolarOne (Qidong) HSL72M6-HB-4-310TB | Hanwha SolarOne (Qidong) HSL72M6-HB-4-310TW | Hanwha SolarOne (Qidong) HSL72P6-PB-0-310T | Hanwha SolarOne (Qidong) HSL72P6-PB-0-310TW | Hanwha SolarOne (Qidong) HSL72P6-PB-4-310 | Hanwha SolarOne (Qidong) HSL72P6-PB-4-310T | Hanwha SolarOne (Qidong) HSL72P6-PB-4-310TW | Hanwha SolarOne (Qidong) HSL72P6-PB-4-310W | Hanwha SolarOne (Qidong) HSL72P6-PC-3-310 | Hanwha SolarOne (Qidong) HSL72P6-PC-3-310Q | Hanwha SolarOne (Qidong) HSL72P6-PC-3-310QW | Hanwha SolarOne (Qidong) HSL72P6-PC-3-310W | Hanwha SolarOne (Qidong) HSL72P6-PB-0-315T | Hanwha SolarOne (Qidong) HSL72P6-PB-0-315TW | Hanwha SolarOne (Qidong) HSL72P6-PB-4-315T | Hanwha SolarOne (Qidong) HSL72P6-PB-4-315TW | Hanwha SolarOne (Qidong) HSL72P6-PC-3-315Q | Hanwha SolarOne (Qidong) HSL72P6-PC-3-315QW | Hanwha SolarOne Hong Kong HSL60P-PA-0-235K | Hanwha SolarOne Hong Kong HSL60P-PA-0-240K | Hanwha SolarOne Hong Kong HSL60P-PA-0-245K | Hanwha SolarOne Hong Kong HSL60P-PA-0-250K | Hanwha SolarOne Hong Kong HSL72P-PA-0-280K | Hanwha SolarOne Hong Kong HSL72P-PA-0-285K | Hanwha SolarOne Hong Kong HSL72P-PA-0-290K | Hanwha SolarOne Hong Kong HSL72P-PA-0-295K | HC Solar Power HCP175D-24 | HC Solar Power HCP180D-24 | HC Solar Power HCP185D-24 | HC Solar Power HCP190D-24 | HC Solar Power HCP195D-24 | HC Solar Power HCP230P-20 | HC Solar Power HCP235P-20 | HC Solar Power HCP240P-20 | HC Solar Power HCP245P-24 | HC Solar Power HCP250P-24 | HC Solar Power HCP255P-24 | HC Solar Power HCP260P-24 | HC Solar Power HCP265P-24 | HC Solar Power HCP270P-24 | HC Solar Power HCP275P-24 | HC Solar Power HCP280P-24 | Heliene 60P215 | Heliene 60P220 | Heliene 60P225 | Heliene 60M230 | Heliene 60P230 | Heliene 60M235 | Heliene 60M240 | Heliene 60P240 | Heliene 60P240-HD | Heliene 60M245 | Heliene 60P245 | Heliene 60P245-HD | Heliene 60M250 | Heliene 60P250 | Heliene 60P250-HD | Heliene 60M255 | Heliene 60P255 | Heliene 60P255-HD | Heliene 60M260 | Heliene 60P260 | Heliene 72P260 | Heliene 60M265 | Heliene 72P265 | Heliene 60M270 | Heliene 60M270-HD | Heliene 72P270 | Heliene 60M275 | Heliene 60M275-HD | Heliene 72P275 | Heliene 60M280 | Heliene 60M280-HD | Heliene 72M280 | Heliene 60M285 | Heliene 60M285-HD | Heliene 72M285 | Heliene 72P285 | Heliene 72P285-HD | Heliene 60M290 | Heliene 60M290-HD | Heliene 72M290 | Heliene 72P290 | Heliene 72P290-HD | Heliene 60M295 | Heliene 72M295 | Heliene 60M300 | Heliene 72M300 | Heliene 72P300 | Heliene 72P300-HD | Heliene 72M305 | Heliene 72P305 | Heliene 72P305-HD | Heliene 72M310 | Heliene 72P310 | Heliene 72P310-HD | Heliene 72M315 | Heliene 72M315-HD | Heliene 72P315 | Heliene 72P315-HD | Heliene 72M320 | Heliene 72M320-HD | Heliene 72P320 | Heliene 72P320-HD | Heliene 72M325 | Heliene 72M325-HD | Heliene 72P-325 | Heliene 72M330 | Heliene 72M330-HD | Heliene 72M335 | Heliene 72M335-HD | Heliene 72M340 | Heliene 72M340-HD | Heliene 72M345 | Heliene 72M345-HD | Heliene 72M350 | Heliene 72M355 | Heliene 72M360 | Heliene 72M365 | Heliene 72M370 | Heliene 96M390 | Heliene 96M395 | Heliene 96M400 | Heliene 96M405 | Heliene 96M410 | Heliene 96M415 | Heliene 96P415 | Heliene 96M420 | Heliene 96P420 | Heliene 96P425 | Heliene 96P430 | Heliene 96P435 | Heliene 96M440 | Heliene 96P440 | Heliene 96M445 | Heliene 96M450 | Heliene 96M455 | Heliene 96M460 | Heliene 96M465 | Heliene 96M470 | Heliene 96M475 | Helios Energy Europe HEE210UA62 | Helios Energy Europe HEE210UA63 | Helios Energy Europe HEE210U | Helios Energy Europe HEE210UA64 | Helios Energy Europe HEE210UA65 | Helios Energy Europe HEE215MA64 | Helios Energy Europe HEE215MA65 | Helios Energy Europe 60P240 | Helios Energy Europe HEE215M | Helios Energy Europe HEE215MA66 | Helios Energy Europe 60P245 | Helios Energy Europe HEE215MA67 | Helios Energy Europe 60M250 | Helios Energy Europe 60P250 | Helios Energy Europe HEE215MA68 | Helios Energy Europe 60M255 | Helios Energy Europe 60P255 | Helios Energy Europe 60M260 | Helios Energy Europe 60P260 | Helios Energy Europe HEE275AU72 | Helios Energy Europe 60M265 | Helios Energy Europe HEE275AU73 | Helios Energy Europe 60M270 | Helios Energy Europe HEE275AU74 | Helios Energy Europe HEE275U | Helios Energy Europe 60M275 | Helios Energy Europe HEE275AU75 | Helios Energy Europe 60M280 | Helios Energy Europe HEE300MA74 | Helios Energy Europe 60M285 | Helios Energy Europe 72P285 | Helios Energy Europe HEE300MA75 | Helios Energy Europe 60M290 | Helios Energy Europe 72P290 | Helios Energy Europe HEE300M | Helios Energy Europe HEE300MA76 | Helios Energy Europe HEE300MA77 | Helios Energy Europe 72P300 | Helios Energy Europe HEE300MA78 | Helios Energy Europe 72M305 | Helios Energy Europe 72P305 | Helios Energy Europe 72M310 | Helios Energy Europe 72P310 | Helios Energy Europe 72M315 | Helios Energy Europe 72P315 | Helios Energy Europe 72M320 | Helios Energy Europe 72P320 | Helios Energy Europe 72M325 | Helios Energy Europe 72M330 | Helios Energy Europe 72M335 | Helios Energy Europe 72M340 | Helios Energy Europe 72M345 | Helios Energy Europe 96M390 | Helios Energy Europe 96M395 | Helios Energy Europe 96M400 | Helios Energy Europe 96M405 | Helios Energy Europe 96M410 | Helios Energy Europe 96M415 | Helios Energy Europe 96M420 | Helios USA 6T p215 | Helios USA 6T p220 | Helios USA 6T p225 | Helios USA 6T 230 | Helios USA 6T p230 | Helios USA 6T 235 | Helios USA 6T 240 | Helios USA 6T 245 | Helios USA 6T 250 | Helios USA 6T 255 | Helios USA 6TA | Helios USA 6T 260 | Helios USA 6T 265 | Helios USA 7T2 280 | Helios USA 7T2 285 | Helios USA 7T2 290 | Helios USA 7T2 295 | Helios USA 7T2 300 | Helios USA 7T2 305 | Helios USA 7T2 310 | Helios USA 7T2 315 | Helios USA 9T6 390 | Helios USA 9T6 395 | Helios USA 9T6 400 | Helios USA 9T6 405 | Helios USA 9T6 410 | Helios USA 9T6 415 | Helios USA 9T6 420 | HelioVolt HVC-170X | HelioVolt HVC-190X | Hengdian Group DMEGC Magnetics DM175-M125-72 | Hengdian Group DMEGC Magnetics DM180-M125-72 | Hengdian Group DMEGC Magnetics DM185-M125-72 | Hengdian Group DMEGC Magnetics DM190-M125-72 | Hengdian Group DMEGC Magnetics DM195-M125-72 | Hengdian Group DMEGC Magnetics DM210-P156-60 | Hengdian Group DMEGC Magnetics DM215-P156-60 | Hengdian Group DMEGC Magnetics DM220-P156-60 | Hengdian Group DMEGC Magnetics DM225-P156-60 | Hengdian Group DMEGC Magnetics DM230-M156-60 | Hengdian Group DMEGC Magnetics DM230-P156-60 | Hengdian Group DMEGC Magnetics DM230-P156-60BF | Hengdian Group DMEGC Magnetics DM235-M156-60 | Hengdian Group DMEGC Magnetics DM235-P156-60 | Hengdian Group DMEGC Magnetics DM235-P156-60BF | Hengdian Group DMEGC Magnetics DM240-M156-60 | Hengdian Group DMEGC Magnetics DM240-P156-60 | Hengdian Group DMEGC Magnetics DM240-P156-60BF | Hengdian Group DMEGC Magnetics DM245-M156-60 | Hengdian Group DMEGC Magnetics DM245-P156-60 | Hengdian Group DMEGC Magnetics DM245-P156-60BF | Hengdian Group DMEGC Magnetics DM250-M156-60 | Hengdian Group DMEGC Magnetics DM250-P156-60 | Hengdian Group DMEGC Magnetics DM250-P156-60BF | Hengdian Group DMEGC Magnetics DM250-P156-72 | Hengdian Group DMEGC Magnetics DM255-P156-60 | Hengdian Group DMEGC Magnetics DM255-P156-60BF | Hengdian Group DMEGC Magnetics DM255-P156-72 | Hengdian Group DMEGC Magnetics DM260-P156-60 | Hengdian Group DMEGC Magnetics DM260-P156-60BF | Hengdian Group DMEGC Magnetics DM260-P156-72 | Hengdian Group DMEGC Magnetics DM265-M156-72 | Hengdian Group DMEGC Magnetics DM265-P156-72 | Hengdian Group DMEGC Magnetics DM270-M156-72 | Hengdian Group DMEGC Magnetics DM270-P156-72 | Hengdian Group DMEGC Magnetics DM275-M156-72 | Hengdian Group DMEGC Magnetics DM275-P156-72 | Hengdian Group DMEGC Magnetics DM280-M156-72 | Hengdian Group DMEGC Magnetics DM280-P156-72 | Hengdian Group DMEGC Magnetics DM285-M156-72 | Hengdian Group DMEGC Magnetics DM285-P156-72 | Hengdian Group DMEGC Magnetics DM290-M156-72 | Hengdian Group DMEGC Magnetics DM290-P156-72 | Hengdian Group DMEGC Magnetics DM295-M156-72 | Hengdian Group DMEGC Magnetics DM295-P156-72 | Hengdian Group DMEGC Magnetics DM300-P156-72 | Hengdian Group DMEGC Magnetics DM305-P156-72 | Hengji PV-Tech Energy HJM085M-12 | Hengji PV-Tech Energy HJM090M-12 | Hengji PV-Tech Energy HJM095M-12 | Hengji PV-Tech Energy HJM170M-24 | Hengji PV-Tech Energy HJM175M-24 | Hengji PV-Tech Energy HJM180M-24 | Hengji PV-Tech Energy HJM180P-16 | Hengji PV-Tech Energy HJM185M-24 | Hengji PV-Tech Energy HJM190M-24 | Hengji PV-Tech Energy HJM190M-28 | Hengji PV-Tech Energy HJM190P-16 | Hengji PV-Tech Energy HJM200M-28 | Hengji PV-Tech Energy HJM200P-16 | Hengji PV-Tech Energy HJM200P-18 | Hengji PV-Tech Energy HJM210M-28 | Hengji PV-Tech Energy HJM210P-18 | Hengji PV-Tech Energy HJM220M-28 | Hengji PV-Tech Energy HJM220P-18 | Hengji PV-Tech Energy HJM230M-28 | Hengji PV-Tech Energy HJM230P-20 | Hengji PV-Tech Energy HJM240P-20 | Hengji PV-Tech Energy HJM250P-20 | Hengji PV-Tech Energy HJM270P-24 | Hengji PV-Tech Energy HJM280P-24 | Hengji PV-Tech Energy HJM290P-24 | HHV Solar Technologies HSTUBC12095P | HHV Solar Technologies HSTUBC12100P | HHV Solar Technologies HSTUBC12105P | HHV Solar Technologies HSTUBF12130P | HHV Solar Technologies HSTUAF12135M | HHV Solar Technologies HSTUBF12135P | HHV Solar Technologies HSTUAF12140M | HHV Solar Technologies HSTUBF12140P | HHV Solar Technologies HSTUAF12145M | HHV Solar Technologies HSTUBF12175P | HHV Solar Technologies HSTUAF12180M | HHV Solar Technologies HSTUBF12180P | HHV Solar Technologies HSTUAF12185M | HHV Solar Technologies HSTUBF12185P | HHV Solar Technologies HSTUAF12190M | HHV Solar Technologies HSTUBF12190P | HHV Solar Technologies HSTUAF12195M | HHV Solar Technologies HSTUBF12195P | HHV Solar Technologies HSTUBF12200P | HHV Solar Technologies HSTUAF12205M | HHV Solar Technologies HSTUBF12205P | HHV Solar Technologies HSTUAF12210M | HHV Solar Technologies HSTUBF12210P | HHV Solar Technologies HSTUAF12215M | HHV Solar Technologies HSTUBF24215P | HHV Solar Technologies HSTUCF24215P | HHV Solar Technologies HSTUAF12220M | HHV Solar Technologies HSTUBF24220P | HHV Solar Technologies HSTUCF24220P | HHV Solar Technologies HSTUAF24225M | HHV Solar Technologies HSTUBF24225P | HHV Solar Technologies HSTUCF24225P | HHV Solar Technologies HSTUAF24230M | HHV Solar Technologies HSTUBF24230P | HHV Solar Technologies HSTUCF24230P | HHV Solar Technologies HSTUAF24235M | HHV Solar Technologies HSTUBF24235P | HHV Solar Technologies HSTUCF24235P | HHV Solar Technologies HSTUAF24240M | HHV Solar Technologies HSTUAF24245M | HHV Solar Technologies HSTUAF24260M | HHV Solar Technologies HSTUBF24260P | HHV Solar Technologies HSTUCF24260P | HHV Solar Technologies HSTUAF24265M | HHV Solar Technologies HSTUBF24265P | HHV Solar Technologies HSTUCF24265P | HHV Solar Technologies HSTUAF24270M | HHV Solar Technologies HSTUBF24270P | HHV Solar Technologies HSTUCF24270P | HHV Solar Technologies HSTUAF24275M | HHV Solar Technologies HSTUBF24275P | HHV Solar Technologies HSTUCF24275P | HHV Solar Technologies HSTUAF24280M | HHV Solar Technologies HSTUBF24280P | HHV Solar Technologies HSTUCF24280P | HHV Solar Technologies HSTUAF24285M | HHV Solar Technologies HSTUAF24290M | HHV Solar Technologies HSTUAF24295M | Himin Clean Energy Holdings HG-160S | Himin Clean Energy Holdings HG-165S | Himin Clean Energy Holdings HG-170S | Himin Clean Energy Holdings HG-175S | Himin Clean Energy Holdings HG-180S | Himin Clean Energy Holdings HG-185S | Honda Soltec HEM120PUB | Honda Soltec HEM125PUB | Honda Soltec HEM130PUB | Hunan Sunzone Optoelectronics Energy SZ180M-36 | Hunan Sunzone Optoelectronics Energy SZ185M-36 | Hunan Sunzone Optoelectronics Energy SZ190M-36 | Hunan Sunzone Optoelectronics Energy SZ220P-29 | Hunan Sunzone Optoelectronics Energy SZ225P-29 | Hunan Sunzone Optoelectronics Energy SZ230P-29 | Hunan Sunzone Optoelectronics Energy SZ235P-29 | Hunan Sunzone Optoelectronics Energy SZ240P-29 | Hunan Sunzone Optoelectronics Energy SZ275P-35 | Hunan Sunzone Optoelectronics Energy SZ280P-35 | Hunan Sunzone Optoelectronics Energy SZ285P-35 | Hunan Sunzone Optoelectronics Energy SZ290P-35 | Hyundai Heavy Industries Green Energy Co. HiS-M191SF | Hyundai Heavy Industries Green Energy Co. HiS-M194SF | Hyundai Heavy Industries Green Energy Co. HiS-M197SF | Hyundai Heavy Industries Green Energy Co. HiS-M200SF | Hyundai Heavy Industries Green Energy Co. HiS-M203SF | Hyundai Heavy Industries Green Energy Co. HiS-M206SF | Hyundai Heavy Industries Green Energy Co. HiS-S206SF | Hyundai Heavy Industries Green Energy Co. HiS-M209SF | Hyundai Heavy Industries Green Energy Co. HiS-S209SF | Hyundai Heavy Industries Green Energy Co. HiS-M212SF | Hyundai Heavy Industries Green Energy Co. HiS-M212SG | Hyundai Heavy Industries Green Energy Co. HiS-S212SF | Hyundai Heavy Industries Green Energy Co. HiS-M215SF | Hyundai Heavy Industries Green Energy Co. HiS-M215SG | Hyundai Heavy Industries Green Energy Co. HiS-S215SF | Hyundai Heavy Industries Green Energy Co. HiS-M218SG | Hyundai Heavy Industries Green Energy Co. HiS-S218SF | Hyundai Heavy Industries Green Energy Co. HiS-M221SG | Hyundai Heavy Industries Green Energy Co. HiS-S221SF | Hyundai Heavy Industries Green Energy Co. HiS-M223MG | Hyundai Heavy Industries Green Energy Co. HiS-M223MG(BK) | Hyundai Heavy Industries Green Energy Co. HiS-M224SG | Hyundai Heavy Industries Green Energy Co. HiS-S224SF | Hyundai Heavy Industries Green Energy Co. HiS-S224SG | Hyundai Heavy Industries Green Energy Co. HiS-M225MG | Hyundai Heavy Industries Green Energy Co. HiS-M225MG(BK) | Hyundai Heavy Industries Green Energy Co. HiS-M227SG | Hyundai Heavy Industries Green Energy Co. HiS-S227SG | Hyundai Heavy Industries Green Energy Co. HiS-M228MG | Hyundai Heavy Industries Green Energy Co. HiS-M228MG(BK) | Hyundai Heavy Industries Green Energy Co. HiS-M230MG | Hyundai Heavy Industries Green Energy Co. HiS-M230MG(BK) | Hyundai Heavy Industries Green Energy Co. HiS-M230SG | Hyundai Heavy Industries Green Energy Co. HiS-S230SG | Hyundai Heavy Industries Green Energy Co. HiS-M233MG | Hyundai Heavy Industries Green Energy Co. HiS-M233MG(BK) | Hyundai Heavy Industries Green Energy Co. HiS-M233SG | Hyundai Heavy Industries Green Energy Co. HiS-S233MG | Hyundai Heavy Industries Green Energy Co. HiS-S233MG(BK) | Hyundai Heavy Industries Green Energy Co. HiS-S233SG | Hyundai Heavy Industries Green Energy Co. HiS-M235MG | Hyundai Heavy Industries Green Energy Co. HiS-M235MG(BK) | Hyundai Heavy Industries Green Energy Co. HiS-M235RG(BK) | Hyundai Heavy Industries Green Energy Co. HiS-S235MG | Hyundai Heavy Industries Green Energy Co. HiS-S235MG(BK) | Hyundai Heavy Industries Green Energy Co. HiS-M236SG | Hyundai Heavy Industries Green Energy Co. HiS-S236SG | Hyundai Heavy Industries Green Energy Co. HiS-M238MG | Hyundai Heavy Industries Green Energy Co. HiS-M238MG(BK) | Hyundai Heavy Industries Green Energy Co. HiS-S238MG | Hyundai Heavy Industries Green Energy Co. HiS-S238MG(BK) | Hyundai Heavy Industries Green Energy Co. HiS-M239SG | Hyundai Heavy Industries Green Energy Co. HiS-S239SG | Hyundai Heavy Industries Green Energy Co. HiS-M240MG | Hyundai Heavy Industries Green Energy Co. HiS-M240MG(BK) | Hyundai Heavy Industries Green Energy Co. HiS-M240RG | Hyundai Heavy Industries Green Energy Co. HiS-M240RG(BK) | Hyundai Heavy Industries Green Energy Co. HiS-M240RW | Hyundai Heavy Industries Green Energy Co. HiS-M240TG | Hyundai Heavy Industries Green Energy Co. HiS-S240MG | Hyundai Heavy Industries Green Energy Co. HiS-S240MG(BK) | Hyundai Heavy Industries Green Energy Co. HiS-M242SG | Hyundai Heavy Industries Green Energy Co. HiS-S242SG | Hyundai Heavy Industries Green Energy Co. HiS-M243MG | Hyundai Heavy Industries Green Energy Co. HiS-M243MG(BK) | Hyundai Heavy Industries Green Energy Co. HiS-S243MG | Hyundai Heavy Industries Green Energy Co. HiS-S243MG(BK) | Hyundai Heavy Industries Green Energy Co. HiS-M245HG | Hyundai Heavy Industries Green Energy Co. HiS-M245MG | Hyundai Heavy Industries Green Energy Co. HiS-M245MG(BK) | Hyundai Heavy Industries Green Energy Co. HiS-M245RG | Hyundai Heavy Industries Green Energy Co. HiS-M245RG(BK) | Hyundai Heavy Industries Green Energy Co. HiS-M245RW | Hyundai Heavy Industries Green Energy Co. HiS-M245TG | Hyundai Heavy Industries Green Energy Co. HiS-S245MG | Hyundai Heavy Industries Green Energy Co. HiS-S245MG(BK) | Hyundai Heavy Industries Green Energy Co. HiS-S245RG(BK) | Hyundai Heavy Industries Green Energy Co. HiS-M248MG | Hyundai Heavy Industries Green Energy Co. HiS-M248MG(BK) | Hyundai Heavy Industries Green Energy Co. HiS-S248MG | Hyundai Heavy Industries Green Energy Co. HiS-S248MG(BK) | Hyundai Heavy Industries Green Energy Co. HiS-M250HG | Hyundai Heavy Industries Green Energy Co. HiS-M250MG | Hyundai Heavy Industries Green Energy Co. HiS-M250MG(BK) | Hyundai Heavy Industries Green Energy Co. HiS-M250RG | Hyundai Heavy Industries Green Energy Co. HiS-M250RG(BK) | Hyundai Heavy Industries Green Energy Co. HiS-M250RW | Hyundai Heavy Industries Green Energy Co. HiS-M250TG | Hyundai Heavy Industries Green Energy Co. HiS-S250MG | Hyundai Heavy Industries Green Energy Co. HiS-S250MG(BK) | Hyundai Heavy Industries Green Energy Co. HiS-S250RG(BK) | Hyundai Heavy Industries Green Energy Co. HiS-S250RW | Hyundai Heavy Industries Green Energy Co. HiS-M253MG(BK) | Hyundai Heavy Industries Green Energy Co. HiS-S253MG | Hyundai Heavy Industries Green Energy Co. HiS-S253MG(BK) | Hyundai Heavy Industries Green Energy Co. HiS-M255HG | Hyundai Heavy Industries Green Energy Co. HiS-M255MG(BK) | Hyundai Heavy Industries Green Energy Co. HiS-M255RG | Hyundai Heavy Industries Green Energy Co. HiS-M255RG(BK) | Hyundai Heavy Industries Green Energy Co. HiS-M255RW | Hyundai Heavy Industries Green Energy Co. HiS-M255TG | Hyundai Heavy Industries Green Energy Co. HiS-S255HG | Hyundai Heavy Industries Green Energy Co. HiS-S255MG | Hyundai Heavy Industries Green Energy Co. HiS-S255MG(BK) | Hyundai Heavy Industries Green Energy Co. HiS-S255RG | Hyundai Heavy Industries Green Energy Co. HiS-S255RG(BK) | Hyundai Heavy Industries Green Energy Co. HiS-S255RW | Hyundai Heavy Industries Green Energy Co. HiS-S255TG | Hyundai Heavy Industries Green Energy Co. HiS-S258MG | Hyundai Heavy Industries Green Energy Co. HiS-S258MG(BK) | Hyundai Heavy Industries Green Energy Co. HiS-M260HG | Hyundai Heavy Industries Green Energy Co. HiS-M260KG | Hyundai Heavy Industries Green Energy Co. HiS-M260RG | Hyundai Heavy Industries Green Energy Co. HiS-M260RG(BK) | Hyundai Heavy Industries Green Energy Co. HiS-M260TG | Hyundai Heavy Industries Green Energy Co. HiS-S260HG | Hyundai Heavy Industries Green Energy Co. HiS-S260MG | Hyundai Heavy Industries Green Energy Co. HiS-S260MG(BK) | Hyundai Heavy Industries Green Energy Co. HiS-S260RG | Hyundai Heavy Industries Green Energy Co. HiS-S260RG(BK) | Hyundai Heavy Industries Green Energy Co. HiS-S260RW | Hyundai Heavy Industries Green Energy Co. HiS-S260TG | Hyundai Heavy Industries Green Energy Co. HiS-S263MG | Hyundai Heavy Industries Green Energy Co. HiS-S263MG(BK) | Hyundai Heavy Industries Green Energy Co. HiS-M265KG | Hyundai Heavy Industries Green Energy Co. HiS-M265RG | Hyundai Heavy Industries Green Energy Co. HiS-M265RG(BK) | Hyundai Heavy Industries Green Energy Co. HiS-M265TG | Hyundai Heavy Industries Green Energy Co. HiS-S265HG | Hyundai Heavy Industries Green Energy Co. HiS-S265MG | Hyundai Heavy Industries Green Energy Co. HiS-S265MG(BK) | Hyundai Heavy Industries Green Energy Co. HiS-S265RG | Hyundai Heavy Industries Green Energy Co. HiS-S265RG(BK) | Hyundai Heavy Industries Green Energy Co. HiS-S265RW | Hyundai Heavy Industries Green Energy Co. HiS-S265TG | Hyundai Heavy Industries Green Energy Co. HiS-S268MG | Hyundai Heavy Industries Green Energy Co. HiS-S268MG(BK) | Hyundai Heavy Industries Green Energy Co. HiS-M270KG | Hyundai Heavy Industries Green Energy Co. HiS-M270RG | Hyundai Heavy Industries Green Energy Co. HiS-M270RG(BK) | Hyundai Heavy Industries Green Energy Co. HiS-M270TG | Hyundai Heavy Industries Green Energy Co. HiS-S270HG | Hyundai Heavy Industries Green Energy Co. HiS-S270MG | Hyundai Heavy Industries Green Energy Co. HiS-S270MG(BK) | Hyundai Heavy Industries Green Energy Co. HiS-S270RG | Hyundai Heavy Industries Green Energy Co. HiS-S270RG(BK) | Hyundai Heavy Industries Green Energy Co. HiS-S270TG | Hyundai Heavy Industries Green Energy Co. HiS-M273MI | Hyundai Heavy Industries Green Energy Co. HiS-S273MG | Hyundai Heavy Industries Green Energy Co. HiS-M275HI | Hyundai Heavy Industries Green Energy Co. HiS-M275KG | Hyundai Heavy Industries Green Energy Co. HiS-M275MI | Hyundai Heavy Industries Green Energy Co. HiS-M275RG | Hyundai Heavy Industries Green Energy Co. HiS-M275RG(BK) | Hyundai Heavy Industries Green Energy Co. HiS-M275TG | Hyundai Heavy Industries Green Energy Co. HiS-S275HG | Hyundai Heavy Industries Green Energy Co. HiS-S275MG | Hyundai Heavy Industries Green Energy Co. HiS-S275RG | Hyundai Heavy Industries Green Energy Co. HiS-S275RG(BK) | Hyundai Heavy Industries Green Energy Co. HiS-S275TG | Hyundai Heavy Industries Green Energy Co. HiS-M278MI | Hyundai Heavy Industries Green Energy Co. HiS-M280HI | Hyundai Heavy Industries Green Energy Co. HiS-M280MI | Hyundai Heavy Industries Green Energy Co. HiS-S280KG | Hyundai Heavy Industries Green Energy Co. HiS-S280MI | Hyundai Heavy Industries Green Energy Co. HiS-S280RG | Hyundai Heavy Industries Green Energy Co. HiS-S280RG(BK) | Hyundai Heavy Industries Green Energy Co. HiS-S280TG | Hyundai Heavy Industries Green Energy Co. HiS-M283MI | Hyundai Heavy Industries Green Energy Co. HiS-S283MI | Hyundai Heavy Industries Green Energy Co. HiS-M285HI | Hyundai Heavy Industries Green Energy Co. HiS-M285MI | Hyundai Heavy Industries Green Energy Co. HiS-S285KG | Hyundai Heavy Industries Green Energy Co. HiS-S285MI | Hyundai Heavy Industries Green Energy Co. HiS-S285RG | Hyundai Heavy Industries Green Energy Co. HiS-S285RG(BK) | Hyundai Heavy Industries Green Energy Co. HiS-S285TG | Hyundai Heavy Industries Green Energy Co. HiS-M288MI | Hyundai Heavy Industries Green Energy Co. HiS-S288MI | Hyundai Heavy Industries Green Energy Co. HiS-M290HI | Hyundai Heavy Industries Green Energy Co. HiS-M290MI | Hyundai Heavy Industries Green Energy Co. HiS-M290RI | Hyundai Heavy Industries Green Energy Co. HiS-M290TI | Hyundai Heavy Industries Green Energy Co. HiS-S290KG | Hyundai Heavy Industries Green Energy Co. HiS-S290MI | Hyundai Heavy Industries Green Energy Co. HiS-S290RG | Hyundai Heavy Industries Green Energy Co. HiS-S290RG(BK) | Hyundai Heavy Industries Green Energy Co. HiS-S290TG | Hyundai Heavy Industries Green Energy Co. HiS-M293MI | Hyundai Heavy Industries Green Energy Co. HiS-S293MI | Hyundai Heavy Industries Green Energy Co. HiS-M295HI | Hyundai Heavy Industries Green Energy Co. HiS-M295KI | Hyundai Heavy Industries Green Energy Co. HiS-M295MI | Hyundai Heavy Industries Green Energy Co. HiS-M295RI | Hyundai Heavy Industries Green Energy Co. HiS-M295TI | Hyundai Heavy Industries Green Energy Co. HiS-S295HI | Hyundai Heavy Industries Green Energy Co. HiS-S295KG | Hyundai Heavy Industries Green Energy Co. HiS-S295MI | Hyundai Heavy Industries Green Energy Co. HiS-S295RG | Hyundai Heavy Industries Green Energy Co. HiS-S295RG(BK) | Hyundai Heavy Industries Green Energy Co. HiS-S295TG | Hyundai Heavy Industries Green Energy Co. HiS-M298MI | Hyundai Heavy Industries Green Energy Co. HiS-S298MI | Hyundai Heavy Industries Green Energy Co. HiS-M300HI | Hyundai Heavy Industries Green Energy Co. HiS-M300KI | Hyundai Heavy Industries Green Energy Co. HiS-M300MI | Hyundai Heavy Industries Green Energy Co. HiS-M300RI | Hyundai Heavy Industries Green Energy Co. HiS-M300TI | Hyundai Heavy Industries Green Energy Co. HiS-S300HI | Hyundai Heavy Industries Green Energy Co. HiS-S300KG | Hyundai Heavy Industries Green Energy Co. HiS-S300MI | Hyundai Heavy Industries Green Energy Co. HiS-S300RG | Hyundai Heavy Industries Green Energy Co. HiS-S300RG(BK) | Hyundai Heavy Industries Green Energy Co. HiS-S300TG | Hyundai Heavy Industries Green Energy Co. HiS-S303MI | Hyundai Heavy Industries Green Energy Co. HiS-M305KI | Hyundai Heavy Industries Green Energy Co. HiS-M305RI | Hyundai Heavy Industries Green Energy Co. HiS-M305TI | Hyundai Heavy Industries Green Energy Co. HiS-S305HI | Hyundai Heavy Industries Green Energy Co. HiS-S305MI | Hyundai Heavy Industries Green Energy Co. HiS-S305RI | Hyundai Heavy Industries Green Energy Co. HiS-S305TI | Hyundai Heavy Industries Green Energy Co. HiS-M310KI | Hyundai Heavy Industries Green Energy Co. HiS-M310RI | Hyundai Heavy Industries Green Energy Co. HiS-M310TI | Hyundai Heavy Industries Green Energy Co. HiS-S310HI | Hyundai Heavy Industries Green Energy Co. HiS-S310MI | Hyundai Heavy Industries Green Energy Co. HiS-S310RI | Hyundai Heavy Industries Green Energy Co. HiS-S310TI | Hyundai Heavy Industries Green Energy Co. HiS-M315KI | Hyundai Heavy Industries Green Energy Co. HiS-M315RI | Hyundai Heavy Industries Green Energy Co. HiS-M315TI | Hyundai Heavy Industries Green Energy Co. HiS-S315HI | Hyundai Heavy Industries Green Energy Co. HiS-S315MI | Hyundai Heavy Industries Green Energy Co. HiS-S315RI | Hyundai Heavy Industries Green Energy Co. HiS-S315TI | Hyundai Heavy Industries Green Energy Co. HiS-M320KI | Hyundai Heavy Industries Green Energy Co. HiS-M320RI | Hyundai Heavy Industries Green Energy Co. HiS-M320TI | Hyundai Heavy Industries Green Energy Co. HiS-S320RI | Hyundai Heavy Industries Green Energy Co. HiS-S320TI | Hyundai Heavy Industries Green Energy Co. HiS-M325KI | Hyundai Heavy Industries Green Energy Co. HiS-M325RI | Hyundai Heavy Industries Green Energy Co. HiS-M325TI | Hyundai Heavy Industries Green Energy Co. HiS-S325RI | Hyundai Heavy Industries Green Energy Co. HiS-S325TI | Hyundai Heavy Industries Green Energy Co. HiS-M330KI | Hyundai Heavy Industries Green Energy Co. HiS-M330RI | Hyundai Heavy Industries Green Energy Co. HiS-M330TI | Hyundai Heavy Industries Green Energy Co. HiS-S330KI | Hyundai Heavy Industries Green Energy Co. HiS-S330RI | Hyundai Heavy Industries Green Energy Co. HiS-S330TI | Hyundai Heavy Industries Green Energy Co. HIS-S335KI | Hyundai Heavy Industries Green Energy Co. HiS-S335RI | Hyundai Heavy Industries Green Energy Co. HiS-S335TI | Hyundai Heavy Industries Green Energy Co. HIS-S340KI | Hyundai Heavy Industries Green Energy Co. HiS-S340RI | Hyundai Heavy Industries Green Energy Co. HiS-S340TI | Hyundai Heavy Industries Green Energy Co. HIS-S345KI | Hyundai Heavy Industries Green Energy Co. HiS-S345RI | Hyundai Heavy Industries Green Energy Co. HiS-S345TI | Hyundai Heavy Industries Green Energy Co. HIS-S350KI | Hyundai Heavy Industries Green Energy Co. HiS-S350RI | Hyundai Heavy Industries Green Energy Co. HiS-S350TI | Hyundai Heavy Industries Green Energy Co. HIS-S355KI | Hyundai Heavy Industries Green Energy Co. HiS-S355RI | Hyundai Heavy Industries Green Energy Co. HiS-S355TI | Hyundai Heavy Industries Green Energy Co. HIS-S360KI | Hyundai Heavy Industries Green Energy Co. HiS-S360RI | Innotech Solar ITS210XXXX | Innotech Solar ITS220Eyz2 | Innotech Solar 